simulink model "Comprobacion_Final"  (R2024a)
settings: Solver=ode45  StartTime=0.0  StopTime=10  MaxStep=0.001  RelTol=1e-3
(part 2 of 2)

== matlab function Comprobacion_Final/Cinematica ==
  data: x output; y output; Zin output; x input; dx input; ddx input; theta output; dlth output; ddlth2 output; phi output; dlph output; ddlph2 output; dT output; y input; dy input; ddy input; dz input; ddz input; Zin input; dZin input; ddZin input; ddT output; dpsi output; ddpsi output
function [x, y, Zin, theta, dlth, ddlth2, phi, dlph, ddlph2, dT, ddT, dpsi, ddpsi] = fcn(x, dx, ddx, y, dy, ddy, dz, ddz, Zin, dZin, ddZin)
%% Constantes
p = 79.375;
b = 50.8;
l2 = 93.196;
l1 = 44.45;

%% ============ Geometria de la plataforma (Ax,Ay,Zin -> Oi) ============
Ax = x;
Ay = y;
f1 = (-sin(Ax)*sin(Ay))/(cos(Ax)+cos(Ay));
Az = atan(f1);

alfa1 = deg2rad(0);
alfa2 = deg2rad(120);
alfa3 = deg2rad(240);

Oz = Zin;

R = [ cos(Ay)*cos(Az)                            -cos(Ay)*sin(Az)                          sin(Ay)
      cos(Ax)*sin(Az)+cos(Az)*sin(Ax)*sin(Ay)    cos(Ax)*cos(Az)-sin(Ax)*sin(Ay)*sin(Az)  -cos(Ay)*sin(Ax)
      sin(Ax)*sin(Az)-cos(Ax)*cos(Az)*sin(Ay)    cos(Az)*sin(Ax)+cos(Ax)*sin(Ay)*sin(Az)   cos(Ax)*cos(Ay)];

Rz1 = [cos(alfa1) -sin(alfa1) 0; sin(alfa1) cos(alfa1) 0; 0 0 1];
Rz2 = [cos(alfa2) -sin(alfa2) 0; sin(alfa2) cos(alfa2) 0; 0 0 1];
Rz3 = [cos(alfa3) -sin(alfa3) 0; sin(alfa3) cos(alfa3) 0; 0 0 1];

P = [p; 0; 0];
ux = R(1,1); uy = R(1,2); vy = R(2,2);
Ox = (p*(ux-vy))/2;
Oy = -uy*p;
T  = [Ox; Oy; Oz];
psi = [Ax;Ay;Az];

O1 = T + (R*Rz1*P);
O2 = T + (R*Rz2*P);
O3 = T + (R*Rz3*P);
%% derivadas de o
% Derivada temporal de R (verificada simbólicamente con sympy)
dAx=dx; dAy=dy; dAz=dz;
dpsi=[dAx;dAy;dAz];
ddAx=ddx; ddAy=ddy; ddAz=ddz;
ddpsi=[ddAx;ddAy;ddAz];

dR = [ -dAy*sin(Ay)*cos(Az) - dAz*sin(Az)*cos(Ay), dAy*sin(Ay)*sin(Az) - dAz*cos(Ay)*cos(Az), dAy*cos(Ay);
       -dAx*sin(Ax)*sin(Az) + dAx*sin(Ay)*cos(Ax)*cos(Az) + dAy*sin(Ax)*cos(Ay)*cos(Az) - dAz*sin(Ax)*sin(Ay)*sin(Az) + dAz*cos(Ax)*cos(Az),-dAx*sin(Ax)*cos(Az) - dAx*sin(Ay)*sin(Az)*cos(Ax) - dAy*sin(Ax)*sin(Az)*cos(Ay) - dAz*sin(Ax)*sin(Ay)*cos(Az) - dAz*sin(Az)*cos(Ax), -dAx*cos(Ax)*cos(Ay) + dAy*sin(Ax)*sin(Ay);
        dAx*sin(Ax)*sin(Ay)*cos(Az) + dAx*sin(Az)*cos(Ax) - dAy*cos(Ax)*cos(Ay)*cos(Az) + dAz*sin(Ax)*cos(Az) + dAz*sin(Ay)*sin(Az)*cos(Ax), -dAx*sin(Ax)*sin(Ay)*sin(Az) + dAx*cos(Ax)*cos(Az) + dAy*sin(Az)*cos(Ax)*cos(Ay) - dAz*sin(Ax)*sin(Az) + dAz*sin(Ay)*cos(Ax)*cos(Az), -dAx*sin(Ax)*cos(Ay) - dAy*sin(Ay)*cos(Ax) ];

% Derivada temporal de T = [Ox;Oy;Oz]
dux = dR(1,1);   
duy = dR(1,2);   
dvy = dR(2,2);   

dOx = (p*(dux - dvy))/2;
dOy = -duy*p;
dOz = dZin;         

dT = [dOx; dOy; dOz];

dO1 = dT + p*cos(alfa1)*dR(:,1) + p*sin(alfa1)*dR(:,2);
dO2 = dT + p*cos(alfa2)*dR(:,1) + p*sin(alfa2)*dR(:,2);
dO3 = dT + p*cos(alfa3)*dR(:,1) + p*sin(alfa3)*dR(:,2);
%segunda derivada
% Segundas derivadas de ux = R(1,1), uy = R(1,2), vy = R(2,2)
d2ux = 2*dAy*dAz*sin(Ay)*sin(Az) - (dAy^2*cos(Ay) + ddAy*sin(Ay))*cos(Az) - (dAz^2*cos(Az) + ddAz*sin(Az))*cos(Ay);
d2uy = 2*dAy*dAz*sin(Ay)*cos(Az) + (dAy^2*cos(Ay) + ddAy*sin(Ay))*sin(Az) + (dAz^2*sin(Az) - ddAz*cos(Az))*cos(Ay);
d2vy = dAx^2*sin(Ax)*sin(Ay)*sin(Az) - dAx^2*cos(Ax)*cos(Az)- 2*dAx*dAy*sin(Az)*cos(Ax)*cos(Ay)+ 2*dAx*dAz*sin(Ax)*sin(Az)- 2*dAx*dAz*sin(Ay)*cos(Ax)*cos(Az) + dAy^2*sin(Ax)*sin(Ay)*sin(Az)  - 2*dAy*dAz*sin(Ax)*cos(Ay)*cos(Az) + dAz^2*sin(Ax)*sin(Ay)*sin(Az) - dAz^2*cos(Ax)*cos(Az) - ddAx*sin(Ax)*cos(Az) - ddAx*sin(Ay)*sin(Az)*cos(Ax) - ddAy*sin(Ax)*sin(Az)*cos(Ay) - ddAz*sin(Ax)*sin(Ay)*cos(Az) - ddAz*sin(Az)*cos(Ax);
% Segunda derivada de T = [Ox;Oy;Oz]
ddOx = p*(d2ux - d2vy)/2;
ddOy = -d2uy*p;
ddOz = ddZin; 

ddT = [ddOx; ddOy; ddOz];

%% ============ Cinematica inversa de posicion por pierna ============
[th1, phi1] = solveLeg(O1, alfa1, b, l1, l2);
[th2, phi2] = solveLeg(O2, alfa2, b, l1, l2);
[th3, phi3] = solveLeg(O3, alfa3, b, l1, l2);

theta = [th1; th2; th3];
phi   = [phi1; phi2; phi3];

%% ============ Jacobiano de restriccion por pierna (lD, E) ============
lD1 = [-2*cos(alfa1)*(b+l1*cos(th1))+2*O1(1)   0   2*cos(alfa1)^2*(O1(3)+l1*sin(th1))];
E1  =  2*l1*cos(alfa1)*(cos(alfa1)*cos(th1)*O1(3) + (-b*cos(alfa1)+O1(1))*sin(th1));

lD2 = [-2*cos(alfa2)*(b+l1*cos(th2))+2*O2(1)   0   2*cos(alfa2)^2*(O2(3)+l1*sin(th2))];
E2  =  2*l1*cos(alfa2)*(cos(alfa2)*cos(th2)*O2(3) + (-b*cos(alfa2)+O2(1))*sin(th2));

lD3 = [-2*cos(alfa3)*(b+l1*cos(th3))+2*O3(1)   0   2*cos(alfa3)^2*(O3(3)+l1*sin(th3))];
E3  =  2*l1*cos(alfa3)*(cos(alfa3)*cos(th3)*O3(3) + (-b*cos(alfa3)+O3(1))*sin(th3));

Js = [lD1  0  0  0  0  0  0
       0   0  0 lD2 0  0  0
       0   0  0  0  0  0 lD3];

Jth = [E1  0  0
        0  E2 0
        0  0  E3];

dlX = [dZin; dx; dy];

%% ============ Jacobiano de orientacion pierna<-plataforma ============
Jto1 = [1 0 0                    0                                           (-p*sin(Ay)*cos(alfa1+Az))              (-p*cos(Ay)*sin(alfa1+Az))
        0 1 0 p*((cos(Ax)*sin(Ay)*cos(alfa1+Az))-sin(Ax)*sin(alfa1+Az))  (p*sin(Ax)*cos(Ay)*cos(alfa1+Az))  p*(cos(Ax)*cos(alfa1+Az)-(sin(Ax)*sin(Ay)*sin(alfa1+Az)))
        0 0 1 p*((sin(Ax)*sin(Ay)*cos(alfa1+Az))+cos(Ax)*sin(alfa1+Az)) (-p*cos(Ax)*cos(Ay)*cos(alfa1+Az))  p*(sin(Ax)*cos(alfa1+Az)+(cos(Ax)*sin(Ay)*sin(alfa1+Az)))];

Jto2 = [1 0 0                    0                                           (-p*sin(Ay)*cos(alfa2+Az))              (-p*cos(Ay)*sin(alfa2+Az))
        0 1 0 p*((cos(Ax)*sin(Ay)*cos(alfa2+Az))-sin(Ax)*sin(alfa2+Az))  (p*sin(Ax)*cos(Ay)*cos(alfa2+Az))  p*(cos(Ax)*cos(alfa2+Az)-(sin(Ax)*sin(Ay)*sin(alfa2+Az)))
        0 0 1 p*((sin(Ax)*sin(Ay)*cos(alfa2+Az))+cos(Ax)*sin(alfa2+Az)) (-p*cos(Ax)*cos(Ay)*cos(alfa2+Az))  p*(sin(Ax)*cos(alfa2+Az)+(cos(Ax)*sin(Ay)*sin(alfa2+Az)))];

Jto3 = [1 0 0                    0                                           (-p*sin(Ay)*cos(alfa3+Az))              (-p*cos(Ay)*sin(alfa3+Az))
        0 1 0 p*((cos(Ax)*sin(Ay)*cos(alfa3+Az))-sin(Ax)*sin(alfa3+Az))  (p*sin(Ax)*cos(Ay)*cos(alfa3+Az))  p*(cos(Ax)*cos(alfa3+Az)-(sin(Ax)*sin(Ay)*sin(alfa3+Az)))
        0 0 1 p*((sin(Ax)*sin(Ay)*cos(alfa3+Az))+cos(Ax)*sin(alfa3+Az)) (-p*cos(Ax)*cos(Ay)*cos(alfa3+Az))  p*(sin(Ax)*cos(alfa3+Az)+(cos(Ax)*sin(Ay)*sin(alfa3+Az)))];

Jts = [Jto1; Jto2; Jto3];

%% ============ Jacobiano de la tarea independiente ============
Jox = [0 -(p*cos(Ay)*sin(Ay)*(cos(Ax)+cos(Ay)*sin(Ax)*sin(Ay)))/(2*(1+cos(Ax)*cos(Ay))^2) ...
         -(p*cos(Ay)*sin(Ax)*(cos(Ax)+cos(Ay)+sin(Ax)*sin(Ay)))/(2*(1+cos(Ax)*cos(Ay))^2)];
Joy = [0 -(p*cos(Ay)*sin(Ay)*(cos(Ax)+cos(Ay)))/((1+cos(Ax)*cos(Ay))^2) ...
         -(p*sin(Ax)*(sin(Ax)^2*sin(Ay)^2-cos(Ay)^4-cos(Ax)^2*cos(Ay)^2-1/4*cos(Ax)*(5*cos(Ay)+3*cos(Ay)^3)))/((1+cos(Ax)*cos(Ay))^3)];
JAz = [0 -sin(Ay)/(1+cos(Ax)*cos(Ay))  -sin(Ax)/(1+cos(Ax)*cos(Ay))];
I3x3 = eye(3);

Jxit = [Jox; Joy; I3x3; JAz];
Jxith = (-inv(Jth))*Js*Jts*Jxit;

Dlth = Jxith*dlX;
dlth = [Dlth(1); Dlth(2); Dlth(3)];
dth1=Dlth(1); dth2=Dlth(2); dth3=Dlth(3);
%
JSph1 = [0 0 -1/l2*cos(phi1)];
Jth1ph1 = -l1*cos(th1)/l2*cos(phi1);
JSph2 = [0 0 -1/l2*cos(phi2)];
Jth2ph2 = -l1*cos(th2)/l2*cos(phi2);
JSph3 = [0 0 -1/l2*cos(phi3)];
Jth3ph3 = -l1*cos(th3)/l2*cos(phi3);

JSph = [JSph1 0 0   0   0 0   0
          0   0 0 JSph2 0 0   0
          0   0 0   0   0 0 JSph3];
Jthph = [Jth1ph1    0        0
            0    Jth2ph2     0
            0       0    Jth3ph3];

Jxis = Jts*Jxit;
Jxiph = (JSph*Jxis + Jthph*Jxith);

Dlph = Jxiph*dlX;
dlph = [Dlph(1); Dlph(2); Dlph(3)];
dphi1=Dlph(1); dphi2=Dlph(2); dphi3=Dlph(3);
%% ============ Segunda derivada ============
ddlX = [ddZin; ddx; ddy];

%Ddlth = dJxith*dlX + Jxith*ddlX;
%ddlth = [Ddlth(1); Ddlth(2); Ddlth(3)];

%Ddlph = dJxiph*dlX + Jxiph*ddlX;
%ddlph = [Ddlph(1); Ddlph(2); Ddlph(3)];
%% Segunda derivada time deriv
dJXTH=[(cos(alfa1)*(dO1(1)*l1 - dO1(1)*l1*cos(th1)^2 - O1(1)*dO1(3)*sin(th1) + O1(3)*dO1(1)*sin(th1) - O1(3)^2*dth1*cos(alfa1)*sin(th1) + O1(1)*O1(3)*dth1*cos(th1) - O1(3)*dth1*l1*cos(alfa1) + b*dO1(3)*cos(alfa1)*sin(th1) - O1(3)*b*dth1*cos(alfa1)*cos(th1) + dO1(3)*l1*cos(alfa1)*cos(th1)*sin(th1)))/(l1*(O1(1)*sin(th1) + O1(3)*cos(alfa1)*cos(th1) - b*cos(alfa1)*sin(th1))^2), dAx*((cos(Ay)*sin(Ax)*sin(Ay)*((p*cos(alfa1)*(cos(Az + alfa1)*sin(Ax) + sin(Az + alfa1)*cos(Ax)*sin(Ay))*(O1(3) + l1*sin(th1)))/(l1*(O1(1)*sin(th1) + O1(3)*cos(alfa1)*cos(th1) - b*cos(alfa1)*sin(th1))) + (p*sin(Az + alfa1)*cos(Ay)*(2*b*cos(alfa1) - 2*O1(1) + 2*l1*cos(alfa1)*cos(th1)))/(2*l1*cos(alfa1)*(O1(1)*sin(th1) + O1(3)*cos(alfa1)*cos(th1) - b*cos(alfa1)*sin(th1)))))/(cos(Ax)*cos(Ay) + 1)^2 + (p*cos(alfa1)*(sin(Az + alfa1)*sin(Ax) - cos(Az + alfa1)*cos(Ax)*sin(Ay))*(O1(3) + l1*sin(th1)))/(l1*(O1(1)*sin(th1) + O1(3)*cos(alfa1)*cos(th1) - b*cos(alfa1)*sin(th1))) + (p*sin(Ay)*cos(alfa1)*(cos(Az + alfa1)*cos(Ax) - sin(Az + alfa1)*sin(Ax)*sin(Ay))*(O1(3) + l1*sin(th1)))/(l1*(cos(Ax)*cos(Ay) + 1)*(O1(1)*sin(th1) + O1(3)*cos(alfa1)*cos(th1) - b*cos(alfa1)*sin(th1))) + (p*cos(Ay)*sin(Ay)*(sin(Ax) - cos(Ax)*cos(Ay)*sin(Ay))*(2*b*cos(alfa1) - 2*O1(1) + 2*l1*cos(alfa1)*cos(th1)))/(4*l1*cos(alfa1)*(cos(Ax)*cos(Ay) + 1)^2*(O1(1)*sin(th1) + O1(3)*cos(alfa1)*cos(th1) - b*cos(alfa1)*sin(th1))) - (p*cos(Ay)^2*sin(Ax)*sin(Ay)*(cos(Ax) + cos(Ay)*sin(Ax)*sin(Ay))*(2*b*cos(alfa1) - 2*O1(1) + 2*l1*cos(alfa1)*cos(th1)))/(2*l1*cos(alfa1)*(cos(Ax)*cos(Ay) + 1)^3*(O1(1)*sin(th1) + O1(3)*cos(alfa1)*cos(th1) - b*cos(alfa1)*sin(th1)))) - dAz*((sin(Ay)*((p*cos(alfa1)*(sin(Az + alfa1)*sin(Ax) - cos(Az + alfa1)*cos(Ax)*sin(Ay))*(O1(3) + l1*sin(th1)))/(l1*(O1(1)*sin(th1) + O1(3)*cos(alfa1)*cos(th1) - b*cos(alfa1)*sin(th1))) - (p*cos(Az + alfa1)*cos(Ay)*(2*b*cos(alfa1) - 2*O1(1) + 2*l1*cos(alfa1)*cos(th1)))/(2*l1*cos(alfa1)*(O1(1)*sin(th1) + O1(3)*cos(alfa1)*cos(th1) - b*cos(alfa1)*sin(th1)))))/(cos(Ax)*cos(Ay) + 1) + (p*cos(alfa1)*(cos(Az + alfa1)*cos(Ax) - sin(Az + alfa1)*sin(Ax)*sin(Ay))*(O1(3) + l1*sin(th1)))/(l1*(O1(1)*sin(th1) + O1(3)*cos(alfa1)*cos(th1) - b*cos(alfa1)*sin(th1)))) + dAy*((cos(Ay)*((p*cos(alfa1)*(cos(Az + alfa1)*sin(Ax) + sin(Az + alfa1)*cos(Ax)*sin(Ay))*(O1(3) + l1*sin(th1)))/(l1*(O1(1)*sin(th1) + O1(3)*cos(alfa1)*cos(th1) - b*cos(alfa1)*sin(th1))) + (p*sin(Az + alfa1)*cos(Ay)*(2*b*cos(alfa1) - 2*O1(1) + 2*l1*cos(alfa1)*cos(th1)))/(2*l1*cos(alfa1)*(O1(1)*sin(th1) + O1(3)*cos(alfa1)*cos(th1) - b*cos(alfa1)*sin(th1)))))/(cos(Ax)*cos(Ay) + 1) + (cos(Ax)*sin(Ay)^2*((p*cos(alfa1)*(cos(Az + alfa1)*sin(Ax) + sin(Az + alfa1)*cos(Ax)*sin(Ay))*(O1(3) + l1*sin(th1)))/(l1*(O1(1)*sin(th1) + O1(3)*cos(alfa1)*cos(th1) - b*cos(alfa1)*sin(th1))) + (p*sin(Az + alfa1)*cos(Ay)*(2*b*cos(alfa1) - 2*O1(1) + 2*l1*cos(alfa1)*cos(th1)))/(2*l1*cos(alfa1)*(O1(1)*sin(th1) + O1(3)*cos(alfa1)*cos(th1) - b*cos(alfa1)*sin(th1)))))/(cos(Ax)*cos(Ay) + 1)^2 - (p*cos(Az + alfa1)*cos(Ay)*sin(Ax)*cos(alfa1)*(O1(3) + l1*sin(th1)))/(l1*(O1(1)*sin(th1) + O1(3)*cos(alfa1)*cos(th1) - b*cos(alfa1)*sin(th1))) - (p*cos(Ay)^2*(cos(Ax) + cos(Ay)*sin(Ax)*sin(Ay))*(2*b*cos(alfa1) - 2*O1(1) + 2*l1*cos(alfa1)*cos(th1)))/(4*l1*cos(alfa1)*(cos(Ax)*cos(Ay) + 1)^2*(O1(1)*sin(th1) + O1(3)*cos(alfa1)*cos(th1) - b*cos(alfa1)*sin(th1))) + (p*sin(Ay)^2*(cos(Ax) + cos(Ay)*sin(Ax)*sin(Ay))*(2*b*cos(alfa1) - 2*O1(1) + 2*l1*cos(alfa1)*cos(th1)))/(4*l1*cos(alfa1)*(cos(Ax)*cos(Ay) + 1)^2*(O1(1)*sin(th1) + O1(3)*cos(alfa1)*cos(th1) - b*cos(alfa1)*sin(th1))) + (p*sin(Az + alfa1)*sin(Ay)*(O1(1)*sin(Ay) - b*sin(Ay)*cos(alfa1) + O1(3)*cos(Ax)*cos(Ay)*cos(alfa1)^2 - l1*sin(Ay)*cos(alfa1)*cos(th1) + l1*cos(Ax)*cos(Ay)*cos(alfa1)^2*sin(th1)))/(l1*cos(alfa1)*(cos(Ax)*cos(Ay) + 1)*(O1(1)*sin(th1) + O1(3)*cos(alfa1)*cos(th1) - b*cos(alfa1)*sin(th1))) - (p*cos(Ax)*cos(Ay)*sin(Ay)^2*(cos(Ax) + cos(Ay)*sin(Ax)*sin(Ay))*(2*b*cos(alfa1) - 2*O1(1) + 2*l1*cos(alfa1)*cos(th1)))/(2*l1*cos(alfa1)*(cos(Ax)*cos(Ay) + 1)^3*(O1(1)*sin(th1) + O1(3)*cos(alfa1)*cos(th1) - b*cos(alfa1)*sin(th1))) - (p*cos(Ay)*sin(Ax)*sin(Ay)*(2*cos(Ay)^2 - 1)*(2*b*cos(alfa1) - 2*O1(1) + 2*l1*cos(alfa1)*cos(th1)))/(4*l1*cos(alfa1)*(cos(Ax)*cos(Ay) + 1)^2*(O1(1)*sin(th1) + O1(3)*cos(alfa1)*cos(th1) - b*cos(alfa1)*sin(th1)))) + (dO1(3)*p*(b*cos(alfa1) - O1(1) + l1*cos(alfa1)*cos(th1))*(cos(Ay)^2*sin(Ax)*sin(Ay)^2*cos(th1) - 2*sin(Az + alfa1)*cos(Ay)*sin(Ay)*cos(th1) + 2*sin(Az + alfa1)*cos(Ax)*cos(alfa1)*sin(th1) + cos(Ax)*cos(Ay)*sin(Ay)*cos(th1) - 2*sin(Az + alfa1)*cos(Ax)*cos(Ay)^2*sin(Ay)*cos(th1) + 4*sin(Az + alfa1)*cos(Ax)^2*cos(Ay)*cos(alfa1)*sin(th1) - 2*sin(Az + alfa1)*cos(Ax)*sin(Ay)^2*cos(alfa1)*sin(th1) + 2*sin(Az + alfa1)*cos(Ax)^3*cos(Ay)^2*cos(alfa1)*sin(th1) - 2*sin(Az + alfa1)*cos(Ax)^2*cos(Ay)*sin(Ay)^2*cos(alfa1)*sin(th1) + 2*cos(Az + alfa1)*cos(Ax)*cos(Ay)*sin(Ax)*sin(Ay)*cos(alfa1)*sin(th1) + 2*cos(Az + alfa1)*cos(Ax)^2*cos(Ay)^2*sin(Ax)*sin(Ay)*cos(alfa1)*sin(th1)))/(2*l1*(cos(Ax)*cos(Ay) + 1)^2*(O1(1)*sin(th1) + O1(3)*cos(alfa1)*cos(th1) - b*cos(alfa1)*sin(th1))^2) + (dO1(1)*p*(O1(3) + l1*sin(th1))*(cos(Ay)^2*sin(Ax)*sin(Ay)^2*cos(th1) - 2*sin(Az + alfa1)*cos(Ay)*sin(Ay)*cos(th1) + 2*sin(Az + alfa1)*cos(Ax)*cos(alfa1)*sin(th1) + cos(Ax)*cos(Ay)*sin(Ay)*cos(th1) - 2*sin(Az + alfa1)*cos(Ax)*cos(Ay)^2*sin(Ay)*cos(th1) + 4*sin(Az + alfa1)*cos(Ax)^2*cos(Ay)*cos(alfa1)*sin(th1) - 2*sin(Az + alfa1)*cos(Ax)*sin(Ay)^2*cos(alfa1)*sin(th1) + 2*sin(Az + alfa1)*cos(Ax)^3*cos(Ay)^2*cos(alfa1)*sin(th1) - 2*sin(Az + alfa1)*cos(Ax)^2*cos(Ay)*sin(Ay)^2*cos(alfa1)*sin(th1) + 2*cos(Az + alfa1)*cos(Ax)*cos(Ay)*sin(Ax)*sin(Ay)*cos(alfa1)*sin(th1) + 2*cos(Az + alfa1)*cos(Ax)^2*cos(Ay)^2*sin(Ax)*sin(Ay)*cos(alfa1)*sin(th1)))/(2*l1*(cos(Ax)*cos(Ay) + 1)^2*(O1(1)*sin(th1) + O1(3)*cos(alfa1)*cos(th1) - b*cos(alfa1)*sin(th1))^2) - (dth1*p*(l1*cos(alfa1) - O1(1)*cos(th1) + O1(3)*cos(alfa1)*sin(th1) + b*cos(alfa1)*cos(th1))*(2*O1(1)*sin(Az + alfa1)*cos(Ay)*sin(Ay) - O1(1)*cos(Ax)*cos(Ay)*sin(Ay) + O1(1)*sin(Ax)*sin(Ay)^2*(sin(Ay)^2 - 1) + 2*O1(3)*sin(Az + alfa1)*cos(Ax)*cos(alfa1)^2 - 2*O1(3)*sin(Az + alfa1)*cos(Ax)*sin(Ay)^2*cos(alfa1)^2 + 2*O1(3)*sin(Az + alfa1)*cos(Ax)^3*cos(Ay)^2*cos(alfa1)^2 + b*cos(Ay)^2*sin(Ax)*sin(Ay)^2*cos(alfa1) - 2*b*sin(Az + alfa1)*cos(Ay)*sin(Ay)*cos(alfa1) + 2*O1(1)*sin(Az + alfa1)*cos(Ax)*cos(Ay)^2*sin(Ay) + b*cos(Ax)*cos(Ay)*sin(Ay)*cos(alfa1) + 4*O1(3)*sin(Az + alfa1)*cos(Ax)^2*cos(Ay)*cos(alfa1)^2 - 2*O1(3)*sin(Az + alfa1)*cos(Ax)^2*cos(Ay)*sin(Ay)^2*cos(alfa1)^2 - 2*b*sin(Az + alfa1)*cos(Ax)*cos(Ay)^2*sin(Ay)*cos(alfa1) + 2*O1(3)*cos(Az + alfa1)*cos(Ax)^2*cos(Ay)^2*sin(Ax)*sin(Ay)*cos(alfa1)^2 + 2*O1(3)*cos(Az + alfa1)*cos(Ax)*cos(Ay)*sin(Ax)*sin(Ay)*cos(alfa1)^2))/(2*l1*cos(alfa1)*(cos(Ax)*cos(Ay) + 1)^2*(O1(1)*sin(th1) + O1(3)*cos(alfa1)*cos(th1) - b*cos(alfa1)*sin(th1))^2), dAx*((cos(Ax)*((p*cos(alfa1)*(cos(Az + alfa1)*sin(Ax) + sin(Az + alfa1)*cos(Ax)*sin(Ay))*(O1(3) + l1*sin(th1)))/(l1*(O1(1)*sin(th1) + O1(3)*cos(alfa1)*cos(th1) - b*cos(alfa1)*sin(th1))) + (p*sin(Az + alfa1)*cos(Ay)*(2*b*cos(alfa1) - 2*O1(1) + 2*l1*cos(alfa1)*cos(th1)))/(2*l1*cos(alfa1)*(O1(1)*sin(th1) + O1(3)*cos(alfa1)*cos(th1) - b*cos(alfa1)*sin(th1)))))/(cos(Ax)*cos(Ay) + 1) + (cos(Ay)*sin(Ax)^2*((p*cos(alfa1)*(cos(Az + alfa1)*sin(Ax) + sin(Az + alfa1)*cos(Ax)*sin(Ay))*(O1(3) + l1*sin(th1)))/(l1*(O1(1)*sin(th1) + O1(3)*cos(alfa1)*cos(th1) - b*cos(alfa1)*sin(th1))) + (p*sin(Az + alfa1)*cos(Ay)*(2*b*cos(alfa1) - 2*O1(1) + 2*l1*cos(alfa1)*cos(th1)))/(2*l1*cos(alfa1)*(O1(1)*sin(th1) + O1(3)*cos(alfa1)*cos(th1) - b*cos(alfa1)*sin(th1)))))/(cos(Ax)*cos(Ay) + 1)^2 - (p*cos(Az + alfa1)*cos(Ay)*sin(Ax)*cos(alfa1)*(O1(3) + l1*sin(th1)))/(l1*(O1(1)*sin(th1) + O1(3)*cos(alfa1)*cos(th1) - b*cos(alfa1)*sin(th1))) + (p*sin(Ax)*cos(alfa1)*(cos(Az + alfa1)*cos(Ax) - sin(Az + alfa1)*sin(Ax)*sin(Ay))*(O1(3) + l1*sin(th1)))/(l1*(cos(Ax)*cos(Ay) + 1)*(O1(1)*sin(th1) + O1(3)*cos(alfa1)*cos(th1) - b*cos(alfa1)*sin(th1))) + (p*cos(Ay)*sin(Ax)*(sin(Ax) - cos(Ax)*sin(Ay))*(2*b*cos(alfa1) - 2*O1(1) + 2*l1*cos(alfa1)*cos(th1)))/(4*l1*cos(alfa1)*(cos(Ax)*cos(Ay) + 1)^2*(O1(1)*sin(th1) + O1(3)*cos(alfa1)*cos(th1) - b*cos(alfa1)*sin(th1))) - (p*cos(Ay)^2*sin(Ax)^2*(cos(Ax) + cos(Ay) + sin(Ax)*sin(Ay))*(2*b*cos(alfa1) - 2*O1(1) + 2*l1*cos(alfa1)*cos(th1)))/(2*l1*cos(alfa1)*(cos(Ax)*cos(Ay) + 1)^3*(O1(1)*sin(th1) + O1(3)*cos(alfa1)*cos(th1) - b*cos(alfa1)*sin(th1))) - (p*cos(Ax)*cos(Ay)*(cos(Ax) + cos(Ay) + sin(Ax)*sin(Ay))*(2*b*cos(alfa1) - 2*O1(1) + 2*l1*cos(alfa1)*cos(th1)))/(4*l1*cos(alfa1)*(cos(Ax)*cos(Ay) + 1)^2*(O1(1)*sin(th1) + O1(3)*cos(alfa1)*cos(th1) - b*cos(alfa1)*sin(th1)))) - dAz*((sin(Ax)*((p*cos(alfa1)*(sin(Az + alfa1)*sin(Ax) - cos(Az + alfa1)*cos(Ax)*sin(Ay))*(O1(3) + l1*sin(th1)))/(l1*(O1(1)*sin(th1) + O1(3)*cos(alfa1)*cos(th1) - b*cos(alfa1)*sin(th1))) - (p*cos(Az + alfa1)*cos(Ay)*(2*b*cos(alfa1) - 2*O1(1) + 2*l1*cos(alfa1)*cos(th1)))/(2*l1*cos(alfa1)*(O1(1)*sin(th1) + O1(3)*cos(alfa1)*cos(th1) - b*cos(alfa1)*sin(th1)))))/(cos(Ax)*cos(Ay) + 1) - (p*sin(Az + alfa1)*sin(Ay)*(2*b*cos(alfa1) - 2*O1(1) + 2*l1*cos(alfa1)*cos(th1)))/(2*l1*cos(alfa1)*(O1(1)*sin(th1) + O1(3)*cos(alfa1)*cos(th1) - b*cos(alfa1)*sin(th1))) + (p*sin(Az + alfa1)*cos(Ax)*cos(Ay)*cos(alfa1)*(O1(3) + l1*sin(th1)))/(l1*(O1(1)*sin(th1) + O1(3)*cos(alfa1)*cos(th1) - b*cos(alfa1)*sin(th1)))) + dAy*((cos(Ax)*sin(Ax)*sin(Ay)*((p*cos(alfa1)*(cos(Az + alfa1)*sin(Ax) + sin(Az + alfa1)*cos(Ax)*sin(Ay))*(O1(3) + l1*sin(th1)))/(l1*(O1(1)*sin(th1) + O1(3)*cos(alfa1)*cos(th1) - b*cos(alfa1)*sin(th1))) + (p*sin(Az + alfa1)*cos(Ay)*(2*b*cos(alfa1) - 2*O1(1) + 2*l1*cos(alfa1)*cos(th1)))/(2*l1*cos(alfa1)*(O1(1)*sin(th1) + O1(3)*cos(alfa1)*cos(th1) - b*cos(alfa1)*sin(th1)))))/(cos(Ax)*cos(Ay) + 1)^2 - (p*cos(Az + alfa1)*cos(Ay)*(2*b*cos(alfa1) - 2*O1(1) + 2*l1*cos(alfa1)*cos(th1)))/(2*l1*cos(alfa1)*(O1(1)*sin(th1) + O1(3)*cos(alfa1)*cos(th1) - b*cos(alfa1)*sin(th1))) - (p*cos(Az + alfa1)*cos(Ax)*sin(Ay)*cos(alfa1)*(O1(3) + l1*sin(th1)))/(l1*(O1(1)*sin(th1) + O1(3)*cos(alfa1)*cos(th1) - b*cos(alfa1)*sin(th1))) + (p*sin(Az + alfa1)*sin(Ax)*(O1(1)*sin(Ay) - b*sin(Ay)*cos(alfa1) + O1(3)*cos(Ax)*cos(Ay)*cos(alfa1)^2 - l1*sin(Ay)*cos(alfa1)*cos(th1) + l1*cos(Ax)*cos(Ay)*cos(alfa1)^2*sin(th1)))/(l1*cos(alfa1)*(cos(Ax)*cos(Ay) + 1)*(O1(1)*sin(th1) + O1(3)*cos(alfa1)*cos(th1) - b*cos(alfa1)*sin(th1))) + (p*sin(Ax)*sin(Ay)*(cos(Ax) + cos(Ay) + sin(Ax)*sin(Ay))*(2*b*cos(alfa1) - 2*O1(1) + 2*l1*cos(alfa1)*cos(th1)))/(4*l1*cos(alfa1)*(cos(Ax)*cos(Ay) + 1)^2*(O1(1)*sin(th1) + O1(3)*cos(alfa1)*cos(th1) - b*cos(alfa1)*sin(th1))) + (p*cos(Ay)*sin(Ax)*(sin(Ay) - cos(Ay)*sin(Ax))*(2*b*cos(alfa1) - 2*O1(1) + 2*l1*cos(alfa1)*cos(th1)))/(4*l1*cos(alfa1)*(cos(Ax)*cos(Ay) + 1)^2*(O1(1)*sin(th1) + O1(3)*cos(alfa1)*cos(th1) - b*cos(alfa1)*sin(th1))) - (p*cos(Ax)*cos(Ay)*sin(Ax)*sin(Ay)*(cos(Ax) + cos(Ay) + sin(Ax)*sin(Ay))*(2*b*cos(alfa1) - 2*O1(1) + 2*l1*cos(alfa1)*cos(th1)))/(2*l1*cos(alfa1)*(cos(Ax)*cos(Ay) + 1)^3*(O1(1)*sin(th1) + O1(3)*cos(alfa1)*cos(th1) - b*cos(alfa1)*sin(th1)))) - (dO1(3)*p*(b*cos(alfa1) - O1(1) + l1*cos(alfa1)*cos(th1))*(2*sin(Az + alfa1)*cos(Ay)*sin(Ax)*cos(th1) - cos(Ay)^2*sin(Ax)*cos(th1) - 2*cos(Az + alfa1)*sin(Ay)*cos(th1) - cos(Ax)*cos(Ay)*sin(Ax)*cos(th1) + 2*cos(Az + alfa1)*sin(Ax)^2*cos(alfa1)*sin(th1) - cos(Ay)*sin(Ax)^2*sin(Ay)*cos(th1) + 2*sin(Az + alfa1)*cos(Ax)*cos(Ay)^2*sin(Ax)*cos(th1) - 2*cos(Az + alfa1)*cos(Ax)^2*cos(Ay)^2*sin(Ay)*cos(th1) + 4*cos(Az + alfa1)*cos(Ax)^2*cos(Ay)^2*cos(alfa1)*sin(th1) + 2*cos(Az + alfa1)*cos(Ax)^3*cos(Ay)^3*cos(alfa1)*sin(th1) - 4*cos(Az + alfa1)*cos(Ax)*cos(Ay)*sin(Ay)*cos(th1) + 2*cos(Az + alfa1)*cos(Ax)*cos(Ay)*cos(alfa1)*sin(th1) + 2*sin(Az + alfa1)*cos(Ax)*sin(Ax)*sin(Ay)*cos(alfa1)*sin(th1) + 2*cos(Az + alfa1)*cos(Ax)*cos(Ay)*sin(Ax)^2*cos(alfa1)*sin(th1) + 2*sin(Az + alfa1)*cos(Ax)^2*cos(Ay)*sin(Ax)*sin(Ay)*cos(alfa1)*sin(th1)))/(2*l1*(cos(Ax)*cos(Ay) + 1)^2*(O1(1)*sin(th1) + O1(3)*cos(alfa1)*cos(th1) - b*cos(alfa1)*sin(th1))^2) - (dO1(1)*p*(O1(3) + l1*sin(th1))*(2*sin(Az + alfa1)*cos(Ay)*sin(Ax)*cos(th1) - cos(Ay)^2*sin(Ax)*cos(th1) - 2*cos(Az + alfa1)*sin(Ay)*cos(th1) - cos(Ax)*cos(Ay)*sin(Ax)*cos(th1) + 2*cos(Az + alfa1)*sin(Ax)^2*cos(alfa1)*sin(th1) - cos(Ay)*sin(Ax)^2*sin(Ay)*cos(th1) + 2*sin(Az + alfa1)*cos(Ax)*cos(Ay)^2*sin(Ax)*cos(th1) - 2*cos(Az + alfa1)*cos(Ax)^2*cos(Ay)^2*sin(Ay)*cos(th1) + 4*cos(Az + alfa1)*cos(Ax)^2*cos(Ay)^2*cos(alfa1)*sin(th1) + 2*cos(Az + alfa1)*cos(Ax)^3*cos(Ay)^3*cos(alfa1)*sin(th1) - 4*cos(Az + alfa1)*cos(Ax)*cos(Ay)*sin(Ay)*cos(th1) + 2*cos(Az + alfa1)*cos(Ax)*cos(Ay)*cos(alfa1)*sin(th1) + 2*sin(Az + alfa1)*cos(Ax)*sin(Ax)*sin(Ay)*cos(alfa1)*sin(th1) + 2*cos(Az + alfa1)*cos(Ax)*cos(Ay)*sin(Ax)^2*cos(alfa1)*sin(th1) + 2*sin(Az + alfa1)*cos(Ax)^2*cos(Ay)*sin(Ax)*sin(Ay)*cos(alfa1)*sin(th1)))/(2*l1*(cos(Ax)*cos(Ay) + 1)^2*(O1(1)*sin(th1) + O1(3)*cos(alfa1)*cos(th1) - b*cos(alfa1)*sin(th1))^2) + (dth1*p*(l1*cos(alfa1) - O1(1)*cos(th1) + O1(3)*cos(alfa1)*sin(th1) + b*cos(alfa1)*cos(th1))*(O1(1)*cos(Ay)^2*sin(Ax) + 2*O1(1)*cos(Az + alfa1)*sin(Ay) + O1(1)*cos(Ay)*sin(Ax)^2*sin(Ay) - b*cos(Ay)^2*sin(Ax)*cos(alfa1) + 2*O1(3)*cos(Az + alfa1)*sin(Ax)^2*cos(alfa1)^2 - 2*O1(1)*sin(Az + alfa1)*cos(Ay)*sin(Ax) - 2*b*cos(Az + alfa1)*sin(Ay)*cos(alfa1) + O1(1)*cos(Ax)*cos(Ay)*sin(Ax) + 4*O1(1)*cos(Az + alfa1)*cos(Ax)*cos(Ay)*sin(Ay) + 4*O1(3)*cos(Az + alfa1)*cos(Ax)^2*cos(Ay)^2*cos(alfa1)^2 + 2*O1(3)*cos(Az + alfa1)*cos(Ax)^3*cos(Ay)^3*cos(alfa1)^2 + 2*b*sin(Az + alfa1)*cos(Ay)*sin(Ax)*cos(alfa1) - 2*O1(1)*sin(Az + alfa1)*cos(Ax)*cos(Ay)^2*sin(Ax) + 2*O1(3)*cos(Az + alfa1)*cos(Ax)*cos(Ay)*cos(alfa1)^2 - b*cos(Ax)*cos(Ay)*sin(Ax)*cos(alfa1) + 2*O1(1)*cos(Az + alfa1)*cos(Ax)^2*cos(Ay)^2*sin(Ay) - b*cos(Ay)*sin(Ax)^2*sin(Ay)*cos(alfa1) + 2*O1(3)*sin(Az + alfa1)*cos(Ax)*sin(Ax)*sin(Ay)*cos(alfa1)^2 + 2*b*sin(Az + alfa1)*cos(Ax)*cos(Ay)^2*sin(Ax)*cos(alfa1) + 2*O1(3)*cos(Az + alfa1)*cos(Ax)*cos(Ay)*sin(Ax)^2*cos(alfa1)^2 - 2*b*cos(Az + alfa1)*cos(Ax)^2*cos(Ay)^2*sin(Ay)*cos(alfa1) - 4*b*cos(Az + alfa1)*cos(Ax)*cos(Ay)*sin(Ay)*cos(alfa1) + 2*O1(3)*sin(Az + alfa1)*cos(Ax)^2*cos(Ay)*sin(Ax)*sin(Ay)*cos(alfa1)^2))/(2*l1*cos(alfa1)*(cos(Ax)*cos(Ay) + 1)^2*(O1(1)*sin(th1) + O1(3)*cos(alfa1)*cos(th1) - b*cos(alfa1)*sin(th1))^2)
       (cos(alfa2)*(dO2(1)*l1 - dO2(1)*l1*cos(th2)^2 - O2(1)*dO2(3)*sin(th2) + O2(3)*dO2(1)*sin(th2) - O2(3)^2*dth2*cos(alfa2)*sin(th2) + O2(1)*O2(3)*dth2*cos(th2) - O2(3)*dth2*l1*cos(alfa2) + b*dO2(3)*cos(alfa2)*sin(th2) - O2(3)*b*dth2*cos(alfa2)*cos(th2) + dO2(3)*l1*cos(alfa2)*cos(th2)*sin(th2)))/(l1*(O2(1)*sin(th2) + O2(3)*cos(alfa2)*cos(th2) - b*cos(alfa2)*sin(th2))^2), dAx*((cos(Ay)*sin(Ax)*sin(Ay)*((p*cos(alfa2)*(cos(Az + alfa2)*sin(Ax) + sin(Az + alfa2)*cos(Ax)*sin(Ay))*(O2(3) + l1*sin(th2)))/(l1*(O2(1)*sin(th2) + O2(3)*cos(alfa2)*cos(th2) - b*cos(alfa2)*sin(th2))) + (p*sin(Az + alfa2)*cos(Ay)*(2*b*cos(alfa2) - 2*O2(1) + 2*l1*cos(alfa2)*cos(th2)))/(2*l1*cos(alfa2)*(O2(1)*sin(th2) + O2(3)*cos(alfa2)*cos(th2) - b*cos(alfa2)*sin(th2)))))/(cos(Ax)*cos(Ay) + 1)^2 + (p*cos(alfa2)*(sin(Az + alfa2)*sin(Ax) - cos(Az + alfa2)*cos(Ax)*sin(Ay))*(O2(3) + l1*sin(th2)))/(l1*(O2(1)*sin(th2) + O2(3)*cos(alfa2)*cos(th2) - b*cos(alfa2)*sin(th2))) + (p*sin(Ay)*cos(alfa2)*(cos(Az + alfa2)*cos(Ax) - sin(Az + alfa2)*sin(Ax)*sin(Ay))*(O2(3) + l1*sin(th2)))/(l1*(cos(Ax)*cos(Ay) + 1)*(O2(1)*sin(th2) + O2(3)*cos(alfa2)*cos(th2) - b*cos(alfa2)*sin(th2))) + (p*cos(Ay)*sin(Ay)*(sin(Ax) - cos(Ax)*cos(Ay)*sin(Ay))*(2*b*cos(alfa2) - 2*O2(1) + 2*l1*cos(alfa2)*cos(th2)))/(4*l1*cos(alfa2)*(cos(Ax)*cos(Ay) + 1)^2*(O2(1)*sin(th2) + O2(3)*cos(alfa2)*cos(th2) - b*cos(alfa2)*sin(th2))) - (p*cos(Ay)^2*sin(Ax)*sin(Ay)*(cos(Ax) + cos(Ay)*sin(Ax)*sin(Ay))*(2*b*cos(alfa2) - 2*O2(1) + 2*l1*cos(alfa2)*cos(th2)))/(2*l1*cos(alfa2)*(cos(Ax)*cos(Ay) + 1)^3*(O2(1)*sin(th2) + O2(3)*cos(alfa2)*cos(th2) - b*cos(alfa2)*sin(th2)))) - dAz*((sin(Ay)*((p*cos(alfa2)*(sin(Az + alfa2)*sin(Ax) - cos(Az + alfa2)*cos(Ax)*sin(Ay))*(O2(3) + l1*sin(th2)))/(l1*(O2(1)*sin(th2) + O2(3)*cos(alfa2)*cos(th2) - b*cos(alfa2)*sin(th2))) - (p*cos(Az + alfa2)*cos(Ay)*(2*b*cos(alfa2) - 2*O2(1) + 2*l1*cos(alfa2)*cos(th2)))/(2*l1*cos(alfa2)*(O2(1)*sin(th2) + O2(3)*cos(alfa2)*cos(th2) - b*cos(alfa2)*sin(th2)))))/(cos(Ax)*cos(Ay) + 1) + (p*cos(alfa2)*(cos(Az + alfa2)*cos(Ax) - sin(Az + alfa2)*sin(Ax)*sin(Ay))*(O2(3) + l1*sin(th2)))/(l1*(O2(1)*sin(th2) + O2(3)*cos(alfa2)*cos(th2) - b*cos(alfa2)*sin(th2)))) + dAy*((cos(Ay)*((p*cos(alfa2)*(cos(Az + alfa2)*sin(Ax) + sin(Az + alfa2)*cos(Ax)*sin(Ay))*(O2(3) + l1*sin(th2)))/(l1*(O2(1)*sin(th2) + O2(3)*cos(alfa2)*cos(th2) - b*cos(alfa2)*sin(th2))) + (p*sin(Az + alfa2)*cos(Ay)*(2*b*cos(alfa2) - 2*O2(1) + 2*l1*cos(alfa2)*cos(th2)))/(2*l1*cos(alfa2)*(O2(1)*sin(th2) + O2(3)*cos(alfa2)*cos(th2) - b*cos(alfa2)*sin(th2)))))/(cos(Ax)*cos(Ay) + 1) + (cos(Ax)*sin(Ay)^2*((p*cos(alfa2)*(cos(Az + alfa2)*sin(Ax) + sin(Az + alfa2)*cos(Ax)*sin(Ay))*(O2(3) + l1*sin(th2)))/(l1*(O2(1)*sin(th2) + O2(3)*cos(alfa2)*cos(th2) - b*cos(alfa2)*sin(th2))) + (p*sin(Az + alfa2)*cos(Ay)*(2*b*cos(alfa2) - 2*O2(1) + 2*l1*cos(alfa2)*cos(th2)))/(2*l1*cos(alfa2)*(O2(1)*sin(th2) + O2(3)*cos(alfa2)*cos(th2) - b*cos(alfa2)*sin(th2)))))/(cos(Ax)*cos(Ay) + 1)^2 - (p*cos(Az + alfa2)*cos(Ay)*sin(Ax)*cos(alfa2)*(O2(3) + l1*sin(th2)))/(l1*(O2(1)*sin(th2) + O2(3)*cos(alfa2)*cos(th2) - b*cos(alfa2)*sin(th2))) - (p*cos(Ay)^2*(cos(Ax) + cos(Ay)*sin(Ax)*sin(Ay))*(2*b*cos(alfa2) - 2*O2(1) + 2*l1*cos(alfa2)*cos(th2)))/(4*l1*cos(alfa2)*(cos(Ax)*cos(Ay) + 1)^2*(O2(1)*sin(th2) + O2(3)*cos(alfa2)*cos(th2) - b*cos(alfa2)*sin(th2))) + (p*sin(Ay)^2*(cos(Ax) + cos(Ay)*sin(Ax)*sin(Ay))*(2*b*cos(alfa2) - 2*O2(1) + 2*l1*cos(alfa2)*cos(th2)))/(4*l1*cos(alfa2)*(cos(Ax)*cos(Ay) + 1)^2*(O2(1)*sin(th2) + O2(3)*cos(alfa2)*cos(th2) - b*cos(alfa2)*sin(th2))) + (p*sin(Az + alfa2)*sin(Ay)*(O2(1)*sin(Ay) - b*sin(Ay)*cos(alfa2) + O2(3)*cos(Ax)*cos(Ay)*cos(alfa2)^2 - l1*sin(Ay)*cos(alfa2)*cos(th2) + l1*cos(Ax)*cos(Ay)*cos(alfa2)^2*sin(th2)))/(l1*cos(alfa2)*(cos(Ax)*cos(Ay) + 1)*(O2(1)*sin(th2) + O2(3)*cos(alfa2)*cos(th2) - b*cos(alfa2)*sin(th2))) - (p*cos(Ax)*cos(Ay)*sin(Ay)^2*(cos(Ax) + cos(Ay)*sin(Ax)*sin(Ay))*(2*b*cos(alfa2) - 2*O2(1) + 2*l1*cos(alfa2)*cos(th2)))/(2*l1*cos(alfa2)*(cos(Ax)*cos(Ay) + 1)^3*(O2(1)*sin(th2) + O2(3)*cos(alfa2)*cos(th2) - b*cos(alfa2)*sin(th2))) - (p*cos(Ay)*sin(Ax)*sin(Ay)*(2*cos(Ay)^2 - 1)*(2*b*cos(alfa2) - 2*O2(1) + 2*l1*cos(alfa2)*cos(th2)))/(4*l1*cos(alfa2)*(cos(Ax)*cos(Ay) + 1)^2*(O2(1)*sin(th2) + O2(3)*cos(alfa2)*cos(th2) - b*cos(alfa2)*sin(th2)))) + (dO2(3)*p*(b*cos(alfa2) - O2(1) + l1*cos(alfa2)*cos(th2))*(cos(Ay)^2*sin(Ax)*sin(Ay)^2*cos(th2) - 2*sin(Az + alfa2)*cos(Ay)*sin(Ay)*cos(th2) + 2*sin(Az + alfa2)*cos(Ax)*cos(alfa2)*sin(th2) + cos(Ax)*cos(Ay)*sin(Ay)*cos(th2) - 2*sin(Az + alfa2)*cos(Ax)*cos(Ay)^2*sin(Ay)*cos(th2) + 4*sin(Az + alfa2)*cos(Ax)^2*cos(Ay)*cos(alfa2)*sin(th2) - 2*sin(Az + alfa2)*cos(Ax)*sin(Ay)^2*cos(alfa2)*sin(th2) + 2*sin(Az + alfa2)*cos(Ax)^3*cos(Ay)^2*cos(alfa2)*sin(th2) - 2*sin(Az + alfa2)*cos(Ax)^2*cos(Ay)*sin(Ay)^2*cos(alfa2)*sin(th2) + 2*cos(Az + alfa2)*cos(Ax)*cos(Ay)*sin(Ax)*sin(Ay)*cos(alfa2)*sin(th2) + 2*cos(Az + alfa2)*cos(Ax)^2*cos(Ay)^2*sin(Ax)*sin(Ay)*cos(alfa2)*sin(th2)))/(2*l1*(cos(Ax)*cos(Ay) + 1)^2*(O2(1)*sin(th2) + O2(3)*cos(alfa2)*cos(th2) - b*cos(alfa2)*sin(th2))^2) + (dO2(1)*p*(O2(3) + l1*sin(th2))*(cos(Ay)^2*sin(Ax)*sin(Ay)^2*cos(th2) - 2*sin(Az + alfa2)*cos(Ay)*sin(Ay)*cos(th2) + 2*sin(Az + alfa2)*cos(Ax)*cos(alfa2)*sin(th2) + cos(Ax)*cos(Ay)*sin(Ay)*cos(th2) - 2*sin(Az + alfa2)*cos(Ax)*cos(Ay)^2*sin(Ay)*cos(th2) + 4*sin(Az + alfa2)*cos(Ax)^2*cos(Ay)*cos(alfa2)*sin(th2) - 2*sin(Az + alfa2)*cos(Ax)*sin(Ay)^2*cos(alfa2)*sin(th2) + 2*sin(Az + alfa2)*cos(Ax)^3*cos(Ay)^2*cos(alfa2)*sin(th2) - 2*sin(Az + alfa2)*cos(Ax)^2*cos(Ay)*sin(Ay)^2*cos(alfa2)*sin(th2) + 2*cos(Az + alfa2)*cos(Ax)*cos(Ay)*sin(Ax)*sin(Ay)*cos(alfa2)*sin(th2) + 2*cos(Az + alfa2)*cos(Ax)^2*cos(Ay)^2*sin(Ax)*sin(Ay)*cos(alfa2)*sin(th2)))/(2*l1*(cos(Ax)*cos(Ay) + 1)^2*(O2(1)*sin(th2) + O2(3)*cos(alfa2)*cos(th2) - b*cos(alfa2)*sin(th2))^2) - (dth2*p*(l1*cos(alfa2) - O2(1)*cos(th2) + O2(3)*cos(alfa2)*sin(th2) + b*cos(alfa2)*cos(th2))*(2*O2(1)*sin(Az + alfa2)*cos(Ay)*sin(Ay) - O2(1)*cos(Ax)*cos(Ay)*sin(Ay) + O2(1)*sin(Ax)*sin(Ay)^2*(sin(Ay)^2 - 1) + 2*O2(3)*sin(Az + alfa2)*cos(Ax)*cos(alfa2)^2 - 2*O2(3)*sin(Az + alfa2)*cos(Ax)*sin(Ay)^2*cos(alfa2)^2 + 2*O2(3)*sin(Az + alfa2)*cos(Ax)^3*cos(Ay)^2*cos(alfa2)^2 + b*cos(Ay)^2*sin(Ax)*sin(Ay)^2*cos(alfa2) - 2*b*sin(Az + alfa2)*cos(Ay)*sin(Ay)*cos(alfa2) + 2*O2(1)*sin(Az + alfa2)*cos(Ax)*cos(Ay)^2*sin(Ay) + b*cos(Ax)*cos(Ay)*sin(Ay)*cos(alfa2) + 4*O2(3)*sin(Az + alfa2)*cos(Ax)^2*cos(Ay)*cos(alfa2)^2 - 2*O2(3)*sin(Az + alfa2)*cos(Ax)^2*cos(Ay)*sin(Ay)^2*cos(alfa2)^2 - 2*b*sin(Az + alfa2)*cos(Ax)*cos(Ay)^2*sin(Ay)*cos(alfa2) + 2*O2(3)*cos(Az + alfa2)*cos(Ax)^2*cos(Ay)^2*sin(Ax)*sin(Ay)*cos(alfa2)^2 + 2*O2(3)*cos(Az + alfa2)*cos(Ax)*cos(Ay)*sin(Ax)*sin(Ay)*cos(alfa2)^2))/(2*l1*cos(alfa2)*(cos(Ax)*cos(Ay) + 1)^2*(O2(1)*sin(th2) + O2(3)*cos(alfa2)*cos(th2) - b*cos(alfa2)*sin(th2))^2), dAx*((cos(Ax)*((p*cos(alfa2)*(cos(Az + alfa2)*sin(Ax) + sin(Az + alfa2)*cos(Ax)*sin(Ay))*(O2(3) + l1*sin(th2)))/(l1*(O2(1)*sin(th2) + O2(3)*cos(alfa2)*cos(th2) - b*cos(alfa2)*sin(th2))) + (p*sin(Az + alfa2)*cos(Ay)*(2*b*cos(alfa2) - 2*O2(1) + 2*l1*cos(alfa2)*cos(th2)))/(2*l1*cos(alfa2)*(O2(1)*sin(th2) + O2(3)*cos(alfa2)*cos(th2) - b*cos(alfa2)*sin(th2)))))/(cos(Ax)*cos(Ay) + 1) + (cos(Ay)*sin(Ax)^2*((p*cos(alfa2)*(cos(Az + alfa2)*sin(Ax) + sin(Az + alfa2)*cos(Ax)*sin(Ay))*(O2(3) + l1*sin(th2)))/(l1*(O2(1)*sin(th2) + O2(3)*cos(alfa2)*cos(th2) - b*cos(alfa2)*sin(th2))) + (p*sin(Az + alfa2)*cos(Ay)*(2*b*cos(alfa2) - 2*O2(1) + 2*l1*cos(alfa2)*cos(th2)))/(2*l1*cos(alfa2)*(O2(1)*sin(th2) + O2(3)*cos(alfa2)*cos(th2) - b*cos(alfa2)*sin(th2)))))/(cos(Ax)*cos(Ay) + 1)^2 - (p*cos(Az + alfa2)*cos(Ay)*sin(Ax)*cos(alfa2)*(O2(3) + l1*sin(th2)))/(l1*(O2(1)*sin(th2) + O2(3)*cos(alfa2)*cos(th2) - b*cos(alfa2)*sin(th2))) + (p*sin(Ax)*cos(alfa2)*(cos(Az + alfa2)*cos(Ax) - sin(Az + alfa2)*sin(Ax)*sin(Ay))*(O2(3) + l1*sin(th2)))/(l1*(cos(Ax)*cos(Ay) + 1)*(O2(1)*sin(th2) + O2(3)*cos(alfa2)*cos(th2) - b*cos(alfa2)*sin(th2))) + (p*cos(Ay)*sin(Ax)*(sin(Ax) - cos(Ax)*sin(Ay))*(2*b*cos(alfa2) - 2*O2(1) + 2*l1*cos(alfa2)*cos(th2)))/(4*l1*cos(alfa2)*(cos(Ax)*cos(Ay) + 1)^2*(O2(1)*sin(th2) + O2(3)*cos(alfa2)*cos(th2) - b*cos(alfa2)*sin(th2))) - (p*cos(Ay)^2*sin(Ax)^2*(cos(Ax) + cos(Ay) + sin(Ax)*sin(Ay))*(2*b*cos(alfa2) - 2*O2(1) + 2*l1*cos(alfa2)*cos(th2)))/(2*l1*cos(alfa2)*(cos(Ax)*cos(Ay) + 1)^3*(O2(1)*sin(th2) + O2(3)*cos(alfa2)*cos(th2) - b*cos(alfa2)*sin(th2))) - (p*cos(Ax)*cos(Ay)*(cos(Ax) + cos(Ay) + sin(Ax)*sin(Ay))*(2*b*cos(alfa2) - 2*O2(1) + 2*l1*cos(alfa2)*cos(th2)))/(4*l1*cos(alfa2)*(cos(Ax)*cos(Ay) + 1)^2*(O2(1)*sin(th2) + O2(3)*cos(alfa2)*cos(th2) - b*cos(alfa2)*sin(th2)))) - dAz*((sin(Ax)*((p*cos(alfa2)*(sin(Az + alfa2)*sin(Ax) - cos(Az + alfa2)*cos(Ax)*sin(Ay))*(O2(3) + l1*sin(th2)))/(l1*(O2(1)*sin(th2) + O2(3)*cos(alfa2)*cos(th2) - b*cos(alfa2)*sin(th2))) - (p*cos(Az + alfa2)*cos(Ay)*(2*b*cos(alfa2) - 2*O2(1) + 2*l1*cos(alfa2)*cos(th2)))/(2*l1*cos(alfa2)*(O2(1)*sin(th2) + O2(3)*cos(alfa2)*cos(th2) - b*cos(alfa2)*sin(th2)))))/(cos(Ax)*cos(Ay) + 1) - (p*sin(Az + alfa2)*sin(Ay)*(2*b*cos(alfa2) - 2*O2(1) + 2*l1*cos(alfa2)*cos(th2)))/(2*l1*cos(alfa2)*(O2(1)*sin(th2) + O2(3)*cos(alfa2)*cos(th2) - b*cos(alfa2)*sin(th2))) + (p*sin(Az + alfa2)*cos(Ax)*cos(Ay)*cos(alfa2)*(O2(3) + l1*sin(th2)))/(l1*(O2(1)*sin(th2) + O2(3)*cos(alfa2)*cos(th2) - b*cos(alfa2)*sin(th2)))) + dAy*((cos(Ax)*sin(Ax)*sin(Ay)*((p*cos(alfa2)*(cos(Az + alfa2)*sin(Ax) + sin(Az + alfa2)*cos(Ax)*sin(Ay))*(O2(3) + l1*sin(th2)))/(l1*(O2(1)*sin(th2) + O2(3)*cos(alfa2)*cos(th2) - b*cos(alfa2)*sin(th2))) + (p*sin(Az + alfa2)*cos(Ay)*(2*b*cos(alfa2) - 2*O2(1) + 2*l1*cos(alfa2)*cos(th2)))/(2*l1*cos(alfa2)*(O2(1)*sin(th2) + O2(3)*cos(alfa2)*cos(th2) - b*cos(alfa2)*sin(th2)))))/(cos(Ax)*cos(Ay) + 1)^2 - (p*cos(Az + alfa2)*cos(Ay)*(2*b*cos(alfa2) - 2*O2(1) + 2*l1*cos(alfa2)*cos(th2)))/(2*l1*cos(alfa2)*(O2(1)*sin(th2) + O2(3)*cos(alfa2)*cos(th2) - b*cos(alfa2)*sin(th2))) - (p*cos(Az + alfa2)*cos(Ax)*sin(Ay)*cos(alfa2)*(O2(3) + l1*sin(th2)))/(l1*(O2(1)*sin(th2) + O2(3)*cos(alfa2)*cos(th2) - b*cos(alfa2)*sin(th2))) + (p*sin(Az + alfa2)*sin(Ax)*(O2(1)*sin(Ay) - b*sin(Ay)*cos(alfa2) + O2(3)*cos(Ax)*cos(Ay)*cos(alfa2)^2 - l1*sin(Ay)*cos(alfa2)*cos(th2) + l1*cos(Ax)*cos(Ay)*cos(alfa2)^2*sin(th2)))/(l1*cos(alfa2)*(cos(Ax)*cos(Ay) + 1)*(O2(1)*sin(th2) + O2(3)*cos(alfa2)*cos(th2) - b*cos(alfa2)*sin(th2))) + (p*sin(Ax)*sin(Ay)*(cos(Ax) + cos(Ay) + sin(Ax)*sin(Ay))*(2*b*cos(alfa2) - 2*O2(1) + 2*l1*cos(alfa2)*cos(th2)))/(4*l1*cos(alfa2)*(cos(Ax)*cos(Ay) + 1)^2*(O2(1)*sin(th2) + O2(3)*cos(alfa2)*cos(th2) - b*cos(alfa2)*sin(th2))) + (p*cos(Ay)*sin(Ax)*(sin(Ay) - cos(Ay)*sin(Ax))*(2*b*cos(alfa2) - 2*O2(1) + 2*l1*cos(alfa2)*cos(th2)))/(4*l1*cos(alfa2)*(cos(Ax)*cos(Ay) + 1)^2*(O2(1)*sin(th2) + O2(3)*cos(alfa2)*cos(th2) - b*cos(alfa2)*sin(th2))) - (p*cos(Ax)*cos(Ay)*sin(Ax)*sin(Ay)*(cos(Ax) + cos(Ay) + sin(Ax)*sin(Ay))*(2*b*cos(alfa2) - 2*O2(1) + 2*l1*cos(alfa2)*cos(th2)))/(2*l1*cos(alfa2)*(cos(Ax)*cos(Ay) + 1)^3*(O2(1)*sin(th2) + O2(3)*cos(alfa2)*cos(th2) - b*cos(alfa2)*sin(th2)))) - (dO2(3)*p*(b*cos(alfa2) - O2(1) + l1*cos(alfa2)*cos(th2))*(2*sin(Az + alfa2)*cos(Ay)*sin(Ax)*cos(th2) - cos(Ay)^2*sin(Ax)*cos(th2) - 2*cos(Az + alfa2)*sin(Ay)*cos(th2) - cos(Ax)*cos(Ay)*sin(Ax)*cos(th2) + 2*cos(Az + alfa2)*sin(Ax)^2*cos(alfa2)*sin(th2) - cos(Ay)*sin(Ax)^2*sin(Ay)*cos(th2) + 2*sin(Az + alfa2)*cos(Ax)*cos(Ay)^2*sin(Ax)*cos(th2) - 2*cos(Az + alfa2)*cos(Ax)^2*cos(Ay)^2*sin(Ay)*cos(th2) + 4*cos(Az + alfa2)*cos(Ax)^2*cos(Ay)^2*cos(alfa2)*sin(th2) + 2*cos(Az + alfa2)*cos(Ax)^3*cos(Ay)^3*cos(alfa2)*sin(th2) - 4*cos(Az + alfa2)*cos(Ax)*cos(Ay)*sin(Ay)*cos(th2) + 2*cos(Az + alfa2)*cos(Ax)*cos(Ay)*cos(alfa2)*sin(th2) + 2*sin(Az + alfa2)*cos(Ax)*sin(Ax)*sin(Ay)*cos(alfa2)*sin(th2) + 2*cos(Az + alfa2)*cos(Ax)*cos(Ay)*sin(Ax)^2*cos(alfa2)*sin(th2) + 2*sin(Az + alfa2)*cos(Ax)^2*cos(Ay)*sin(Ax)*sin(Ay)*cos(alfa2)*sin(th2)))/(2*l1*(cos(Ax)*cos(Ay) + 1)^2*(O2(1)*sin(th2) + O2(3)*cos(alfa2)*cos(th2) - b*cos(alfa2)*sin(th2))^2) - (dO2(1)*p*(O2(3) + l1*sin(th2))*(2*sin(Az + alfa2)*cos(Ay)*sin(Ax)*cos(th2) - cos(Ay)^2*sin(Ax)*cos(th2) - 2*cos(Az + alfa2)*sin(Ay)*cos(th2) - cos(Ax)*cos(Ay)*sin(Ax)*cos(th2) + 2*cos(Az + alfa2)*sin(Ax)^2*cos(alfa2)*sin(th2) - cos(Ay)*sin(Ax)^2*sin(Ay)*cos(th2) + 2*sin(Az + alfa2)*cos(Ax)*cos(Ay)^2*sin(Ax)*cos(th2) - 2*cos(Az + alfa2)*cos(Ax)^2*cos(Ay)^2*sin(Ay)*cos(th2) + 4*cos(Az + alfa2)*cos(Ax)^2*cos(Ay)^2*cos(alfa2)*sin(th2) + 2*cos(Az + alfa2)*cos(Ax)^3*cos(Ay)^3*cos(alfa2)*sin(th2) - 4*cos(Az + alfa2)*cos(Ax)*cos(Ay)*sin(Ay)*cos(th2) + 2*cos(Az + alfa2)*cos(Ax)*cos(Ay)*cos(alfa2)*sin(th2) + 2*sin(Az + alfa2)*cos(Ax)*sin(Ax)*sin(Ay)*cos(alfa2)*sin(th2) + 2*cos(Az + alfa2)*cos(Ax)*cos(Ay)*sin(Ax)^2*cos(alfa2)*sin(th2) + 2*sin(Az + alfa2)*cos(Ax)^2*cos(Ay)*sin(Ax)*sin(Ay)*cos(alfa2)*sin(th2)))/(2*l1*(cos(Ax)*cos(Ay) + 1)^2*(O2(1)*sin(th2) + O2(3)*cos(alfa2)*cos(th2) - b*cos(alfa2)*sin(th2))^2) + (dth2*p*(l1*cos(alfa2) - O2(1)*cos(th2) + O2(3)*cos(alfa2)*sin(th2) + b*cos(alfa2)*cos(th2))*(O2(1)*cos(Ay)^2*sin(Ax) + 2*O2(1)*cos(Az + alfa2)*sin(Ay) + O2(1)*cos(Ay)*sin(Ax)^2*sin(Ay) - b*cos(Ay)^2*sin(Ax)*cos(alfa2) + 2*O2(3)*cos(Az + alfa2)*sin(Ax)^2*cos(alfa2)^2 - 2*O2(1)*sin(Az + alfa2)*cos(Ay)*sin(Ax) - 2*b*cos(Az + alfa2)*sin(Ay)*cos(alfa2) + O2(1)*cos(Ax)*cos(Ay)*sin(Ax) + 4*O2(1)*cos(Az + alfa2)*cos(Ax)*cos(Ay)*sin(Ay) + 4*O2(3)*cos(Az + alfa2)*cos(Ax)^2*cos(Ay)^2*cos(alfa2)^2 + 2*O2(3)*cos(Az + alfa2)*cos(Ax)^3*cos(Ay)^3*cos(alfa2)^2 + 2*b*sin(Az + alfa2)*cos(Ay)*sin(Ax)*cos(alfa2) - 2*O2(1)*sin(Az + alfa2)*cos(Ax)*cos(Ay)^2*sin(Ax) + 2*O2(3)*cos(Az + alfa2)*cos(Ax)*cos(Ay)*cos(alfa2)^2 - b*cos(Ax)*cos(Ay)*sin(Ax)*cos(alfa2) + 2*O2(1)*cos(Az + alfa2)*cos(Ax)^2*cos(Ay)^2*sin(Ay) - b*cos(Ay)*sin(Ax)^2*sin(Ay)*cos(alfa2) + 2*O2(3)*sin(Az + alfa2)*cos(Ax)*sin(Ax)*sin(Ay)*cos(alfa2)^2 + 2*b*sin(Az + alfa2)*cos(Ax)*cos(Ay)^2*sin(Ax)*cos(alfa2) + 2*O2(3)*cos(Az + alfa2)*cos(Ax)*cos(Ay)*sin(Ax)^2*cos(alfa2)^2 - 2*b*cos(Az + alfa2)*cos(Ax)^2*cos(Ay)^2*sin(Ay)*cos(alfa2) - 4*b*cos(Az + alfa2)*cos(Ax)*cos(Ay)*sin(Ay)*cos(alfa2) + 2*O2(3)*sin(Az + alfa2)*cos(Ax)^2*cos(Ay)*sin(Ax)*sin(Ay)*cos(alfa2)^2))/(2*l1*cos(alfa2)*(cos(Ax)*cos(Ay) + 1)^2*(O2(1)*sin(th2) + O2(3)*cos(alfa2)*cos(th2) - b*cos(alfa2)*sin(th2))^2)
       (cos(alfa3)*(dO3(1)*l1 - dO3(1)*l1*cos(th3)^2 - O3(1)*dO3(3)*sin(th3) + O3(3)*dO3(1)*sin(th3) - O3(3)^2*dth3*cos(alfa3)*sin(th3) + O3(1)*O3(3)*dth3*cos(th3) - O3(3)*dth3*l1*cos(alfa3) + b*dO3(3)*cos(alfa3)*sin(th3) - O3(3)*b*dth3*cos(alfa3)*cos(th3) + dO3(3)*l1*cos(alfa3)*cos(th3)*sin(th3)))/(l1*(O3(1)*sin(th3) + O3(3)*cos(alfa3)*cos(th3) - b*cos(alfa3)*sin(th3))^2), dAx*((cos(Ay)*sin(Ax)*sin(Ay)*((p*cos(alfa3)*(cos(Az + alfa3)*sin(Ax) + sin(Az + alfa3)*cos(Ax)*sin(Ay))*(O3(3) + l1*sin(th3)))/(l1*(O3(1)*sin(th3) + O3(3)*cos(alfa3)*cos(th3) - b*cos(alfa3)*sin(th3))) + (p*sin(Az + alfa3)*cos(Ay)*(2*b*cos(alfa3) - 2*O3(1) + 2*l1*cos(alfa3)*cos(th3)))/(2*l1*cos(alfa3)*(O3(1)*sin(th3) + O3(3)*cos(alfa3)*cos(th3) - b*cos(alfa3)*sin(th3)))))/(cos(Ax)*cos(Ay) + 1)^2 + (p*cos(alfa3)*(sin(Az + alfa3)*sin(Ax) - cos(Az + alfa3)*cos(Ax)*sin(Ay))*(O3(3) + l1*sin(th3)))/(l1*(O3(1)*sin(th3) + O3(3)*cos(alfa3)*cos(th3) - b*cos(alfa3)*sin(th3))) + (p*sin(Ay)*cos(alfa3)*(cos(Az + alfa3)*cos(Ax) - sin(Az + alfa3)*sin(Ax)*sin(Ay))*(O3(3) + l1*sin(th3)))/(l1*(cos(Ax)*cos(Ay) + 1)*(O3(1)*sin(th3) + O3(3)*cos(alfa3)*cos(th3) - b*cos(alfa3)*sin(th3))) + (p*cos(Ay)*sin(Ay)*(sin(Ax) - cos(Ax)*cos(Ay)*sin(Ay))*(2*b*cos(alfa3) - 2*O3(1) + 2*l1*cos(alfa3)*cos(th3)))/(4*l1*cos(alfa3)*(cos(Ax)*cos(Ay) + 1)^2*(O3(1)*sin(th3) + O3(3)*cos(alfa3)*cos(th3) - b*cos(alfa3)*sin(th3))) - (p*cos(Ay)^2*sin(Ax)*sin(Ay)*(cos(Ax) + cos(Ay)*sin(Ax)*sin(Ay))*(2*b*cos(alfa3) - 2*O3(1) + 2*l1*cos(alfa3)*cos(th3)))/(2*l1*cos(alfa3)*(cos(Ax)*cos(Ay) + 1)^3*(O3(1)*sin(th3) + O3(3)*cos(alfa3)*cos(th3) - b*cos(alfa3)*sin(th3)))) - dAz*((sin(Ay)*((p*cos(alfa3)*(sin(Az + alfa3)*sin(Ax) - cos(Az + alfa3)*cos(Ax)*sin(Ay))*(O3(3) + l1*sin(th3)))/(l1*(O3(1)*sin(th3) + O3(3)*cos(alfa3)*cos(th3) - b*cos(alfa3)*sin(th3))) - (p*cos(Az + alfa3)*cos(Ay)*(2*b*cos(alfa3) - 2*O3(1) + 2*l1*cos(alfa3)*cos(th3)))/(2*l1*cos(alfa3)*(O3(1)*sin(th3) + O3(3)*cos(alfa3)*cos(th3) - b*cos(alfa3)*sin(th3)))))/(cos(Ax)*cos(Ay) + 1) + (p*cos(alfa3)*(cos(Az + alfa3)*cos(Ax) - sin(Az + alfa3)*sin(Ax)*sin(Ay))*(O3(3) + l1*sin(th3)))/(l1*(O3(1)*sin(th3) + O3(3)*cos(alfa3)*cos(th3) - b*cos(alfa3)*sin(th3)))) + dAy*((cos(Ay)*((p*cos(alfa3)*(cos(Az + alfa3)*sin(Ax) + sin(Az + alfa3)*cos(Ax)*sin(Ay))*(O3(3) + l1*sin(th3)))/(l1*(O3(1)*sin(th3) + O3(3)*cos(alfa3)*cos(th3) - b*cos(alfa3)*sin(th3))) + (p*sin(Az + alfa3)*cos(Ay)*(2*b*cos(alfa3) - 2*O3(1) + 2*l1*cos(alfa3)*cos(th3)))/(2*l1*cos(alfa3)*(O3(1)*sin(th3) + O3(3)*cos(alfa3)*cos(th3) - b*cos(alfa3)*sin(th3)))))/(cos(Ax)*cos(Ay) + 1) + (cos(Ax)*sin(Ay)^2*((p*cos(alfa3)*(cos(Az + alfa3)*sin(Ax) + sin(Az + alfa3)*cos(Ax)*sin(Ay))*(O3(3) + l1*sin(th3)))/(l1*(O3(1)*sin(th3) + O3(3)*cos(alfa3)*cos(th3) - b*cos(alfa3)*sin(th3))) + (p*sin(Az + alfa3)*cos(Ay)*(2*b*cos(alfa3) - 2*O3(1) + 2*l1*cos(alfa3)*cos(th3)))/(2*l1*cos(alfa3)*(O3(1)*sin(th3) + O3(3)*cos(alfa3)*cos(th3) - b*cos(alfa3)*sin(th3)))))/(cos(Ax)*cos(Ay) + 1)^2 - (p*cos(Az + alfa3)*cos(Ay)*sin(Ax)*cos(alfa3)*(O3(3) + l1*sin(th3)))/(l1*(O3(1)*sin(th3) + O3(3)*cos(alfa3)*cos(th3) - b*cos(alfa3)*sin(th3))) - (p*cos(Ay)^2*(cos(Ax) + cos(Ay)*sin(Ax)*sin(Ay))*(2*b*cos(alfa3) - 2*O3(1) + 2*l1*cos(alfa3)*cos(th3)))/(4*l1*cos(alfa3)*(cos(Ax)*cos(Ay) + 1)^2*(O3(1)*sin(th3) + O3(3)*cos(alfa3)*cos(th3) - b*cos(alfa3)*sin(th3))) + (p*sin(Ay)^2*(cos(Ax) + cos(Ay)*sin(Ax)*sin(Ay))*(2*b*cos(alfa3) - 2*O3(1) + 2*l1*cos(alfa3)*cos(th3)))/(4*l1*cos(alfa3)*(cos(Ax)*cos(Ay) + 1)^2*(O3(1)*sin(th3) + O3(3)*cos(alfa3)*cos(th3) - b*cos(alfa3)*sin(th3))) + (p*sin(Az + alfa3)*sin(Ay)*(O3(1)*sin(Ay) - b*sin(Ay)*cos(alfa3) + O3(3)*cos(Ax)*cos(Ay)*cos(alfa3)^2 - l1*sin(Ay)*cos(alfa3)*cos(th3) + l1*cos(Ax)*cos(Ay)*cos(alfa3)^2*sin(th3)))/(l1*cos(alfa3)*(cos(Ax)*cos(Ay) + 1)*(O3(1)*sin(th3) + O3(3)*cos(alfa3)*cos(th3) - b*cos(alfa3)*sin(th3))) - (p*cos(Ax)*cos(Ay)*sin(Ay)^2*(cos(Ax) + cos(Ay)*sin(Ax)*sin(Ay))*(2*b*cos(alfa3) - 2*O3(1) + 2*l1*cos(alfa3)*cos(th3)))/(2*l1*cos(alfa3)*(cos(Ax)*cos(Ay) + 1)^3*(O3(1)*sin(th3) + O3(3)*cos(alfa3)*cos(th3) - b*cos(alfa3)*sin(th3))) - (p*cos(Ay)*sin(Ax)*sin(Ay)*(2*cos(Ay)^2 - 1)*(2*b*cos(alfa3) - 2*O3(1) + 2*l1*cos(alfa3)*cos(th3)))/(4*l1*cos(alfa3)*(cos(Ax)*cos(Ay) + 1)^2*(O3(1)*sin(th3) + O3(3)*cos(alfa3)*cos(th3) - b*cos(alfa3)*sin(th3)))) + (dO3(3)*p*(b*cos(alfa3) - O3(1) + l1*cos(alfa3)*cos(th3))*(cos(Ay)^2*sin(Ax)*sin(Ay)^2*cos(th3) - 2*sin(Az + alfa3)*cos(Ay)*sin(Ay)*cos(th3) + 2*sin(Az + alfa3)*cos(Ax)*cos(alfa3)*sin(th3) + cos(Ax)*cos(Ay)*sin(Ay)*cos(th3) - 2*sin(Az + alfa3)*cos(Ax)*cos(Ay)^2*sin(Ay)*cos(th3) + 4*sin(Az + alfa3)*cos(Ax)^2*cos(Ay)*cos(alfa3)*sin(th3) - 2*sin(Az + alfa3)*cos(Ax)*sin(Ay)^2*cos(alfa3)*sin(th3) + 2*sin(Az + alfa3)*cos(Ax)^3*cos(Ay)^2*cos(alfa3)*sin(th3) - 2*sin(Az + alfa3)*cos(Ax)^2*cos(Ay)*sin(Ay)^2*cos(alfa3)*sin(th3) + 2*cos(Az + alfa3)*cos(Ax)*cos(Ay)*sin(Ax)*sin(Ay)*cos(alfa3)*sin(th3) + 2*cos(Az + alfa3)*cos(Ax)^2*cos(Ay)^2*sin(Ax)*sin(Ay)*cos(alfa3)*sin(th3)))/(2*l1*(cos(Ax)*cos(Ay) + 1)^2*(O3(1)*sin(th3) + O3(3)*cos(alfa3)*cos(th3) - b*cos(alfa3)*sin(th3))^2) + (dO3(1)*p*(O3(3) + l1*sin(th3))*(cos(Ay)^2*sin(Ax)*sin(Ay)^2*cos(th3) - 2*sin(Az + alfa3)*cos(Ay)*sin(Ay)*cos(th3) + 2*sin(Az + alfa3)*cos(Ax)*cos(alfa3)*sin(th3) + cos(Ax)*cos(Ay)*sin(Ay)*cos(th3) - 2*sin(Az + alfa3)*cos(Ax)*cos(Ay)^2*sin(Ay)*cos(th3) + 4*sin(Az + alfa3)*cos(Ax)^2*cos(Ay)*cos(alfa3)*sin(th3) - 2*sin(Az + alfa3)*cos(Ax)*sin(Ay)^2*cos(alfa3)*sin(th3) + 2*sin(Az + alfa3)*cos(Ax)^3*cos(Ay)^2*cos(alfa3)*sin(th3) - 2*sin(Az + alfa3)*cos(Ax)^2*cos(Ay)*sin(Ay)^2*cos(alfa3)*sin(th3) + 2*cos(Az + alfa3)*cos(Ax)*cos(Ay)*sin(Ax)*sin(Ay)*cos(alfa3)*sin(th3) + 2*cos(Az + alfa3)*cos(Ax)^2*cos(Ay)^2*sin(Ax)*sin(Ay)*cos(alfa3)*sin(th3)))/(2*l1*(cos(Ax)*cos(Ay) + 1)^2*(O3(1)*sin(th3) + O3(3)*cos(alfa3)*cos(th3) - b*cos(alfa3)*sin(th3))^2) - (dth3*p*(l1*cos(alfa3) - O3(1)*cos(th3) + O3(3)*cos(alfa3)*sin(th3) + b*cos(alfa3)*cos(th3))*(2*O3(1)*sin(Az + alfa3)*cos(Ay)*sin(Ay) - O3(1)*cos(Ax)*cos(Ay)*sin(Ay) + O3(1)*sin(Ax)*sin(Ay)^2*(sin(Ay)^2 - 1) + 2*O3(3)*sin(Az + alfa3)*cos(Ax)*cos(alfa3)^2 - 2*O3(3)*sin(Az + alfa3)*cos(Ax)*sin(Ay)^2*cos(alfa3)^2 + 2*O3(3)*sin(Az + alfa3)*cos(Ax)^3*cos(Ay)^2*cos(alfa3)^2 + b*cos(Ay)^2*sin(Ax)*sin(Ay)^2*cos(alfa3) - 2*b*sin(Az + alfa3)*cos(Ay)*sin(Ay)*cos(alfa3) + 2*O3(1)*sin(Az + alfa3)*cos(Ax)*cos(Ay)^2*sin(Ay) + b*cos(Ax)*cos(Ay)*sin(Ay)*cos(alfa3) + 4*O3(3)*sin(Az + alfa3)*cos(Ax)^2*cos(Ay)*cos(alfa3)^2 - 2*O3(3)*sin(Az + alfa3)*cos(Ax)^2*cos(Ay)*sin(Ay)^2*cos(alfa3)^2 - 2*b*sin(Az + alfa3)*cos(Ax)*cos(Ay)^2*sin(Ay)*cos(alfa3) + 2*O3(3)*cos(Az + alfa3)*cos(Ax)^2*cos(Ay)^2*sin(Ax)*sin(Ay)*cos(alfa3)^2 + 2*O3(3)*cos(Az + alfa3)*cos(Ax)*cos(Ay)*sin(Ax)*sin(Ay)*cos(alfa3)^2))/(2*l1*cos(alfa3)*(cos(Ax)*cos(Ay) + 1)^2*(O3(1)*sin(th3) + O3(3)*cos(alfa3)*cos(th3) - b*cos(alfa3)*sin(th3))^2), dAx*((cos(Ax)*((p*cos(alfa3)*(cos(Az + alfa3)*sin(Ax) + sin(Az + alfa3)*cos(Ax)*sin(Ay))*(O3(3) + l1*sin(th3)))/(l1*(O3(1)*sin(th3) + O3(3)*cos(alfa3)*cos(th3) - b*cos(alfa3)*sin(th3))) + (p*sin(Az + alfa3)*cos(Ay)*(2*b*cos(alfa3) - 2*O3(1) + 2*l1*cos(alfa3)*cos(th3)))/(2*l1*cos(alfa3)*(O3(1)*sin(th3) + O3(3)*cos(alfa3)*cos(th3) - b*cos(alfa3)*sin(th3)))))/(cos(Ax)*cos(Ay) + 1) + (cos(Ay)*sin(Ax)^2*((p*cos(alfa3)*(cos(Az + alfa3)*sin(Ax) + sin(Az + alfa3)*cos(Ax)*sin(Ay))*(O3(3) + l1*sin(th3)))/(l1*(O3(1)*sin(th3) + O3(3)*cos(alfa3)*cos(th3) - b*cos(alfa3)*sin(th3))) + (p*sin(Az + alfa3)*cos(Ay)*(2*b*cos(alfa3) - 2*O3(1) + 2*l1*cos(alfa3)*cos(th3)))/(2*l1*cos(alfa3)*(O3(1)*sin(th3) + O3(3)*cos(alfa3)*cos(th3) - b*cos(alfa3)*sin(th3)))))/(cos(Ax)*cos(Ay) + 1)^2 - (p*cos(Az + alfa3)*cos(Ay)*sin(Ax)*cos(alfa3)*(O3(3) + l1*sin(th3)))/(l1*(O3(1)*sin(th3) + O3(3)*cos(alfa3)*cos(th3) - b*cos(alfa3)*sin(th3))) + (p*sin(Ax)*cos(alfa3)*(cos(Az + alfa3)*cos(Ax) - sin(Az + alfa3)*sin(Ax)*sin(Ay))*(O3(3) + l1*sin(th3)))/(l1*(cos(Ax)*cos(Ay) + 1)*(O3(1)*sin(th3) + O3(3)*cos(alfa3)*cos(th3) - b*cos(alfa3)*sin(th3))) + (p*cos(Ay)*sin(Ax)*(sin(Ax) - cos(Ax)*sin(Ay))*(2*b*cos(alfa3) - 2*O3(1) + 2*l1*cos(alfa3)*cos(th3)))/(4*l1*cos(alfa3)*(cos(Ax)*cos(Ay) + 1)^2*(O3(1)*sin(th3) + O3(3)*cos(alfa3)*cos(th3) - b*cos(alfa3)*sin(th3))) - (p*cos(Ay)^2*sin(Ax)^2*(cos(Ax) + cos(Ay) + sin(Ax)*sin(Ay))*(2*b*cos(alfa3) - 2*O3(1) + 2*l1*cos(alfa3)*cos(th3)))/(2*l1*cos(alfa3)*(cos(Ax)*cos(Ay) + 1)^3*(O3(1)*sin(th3) + O3(3)*cos(alfa3)*cos(th3) - b*cos(alfa3)*sin(th3))) - (p*cos(Ax)*cos(Ay)*(cos(Ax) + cos(Ay) + sin(Ax)*sin(Ay))*(2*b*cos(alfa3) - 2*O3(1) + 2*l1*cos(alfa3)*cos(th3)))/(4*l1*cos(alfa3)*(cos(Ax)*cos(Ay) + 1)^2*(O3(1)*sin(th3) + O3(3)*cos(alfa3)*cos(th3) - b*cos(alfa3)*sin(th3)))) - dAz*((sin(Ax)*((p*cos(alfa3)*(sin(Az + alfa3)*sin(Ax) - cos(Az + alfa3)*cos(Ax)*sin(Ay))*(O3(3) + l1*sin(th3)))/(l1*(O3(1)*sin(th3) + O3(3)*cos(alfa3)*cos(th3) - b*cos(alfa3)*sin(th3))) - (p*cos(Az + alfa3)*cos(Ay)*(2*b*cos(alfa3) - 2*O3(1) + 2*l1*cos(alfa3)*cos(th3)))/(2*l1*cos(alfa3)*(O3(1)*sin(th3) + O3(3)*cos(alfa3)*cos(th3) - b*cos(alfa3)*sin(th3)))))/(cos(Ax)*cos(Ay) + 1) - (p*sin(Az + alfa3)*sin(Ay)*(2*b*cos(alfa3) - 2*O3(1) + 2*l1*cos(alfa3)*cos(th3)))/(2*l1*cos(alfa3)*(O3(1)*sin(th3) + O3(3)*cos(alfa3)*cos(th3) - b*cos(alfa3)*sin(th3))) + (p*sin(Az + alfa3)*cos(Ax)*cos(Ay)*cos(alfa3)*(O3(3) + l1*sin(th3)))/(l1*(O3(1)*sin(th3) + O3(3)*cos(alfa3)*cos(th3) - b*cos(alfa3)*sin(th3)))) + dAy*((cos(Ax)*sin(Ax)*sin(Ay)*((p*cos(alfa3)*(cos(Az + alfa3)*sin(Ax) + sin(Az + alfa3)*cos(Ax)*sin(Ay))*(O3(3) + l1*sin(th3)))/(l1*(O3(1)*sin(th3) + O3(3)*cos(alfa3)*cos(th3) - b*cos(alfa3)*sin(th3))) + (p*sin(Az + alfa3)*cos(Ay)*(2*b*cos(alfa3) - 2*O3(1) + 2*l1*cos(alfa3)*cos(th3)))/(2*l1*cos(alfa3)*(O3(1)*sin(th3) + O3(3)*cos(alfa3)*cos(th3) - b*cos(alfa3)*sin(th3)))))/(cos(Ax)*cos(Ay) + 1)^2 - (p*cos(Az + alfa3)*cos(Ay)*(2*b*cos(alfa3) - 2*O3(1) + 2*l1*cos(alfa3)*cos(th3)))/(2*l1*cos(alfa3)*(O3(1)*sin(th3) + O3(3)*cos(alfa3)*cos(th3) - b*cos(alfa3)*sin(th3))) - (p*cos(Az + alfa3)*cos(Ax)*sin(Ay)*cos(alfa3)*(O3(3) + l1*sin(th3)))/(l1*(O3(1)*sin(th3) + O3(3)*cos(alfa3)*cos(th3) - b*cos(alfa3)*sin(th3))) + (p*sin(Az + alfa3)*sin(Ax)*(O3(1)*sin(Ay) - b*sin(Ay)*cos(alfa3) + O3(3)*cos(Ax)*cos(Ay)*cos(alfa3)^2 - l1*sin(Ay)*cos(alfa3)*cos(th3) + l1*cos(Ax)*cos(Ay)*cos(alfa3)^2*sin(th3)))/(l1*cos(alfa3)*(cos(Ax)*cos(Ay) + 1)*(O3(1)*sin(th3) + O3(3)*cos(alfa3)*cos(th3) - b*cos(alfa3)*sin(th3))) + (p*sin(Ax)*sin(Ay)*(cos(Ax) + cos(Ay) + sin(Ax)*sin(Ay))*(2*b*cos(alfa3) - 2*O3(1) + 2*l1*cos(alfa3)*cos(th3)))/(4*l1*cos(alfa3)*(cos(Ax)*cos(Ay) + 1)^2*(O3(1)*sin(th3) + O3(3)*cos(alfa3)*cos(th3) - b*cos(alfa3)*sin(th3))) + (p*cos(Ay)*sin(Ax)*(sin(Ay) - cos(Ay)*sin(Ax))*(2*b*cos(alfa3) - 2*O3(1) + 2*l1*cos(alfa3)*cos(th3)))/(4*l1*cos(alfa3)*(cos(Ax)*cos(Ay) + 1)^2*(O3(1)*sin(th3) + O3(3)*cos(alfa3)*cos(th3) - b*cos(alfa3)*sin(th3))) - (p*cos(Ax)*cos(Ay)*sin(Ax)*sin(Ay)*(cos(Ax) + cos(Ay) + sin(Ax)*sin(Ay))*(2*b*cos(alfa3) - 2*O3(1) + 2*l1*cos(alfa3)*cos(th3)))/(2*l1*cos(alfa3)*(cos(Ax)*cos(Ay) + 1)^3*(O3(1)*sin(th3) + O3(3)*cos(alfa3)*cos(th3) - b*cos(alfa3)*sin(th3)))) - (dO3(3)*p*(b*cos(alfa3) - O3(1) + l1*cos(alfa3)*cos(th3))*(2*sin(Az + alfa3)*cos(Ay)*sin(Ax)*cos(th3) - cos(Ay)^2*sin(Ax)*cos(th3) - 2*cos(Az + alfa3)*sin(Ay)*cos(th3) - cos(Ax)*cos(Ay)*sin(Ax)*cos(th3) + 2*cos(Az + alfa3)*sin(Ax)^2*cos(alfa3)*sin(th3) - cos(Ay)*sin(Ax)^2*sin(Ay)*cos(th3) + 2*sin(Az + alfa3)*cos(Ax)*cos(Ay)^2*sin(Ax)*cos(th3) - 2*cos(Az + alfa3)*cos(Ax)^2*cos(Ay)^2*sin(Ay)*cos(th3) + 4*cos(Az + alfa3)*cos(Ax)^2*cos(Ay)^2*cos(alfa3)*sin(th3) + 2*cos(Az + alfa3)*cos(Ax)^3*cos(Ay)^3*cos(alfa3)*sin(th3) - 4*cos(Az + alfa3)*cos(Ax)*cos(Ay)*sin(Ay)*cos(th3) + 2*cos(Az + alfa3)*cos(Ax)*cos(Ay)*cos(alfa3)*sin(th3) + 2*sin(Az + alfa3)*cos(Ax)*sin(Ax)*sin(Ay)*cos(alfa3)*sin(th3) + 2*cos(Az + alfa3)*cos(Ax)*cos(Ay)*sin(Ax)^2*cos(alfa3)*sin(th3) + 2*sin(Az + alfa3)*cos(Ax)^2*cos(Ay)*sin(Ax)*sin(Ay)*cos(alfa3)*sin(th3)))/(2*l1*(cos(Ax)*cos(Ay) + 1)^2*(O3(1)*sin(th3) + O3(3)*cos(alfa3)*cos(th3) - b*cos(alfa3)*sin(th3))^2) - (dO3(1)*p*(O3(3) + l1*sin(th3))*(2*sin(Az + alfa3)*cos(Ay)*sin(Ax)*cos(th3) - cos(Ay)^2*sin(Ax)*cos(th3) - 2*cos(Az + alfa3)*sin(Ay)*cos(th3) - cos(Ax)*cos(Ay)*sin(Ax)*cos(th3) + 2*cos(Az + alfa3)*sin(Ax)^2*cos(alfa3)*sin(th3) - cos(Ay)*sin(Ax)^2*sin(Ay)*cos(th3) + 2*sin(Az + alfa3)*cos(Ax)*cos(Ay)^2*sin(Ax)*cos(th3) - 2*cos(Az + alfa3)*cos(Ax)^2*cos(Ay)^2*sin(Ay)*cos(th3) + 4*cos(Az + alfa3)*cos(Ax)^2*cos(Ay)^2*cos(alfa3)*sin(th3) + 2*cos(Az + alfa3)*cos(Ax)^3*cos(Ay)^3*cos(alfa3)*sin(th3) - 4*cos(Az + alfa3)*cos(Ax)*cos(Ay)*sin(Ay)*cos(th3) + 2*cos(Az + alfa3)*cos(Ax)*cos(Ay)*cos(alfa3)*sin(th3) + 2*sin(Az + alfa3)*cos(Ax)*sin(Ax)*sin(Ay)*cos(alfa3)*sin(th3) + 2*cos(Az + alfa3)*cos(Ax)*cos(Ay)*sin(Ax)^2*cos(alfa3)*sin(th3) + 2*sin(Az + alfa3)*cos(Ax)^2*cos(Ay)*sin(Ax)*sin(Ay)*cos(alfa3)*sin(th3)))/(2*l1*(cos(Ax)*cos(Ay) + 1)^2*(O3(1)*sin(th3) + O3(3)*cos(alfa3)*cos(th3) - b*cos(alfa3)*sin(th3))^2) + (dth3*p*(l1*cos(alfa3) - O3(1)*cos(th3) + O3(3)*cos(alfa3)*sin(th3) + b*cos(alfa3)*cos(th3))*(O3(1)*cos(Ay)^2*sin(Ax) + 2*O3(1)*cos(Az + alfa3)*sin(Ay) + O3(1)*cos(Ay)*sin(Ax)^2*sin(Ay) - b*cos(Ay)^2*sin(Ax)*cos(alfa3) + 2*O3(3)*cos(Az + alfa3)*sin(Ax)^2*cos(alfa3)^2 - 2*O3(1)*sin(Az + alfa3)*cos(Ay)*sin(Ax) - 2*b*cos(Az + alfa3)*sin(Ay)*cos(alfa3) + O3(1)*cos(Ax)*cos(Ay)*sin(Ax) + 4*O3(1)*cos(Az + alfa3)*cos(Ax)*cos(Ay)*sin(Ay) + 4*O3(3)*cos(Az + alfa3)*cos(Ax)^2*cos(Ay)^2*cos(alfa3)^2 + 2*O3(3)*cos(Az + alfa3)*cos(Ax)^3*cos(Ay)^3*cos(alfa3)^2 + 2*b*sin(Az + alfa3)*cos(Ay)*sin(Ax)*cos(alfa3) - 2*O3(1)*sin(Az + alfa3)*cos(Ax)*cos(Ay)^2*sin(Ax) + 2*O3(3)*cos(Az + alfa3)*cos(Ax)*cos(Ay)*cos(alfa3)^2 - b*cos(Ax)*cos(Ay)*sin(Ax)*cos(alfa3) + 2*O3(1)*cos(Az + alfa3)*cos(Ax)^2*cos(Ay)^2*sin(Ay) - b*cos(Ay)*sin(Ax)^2*sin(Ay)*cos(alfa3) + 2*O3(3)*sin(Az + alfa3)*cos(Ax)*sin(Ax)*sin(Ay)*cos(alfa3)^2 + 2*b*sin(Az + alfa3)*cos(Ax)*cos(Ay)^2*sin(Ax)*cos(alfa3) + 2*O3(3)*cos(Az + alfa3)*cos(Ax)*cos(Ay)*sin(Ax)^2*cos(alfa3)^2 - 2*b*cos(Az + alfa3)*cos(Ax)^2*cos(Ay)^2*sin(Ay)*cos(alfa3) - 4*b*cos(Az + alfa3)*cos(Ax)*cos(Ay)*sin(Ay)*cos(alfa3) + 2*O3(3)*sin(Az + alfa3)*cos(Ax)^2*cos(Ay)*sin(Ax)*sin(Ay)*cos(alfa3)^2))/(2*l1*cos(alfa3)*(cos(Ax)*cos(Ay) + 1)^2*(O3(1)*sin(th3) + O3(3)*cos(alfa3)*cos(th3) - b*cos(alfa3)*sin(th3))^2)];

dJXPH=[-(O1(1)*O1(3)*dth1*cos(alfa1)*cos(phi1)*cos(th1)^2 - b^2*dphi1*cos(alfa1)^2*sin(phi1)*sin(th1)^2 - O1(1)^2*dphi1*sin(phi1)*sin(th1)^2 + O1(1)*O1(3)*dth1*cos(alfa1)*cos(phi1)*sin(th1)^2 + dO1(3)*l1*cos(alfa1)^2*cos(phi1)*cos(th1)^2*sin(th1) + O1(1)*dth1*l1*cos(alfa1)*cos(phi1)*sin(th1)^3 + 2*O1(1)*b*dphi1*cos(alfa1)*sin(phi1)*sin(th1)^2 - O1(1)*dO1(3)*cos(alfa1)*cos(phi1)*cos(th1)*sin(th1) + O1(3)*dO1(1)*cos(alfa1)*cos(phi1)*cos(th1)*sin(th1) - O1(3)*b*dth1*cos(alfa1)^2*cos(phi1)*cos(th1)^2 - O1(3)*dth1*l1*cos(alfa1)^2*cos(phi1)*cos(th1)^3 - O1(3)*b*dth1*cos(alfa1)^2*cos(phi1)*sin(th1)^2 - b*dth1*l1*cos(alfa1)^2*cos(phi1)*sin(th1)^3 + b*dO1(3)*cos(alfa1)^2*cos(phi1)*cos(th1)*sin(th1) + dO1(1)*l1*cos(alfa1)*cos(phi1)*cos(th1)*sin(th1)^2 + O1(3)*b*dphi1*cos(alfa1)^2*cos(th1)*sin(phi1)*sin(th1) + O1(1)*dphi1*l1*cos(alfa1)*cos(th1)*sin(phi1)*sin(th1)^2 + O1(3)*dphi1*l1*cos(alfa1)^2*cos(th1)^2*sin(phi1)*sin(th1) - b*dphi1*l1*cos(alfa1)^2*cos(th1)*sin(phi1)*sin(th1)^2 - O1(1)*O1(3)*dphi1*cos(alfa1)*cos(th1)*sin(phi1)*sin(th1))/(l2*(O1(1)*sin(th1) + O1(3)*cos(alfa1)*cos(th1) - b*cos(alfa1)*sin(th1))^2), dth1*((p*cos(phi1)*(b*cos(alfa1) - O1(1) + l1*cos(alfa1)*cos(th1))*(2*sin(Az + alfa1)*cos(Ax)*cos(alfa1)*cos(th1) - cos(Ay)^2*sin(Ax)*sin(Ay)^2*sin(th1) + 2*sin(Az + alfa1)*cos(Ay)*sin(Ay)*sin(th1) - cos(Ax)*cos(Ay)*sin(Ay)*sin(th1) + 4*sin(Az + alfa1)*cos(Ax)^2*cos(Ay)*cos(alfa1)*cos(th1) + 2*sin(Az + alfa1)*cos(Ax)*cos(Ay)^2*sin(Ay)*sin(th1) - 2*sin(Az + alfa1)*cos(Ax)*sin(Ay)^2*cos(alfa1)*cos(th1) + 2*sin(Az + alfa1)*cos(Ax)^3*cos(Ay)^2*cos(alfa1)*cos(th1) - 2*sin(Az + alfa1)*cos(Ax)^2*cos(Ay)*sin(Ay)^2*cos(alfa1)*cos(th1) + 2*cos(Az + alfa1)*cos(Ax)*cos(Ay)*sin(Ax)*sin(Ay)*cos(alfa1)*cos(th1) + 2*cos(Az + alfa1)*cos(Ax)^2*cos(Ay)^2*sin(Ax)*sin(Ay)*cos(alfa1)*cos(th1)))/(2*l2*cos(alfa1)*(cos(Ax)*cos(Ay) + 1)^2*(O1(1)*sin(th1) + O1(3)*cos(alfa1)*cos(th1) - b*cos(alfa1)*sin(th1))) - (l1*p*cos(phi1)*sin(th1)*(cos(Ay)^2*sin(Ax)*sin(Ay)^2*cos(th1) - 2*sin(Az + alfa1)*cos(Ay)*sin(Ay)*cos(th1) + 2*sin(Az + alfa1)*cos(Ax)*cos(alfa1)*sin(th1) + cos(Ax)*cos(Ay)*sin(Ay)*cos(th1) - 2*sin(Az + alfa1)*cos(Ax)*cos(Ay)^2*sin(Ay)*cos(th1) + 4*sin(Az + alfa1)*cos(Ax)^2*cos(Ay)*cos(alfa1)*sin(th1) - 2*sin(Az + alfa1)*cos(Ax)*sin(Ay)^2*cos(alfa1)*sin(th1) + 2*sin(Az + alfa1)*cos(Ax)^3*cos(Ay)^2*cos(alfa1)*sin(th1) - 2*sin(Az + alfa1)*cos(Ax)^2*cos(Ay)*sin(Ay)^2*cos(alfa1)*sin(th1) + 2*cos(Az + alfa1)*cos(Ax)*cos(Ay)*sin(Ax)*sin(Ay)*cos(alfa1)*sin(th1) + 2*cos(Az + alfa1)*cos(Ax)^2*cos(Ay)^2*sin(Ax)*sin(Ay)*cos(alfa1)*sin(th1)))/(2*l2*(cos(Ax)*cos(Ay) + 1)^2*(O1(1)*sin(th1) + O1(3)*cos(alfa1)*cos(th1) - b*cos(alfa1)*sin(th1))) + (p*cos(phi1)*(O1(3)*cos(alfa1)*sin(th1) - O1(1)*cos(th1) + b*cos(alfa1)*cos(th1))*(b*cos(alfa1) - O1(1) + l1*cos(alfa1)*cos(th1))*(cos(Ay)^2*sin(Ax)*sin(Ay)^2*cos(th1) - 2*sin(Az + alfa1)*cos(Ay)*sin(Ay)*cos(th1) + 2*sin(Az + alfa1)*cos(Ax)*cos(alfa1)*sin(th1) + cos(Ax)*cos(Ay)*sin(Ay)*cos(th1) - 2*sin(Az + alfa1)*cos(Ax)*cos(Ay)^2*sin(Ay)*cos(th1) + 4*sin(Az + alfa1)*cos(Ax)^2*cos(Ay)*cos(alfa1)*sin(th1) - 2*sin(Az + alfa1)*cos(Ax)*sin(Ay)^2*cos(alfa1)*sin(th1) + 2*sin(Az + alfa1)*cos(Ax)^3*cos(Ay)^2*cos(alfa1)*sin(th1) - 2*sin(Az + alfa1)*cos(Ax)^2*cos(Ay)*sin(Ay)^2*cos(alfa1)*sin(th1) + 2*cos(Az + alfa1)*cos(Ax)*cos(Ay)*sin(Ax)*sin(Ay)*cos(alfa1)*sin(th1) + 2*cos(Az + alfa1)*cos(Ax)^2*cos(Ay)^2*sin(Ax)*sin(Ay)*cos(alfa1)*sin(th1)))/(2*l2*cos(alfa1)*(cos(Ax)*cos(Ay) + 1)^2*(O1(1)*sin(th1) + O1(3)*cos(alfa1)*cos(th1) - b*cos(alfa1)*sin(th1))^2)) - (dO1(3)*p*cos(phi1)*cos(th1)*(b*cos(alfa1) - O1(1) + l1*cos(alfa1)*cos(th1))*(cos(Ay)^2*sin(Ax)*sin(Ay)^2*cos(th1) - 2*sin(Az + alfa1)*cos(Ay)*sin(Ay)*cos(th1) + 2*sin(Az + alfa1)*cos(Ax)*cos(alfa1)*sin(th1) + cos(Ax)*cos(Ay)*sin(Ay)*cos(th1) - 2*sin(Az + alfa1)*cos(Ax)*cos(Ay)^2*sin(Ay)*cos(th1) + 4*sin(Az + alfa1)*cos(Ax)^2*cos(Ay)*cos(alfa1)*sin(th1) - 2*sin(Az + alfa1)*cos(Ax)*sin(Ay)^2*cos(alfa1)*sin(th1) + 2*sin(Az + alfa1)*cos(Ax)^3*cos(Ay)^2*cos(alfa1)*sin(th1) - 2*sin(Az + alfa1)*cos(Ax)^2*cos(Ay)*sin(Ay)^2*cos(alfa1)*sin(th1) + 2*cos(Az + alfa1)*cos(Ax)*cos(Ay)*sin(Ax)*sin(Ay)*cos(alfa1)*sin(th1) + 2*cos(Az + alfa1)*cos(Ax)^2*cos(Ay)^2*sin(Ax)*sin(Ay)*cos(alfa1)*sin(th1)))/(2*l2*(cos(Ax)*cos(Ay) + 1)^2*(O1(1)*sin(th1) + O1(3)*cos(alfa1)*cos(th1) - b*cos(alfa1)*sin(th1))^2) - (dAz*p*cos(phi1)*(b*cos(alfa1) - O1(1) + l1*cos(alfa1)*cos(th1))*(cos(Az + alfa1)*cos(Ay)*sin(Ay)*cos(th1) - cos(Az + alfa1)*cos(Ax)*cos(alfa1)*sin(th1) - cos(Az + alfa1)*cos(Ax)^2*cos(Ay)*cos(alfa1)*sin(th1) + cos(Az + alfa1)*cos(Ax)*sin(Ay)^2*cos(alfa1)*sin(th1) + sin(Az + alfa1)*cos(Ax)*cos(Ay)*sin(Ax)*sin(Ay)*cos(alfa1)*sin(th1)))/(l2*cos(alfa1)*(cos(Ax)*cos(Ay) + 1)*(O1(1)*sin(th1) + O1(3)*cos(alfa1)*cos(th1) - b*cos(alfa1)*sin(th1))) - (dphi1*p*sin(phi1)*(b*cos(alfa1) - O1(1) + l1*cos(alfa1)*cos(th1))*(cos(Ay)^2*sin(Ax)*sin(Ay)^2*cos(th1) - 2*sin(Az + alfa1)*cos(Ay)*sin(Ay)*cos(th1) + 2*sin(Az + alfa1)*cos(Ax)*cos(alfa1)*sin(th1) + cos(Ax)*cos(Ay)*sin(Ay)*cos(th1) - 2*sin(Az + alfa1)*cos(Ax)*cos(Ay)^2*sin(Ay)*cos(th1) + 4*sin(Az + alfa1)*cos(Ax)^2*cos(Ay)*cos(alfa1)*sin(th1) - 2*sin(Az + alfa1)*cos(Ax)*sin(Ay)^2*cos(alfa1)*sin(th1) + 2*sin(Az + alfa1)*cos(Ax)^3*cos(Ay)^2*cos(alfa1)*sin(th1) - 2*sin(Az + alfa1)*cos(Ax)^2*cos(Ay)*sin(Ay)^2*cos(alfa1)*sin(th1) + 2*cos(Az + alfa1)*cos(Ax)*cos(Ay)*sin(Ax)*sin(Ay)*cos(alfa1)*sin(th1) + 2*cos(Az + alfa1)*cos(Ax)^2*cos(Ay)^2*sin(Ax)*sin(Ay)*cos(alfa1)*sin(th1)))/(2*l2*cos(alfa1)*(cos(Ax)*cos(Ay) + 1)^2*(O1(1)*sin(th1) + O1(3)*cos(alfa1)*cos(th1) - b*cos(alfa1)*sin(th1))) - (dO1(1)*p*cos(phi1)*cos(th1)*(O1(3) + l1*sin(th1))*(cos(Ay)^2*sin(Ax)*sin(Ay)^2*cos(th1) - 2*sin(Az + alfa1)*cos(Ay)*sin(Ay)*cos(th1) + 2*sin(Az + alfa1)*cos(Ax)*cos(alfa1)*sin(th1) + cos(Ax)*cos(Ay)*sin(Ay)*cos(th1) - 2*sin(Az + alfa1)*cos(Ax)*cos(Ay)^2*sin(Ay)*cos(th1) + 4*sin(Az + alfa1)*cos(Ax)^2*cos(Ay)*cos(alfa1)*sin(th1) - 2*sin(Az + alfa1)*cos(Ax)*sin(Ay)^2*cos(alfa1)*sin(th1) + 2*sin(Az + alfa1)*cos(Ax)^3*cos(Ay)^2*cos(alfa1)*sin(th1) - 2*sin(Az + alfa1)*cos(Ax)^2*cos(Ay)*sin(Ay)^2*cos(alfa1)*sin(th1) + 2*cos(Az + alfa1)*cos(Ax)*cos(Ay)*sin(Ax)*sin(Ay)*cos(alfa1)*sin(th1) + 2*cos(Az + alfa1)*cos(Ax)^2*cos(Ay)^2*sin(Ax)*sin(Ay)*cos(alfa1)*sin(th1)))/(2*l2*(cos(Ax)*cos(Ay) + 1)^2*(O1(1)*sin(th1) + O1(3)*cos(alfa1)*cos(th1) - b*cos(alfa1)*sin(th1))^2) - (dAy*p*cos(phi1)*(b*cos(alfa1) - O1(1) + l1*cos(alfa1)*cos(th1))*(2*sin(Az + alfa1)*cos(Ay)^2*cos(th1) - cos(Ax)^2*cos(Ay)^3*cos(th1) - 2*sin(Az + alfa1)*sin(Ay)^2*cos(th1) - cos(Ax)*cos(Ay)^2*cos(th1) + cos(Ax)*sin(Ay)^2*cos(th1) + 4*sin(Az + alfa1)*cos(Ax)*cos(Ay)^3*cos(th1) + 2*cos(Ay)*sin(Ax)*sin(Ay)^3*cos(th1) - 2*cos(Ay)^3*sin(Ax)*sin(Ay)*cos(th1) + 2*sin(Az + alfa1)*cos(Ax)^2*cos(Ay)^4*cos(th1) - cos(Ax)^2*cos(Ay)*sin(Ay)^2*cos(th1) - 2*sin(Az + alfa1)*cos(Ax)*cos(Ay)*sin(Ay)^2*cos(th1) - 2*cos(Ax)*cos(Ay)^4*sin(Ax)*sin(Ay)*cos(th1) + 2*sin(Az + alfa1)*cos(Ax)^2*sin(Ay)^3*cos(alfa1)*sin(th1) - 4*cos(Az + alfa1)*cos(Ax)^2*cos(Ay)^3*sin(Ax)*cos(alfa1)*sin(th1) - 2*cos(Az + alfa1)*cos(Ax)^3*cos(Ay)^4*sin(Ax)*cos(alfa1)*sin(th1) + 8*sin(Az + alfa1)*cos(Ax)^2*cos(Ay)^2*sin(Ay)*cos(alfa1)*sin(th1) + 2*sin(Az + alfa1)*cos(Ax)^3*cos(Ay)*sin(Ay)^3*cos(alfa1)*sin(th1) + 4*sin(Az + alfa1)*cos(Ax)^3*cos(Ay)^3*sin(Ay)*cos(alfa1)*sin(th1) + 4*sin(Az + alfa1)*cos(Ax)*cos(Ay)*sin(Ay)*cos(alfa1)*sin(th1) - 2*cos(Az + alfa1)*cos(Ax)*cos(Ay)^2*sin(Ax)*cos(alfa1)*sin(th1) + 2*cos(Az + alfa1)*cos(Ax)*sin(Ax)*sin(Ay)^2*cos(alfa1)*sin(th1) + 2*cos(Az + alfa1)*cos(Ax)^2*cos(Ay)*sin(Ax)*sin(Ay)^2*cos(alfa1)*sin(th1)))/(2*l2*cos(alfa1)*(cos(Ax)*cos(Ay) + 1)^3*(O1(1)*sin(th1) + O1(3)*cos(alfa1)*cos(th1) - b*cos(alfa1)*sin(th1))) - (dAx*p*cos(phi1)*(b*cos(alfa1) - O1(1) + l1*cos(alfa1)*cos(th1))*(2*sin(Az + alfa1)*sin(Ax)*cos(alfa1)*sin(th1) + cos(Ay)*sin(Ax)*sin(Ay)*cos(th1) - cos(Ax)^2*cos(Ay)^3*sin(Ay)^2*cos(th1) - 2*cos(Ay)^3*sin(Ax)^2*sin(Ay)^2*cos(th1) - cos(Ax)*cos(Ay)^2*sin(Ay)^2*cos(th1) + 2*sin(Az + alfa1)*cos(Ay)^2*sin(Ax)*sin(Ay)*cos(th1) - cos(Ax)*cos(Ay)^2*sin(Ax)*sin(Ay)*cos(th1) - 2*sin(Az + alfa1)*sin(Ax)*sin(Ay)^2*cos(alfa1)*sin(th1) - 4*cos(Az + alfa1)*cos(Ax)^3*cos(Ay)^2*sin(Ay)*cos(alfa1)*sin(th1) - 2*cos(Az + alfa1)*cos(Ax)^4*cos(Ay)^3*sin(Ay)*cos(alfa1)*sin(th1) + 6*sin(Az + alfa1)*cos(Ax)^2*cos(Ay)^2*sin(Ax)*cos(alfa1)*sin(th1) + 2*sin(Az + alfa1)*cos(Ax)^3*cos(Ay)^3*sin(Ax)*cos(alfa1)*sin(th1) + 6*sin(Az + alfa1)*cos(Ax)*cos(Ay)*sin(Ax)*cos(alfa1)*sin(th1) + 2*sin(Az + alfa1)*cos(Ax)*cos(Ay)^3*sin(Ax)*sin(Ay)*cos(th1) - 2*cos(Az + alfa1)*cos(Ax)^2*cos(Ay)*sin(Ay)*cos(alfa1)*sin(th1) + 2*cos(Az + alfa1)*cos(Ay)*sin(Ax)^2*sin(Ay)*cos(alfa1)*sin(th1) - 2*sin(Az + alfa1)*cos(Ax)*cos(Ay)*sin(Ax)*sin(Ay)^2*cos(alfa1)*sin(th1) + 2*cos(Az + alfa1)*cos(Ax)*cos(Ay)^2*sin(Ax)^2*sin(Ay)*cos(alfa1)*sin(th1)))/(2*l2*cos(alfa1)*(cos(Ax)*cos(Ay) + 1)^3*(O1(1)*sin(th1) + O1(3)*cos(alfa1)*cos(th1) - b*cos(alfa1)*sin(th1))), (dphi1*p*sin(phi1)*(b*cos(alfa1) - O1(1) + l1*cos(alfa1)*cos(th1))*(2*sin(Az + alfa1)*cos(Ay)*sin(Ax)*cos(th1) - cos(Ay)^2*sin(Ax)*cos(th1) - 2*cos(Az + alfa1)*sin(Ay)*cos(th1) - cos(Ax)*cos(Ay)*sin(Ax)*cos(th1) + 2*cos(Az + alfa1)*sin(Ax)^2*cos(alfa1)*sin(th1) - cos(Ay)*sin(Ax)^2*sin(Ay)*cos(th1) + 2*sin(Az + alfa1)*cos(Ax)*cos(Ay)^2*sin(Ax)*cos(th1) - 2*cos(Az + alfa1)*cos(Ax)^2*cos(Ay)^2*sin(Ay)*cos(th1) + 4*cos(Az + alfa1)*cos(Ax)^2*cos(Ay)^2*cos(alfa1)*sin(th1) + 2*cos(Az + alfa1)*cos(Ax)^3*cos(Ay)^3*cos(alfa1)*sin(th1) - 4*cos(Az + alfa1)*cos(Ax)*cos(Ay)*sin(Ay)*cos(th1) + 2*cos(Az + alfa1)*cos(Ax)*cos(Ay)*cos(alfa1)*sin(th1) + 2*sin(Az + alfa1)*cos(Ax)*sin(Ax)*sin(Ay)*cos(alfa1)*sin(th1) + 2*cos(Az + alfa1)*cos(Ax)*cos(Ay)*sin(Ax)^2*cos(alfa1)*sin(th1) + 2*sin(Az + alfa1)*cos(Ax)^2*cos(Ay)*sin(Ax)*sin(Ay)*cos(alfa1)*sin(th1)))/(2*l2*cos(alfa1)*(cos(Ax)*cos(Ay) + 1)^2*(O1(1)*sin(th1) + O1(3)*cos(alfa1)*cos(th1) - b*cos(alfa1)*sin(th1))) - dth1*((p*cos(phi1)*(b*cos(alfa1) - O1(1) + l1*cos(alfa1)*cos(th1))*(cos(Ay)^2*sin(Ax)*sin(th1) + 2*cos(Az + alfa1)*sin(Ay)*sin(th1) - 2*sin(Az + alfa1)*cos(Ay)*sin(Ax)*sin(th1) + cos(Ax)*cos(Ay)*sin(Ax)*sin(th1) + 2*cos(Az + alfa1)*sin(Ax)^2*cos(alfa1)*cos(th1) + cos(Ay)*sin(Ax)^2*sin(Ay)*sin(th1) - 2*sin(Az + alfa1)*cos(Ax)*cos(Ay)^2*sin(Ax)*sin(th1) + 4*cos(Az + alfa1)*cos(Ax)^2*cos(Ay)^2*cos(alfa1)*cos(th1) + 2*cos(Az + alfa1)*cos(Ax)^3*cos(Ay)^3*cos(alfa1)*cos(th1) + 2*cos(Az + alfa1)*cos(Ax)^2*cos(Ay)^2*sin(Ay)*sin(th1) + 2*cos(Az + alfa1)*cos(Ax)*cos(Ay)*cos(alfa1)*cos(th1) + 4*cos(Az + alfa1)*cos(Ax)*cos(Ay)*sin(Ay)*sin(th1) + 2*sin(Az + alfa1)*cos(Ax)*sin(Ax)*sin(Ay)*cos(alfa1)*cos(th1) + 2*cos(Az + alfa1)*cos(Ax)*cos(Ay)*sin(Ax)^2*cos(alfa1)*cos(th1) + 2*sin(Az + alfa1)*cos(Ax)^2*cos(Ay)*sin(Ax)*sin(Ay)*cos(alfa1)*cos(th1)))/(2*l2*cos(alfa1)*(cos(Ax)*cos(Ay) + 1)^2*(O1(1)*sin(th1) + O1(3)*cos(alfa1)*cos(th1) - b*cos(alfa1)*sin(th1))) - (l1*p*cos(phi1)*sin(th1)*(2*sin(Az + alfa1)*cos(Ay)*sin(Ax)*cos(th1) - cos(Ay)^2*sin(Ax)*cos(th1) - 2*cos(Az + alfa1)*sin(Ay)*cos(th1) - cos(Ax)*cos(Ay)*sin(Ax)*cos(th1) + 2*cos(Az + alfa1)*sin(Ax)^2*cos(alfa1)*sin(th1) - cos(Ay)*sin(Ax)^2*sin(Ay)*cos(th1) + 2*sin(Az + alfa1)*cos(Ax)*cos(Ay)^2*sin(Ax)*cos(th1) - 2*cos(Az + alfa1)*cos(Ax)^2*cos(Ay)^2*sin(Ay)*cos(th1) + 4*cos(Az + alfa1)*cos(Ax)^2*cos(Ay)^2*cos(alfa1)*sin(th1) + 2*cos(Az + alfa1)*cos(Ax)^3*cos(Ay)^3*cos(alfa1)*sin(th1) - 4*cos(Az + alfa1)*cos(Ax)*cos(Ay)*sin(Ay)*cos(th1) + 2*cos(Az + alfa1)*cos(Ax)*cos(Ay)*cos(alfa1)*sin(th1) + 2*sin(Az + alfa1)*cos(Ax)*sin(Ax)*sin(Ay)*cos(alfa1)*sin(th1) + 2*cos(Az + alfa1)*cos(Ax)*cos(Ay)*sin(Ax)^2*cos(alfa1)*sin(th1) + 2*sin(Az + alfa1)*cos(Ax)^2*cos(Ay)*sin(Ax)*sin(Ay)*cos(alfa1)*sin(th1)))/(2*l2*(cos(Ax)*cos(Ay) + 1)^2*(O1(1)*sin(th1) + O1(3)*cos(alfa1)*cos(th1) - b*cos(alfa1)*sin(th1))) + (p*cos(phi1)*(O1(3)*cos(alfa1)*sin(th1) - O1(1)*cos(th1) + b*cos(alfa1)*cos(th1))*(b*cos(alfa1) - O1(1) + l1*cos(alfa1)*cos(th1))*(2*sin(Az + alfa1)*cos(Ay)*sin(Ax)*cos(th1) - cos(Ay)^2*sin(Ax)*cos(th1) - 2*cos(Az + alfa1)*sin(Ay)*cos(th1) - cos(Ax)*cos(Ay)*sin(Ax)*cos(th1) + 2*cos(Az + alfa1)*sin(Ax)^2*cos(alfa1)*sin(th1) - cos(Ay)*sin(Ax)^2*sin(Ay)*cos(th1) + 2*sin(Az + alfa1)*cos(Ax)*cos(Ay)^2*sin(Ax)*cos(th1) - 2*cos(Az + alfa1)*cos(Ax)^2*cos(Ay)^2*sin(Ay)*cos(th1) + 4*cos(Az + alfa1)*cos(Ax)^2*cos(Ay)^2*cos(alfa1)*sin(th1) + 2*cos(Az + alfa1)*cos(Ax)^3*cos(Ay)^3*cos(alfa1)*sin(th1) - 4*cos(Az + alfa1)*cos(Ax)*cos(Ay)*sin(Ay)*cos(th1) + 2*cos(Az + alfa1)*cos(Ax)*cos(Ay)*cos(alfa1)*sin(th1) + 2*sin(Az + alfa1)*cos(Ax)*sin(Ax)*sin(Ay)*cos(alfa1)*sin(th1) + 2*cos(Az + alfa1)*cos(Ax)*cos(Ay)*sin(Ax)^2*cos(alfa1)*sin(th1) + 2*sin(Az + alfa1)*cos(Ax)^2*cos(Ay)*sin(Ax)*sin(Ay)*cos(alfa1)*sin(th1)))/(2*l2*cos(alfa1)*(cos(Ax)*cos(Ay) + 1)^2*(O1(1)*sin(th1) + O1(3)*cos(alfa1)*cos(th1) - b*cos(alfa1)*sin(th1))^2)) + (dO1(1)*p*cos(phi1)*cos(th1)*(O1(3) + l1*sin(th1))*(2*sin(Az + alfa1)*cos(Ay)*sin(Ax)*cos(th1) - cos(Ay)^2*sin(Ax)*cos(th1) - 2*cos(Az + alfa1)*sin(Ay)*cos(th1) - cos(Ax)*cos(Ay)*sin(Ax)*cos(th1) + 2*cos(Az + alfa1)*sin(Ax)^2*cos(alfa1)*sin(th1) - cos(Ay)*sin(Ax)^2*sin(Ay)*cos(th1) + 2*sin(Az + alfa1)*cos(Ax)*cos(Ay)^2*sin(Ax)*cos(th1) - 2*cos(Az + alfa1)*cos(Ax)^2*cos(Ay)^2*sin(Ay)*cos(th1) + 4*cos(Az + alfa1)*cos(Ax)^2*cos(Ay)^2*cos(alfa1)*sin(th1) + 2*cos(Az + alfa1)*cos(Ax)^3*cos(Ay)^3*cos(alfa1)*sin(th1) - 4*cos(Az + alfa1)*cos(Ax)*cos(Ay)*sin(Ay)*cos(th1) + 2*cos(Az + alfa1)*cos(Ax)*cos(Ay)*cos(alfa1)*sin(th1) + 2*sin(Az + alfa1)*cos(Ax)*sin(Ax)*sin(Ay)*cos(alfa1)*sin(th1) + 2*cos(Az + alfa1)*cos(Ax)*cos(Ay)*sin(Ax)^2*cos(alfa1)*sin(th1) + 2*sin(Az + alfa1)*cos(Ax)^2*cos(Ay)*sin(Ax)*sin(Ay)*cos(alfa1)*sin(th1)))/(2*l2*(cos(Ax)*cos(Ay) + 1)^2*(O1(1)*sin(th1) + O1(3)*cos(alfa1)*cos(th1) - b*cos(alfa1)*sin(th1))^2) - (dAz*p*cos(phi1)*(b*cos(alfa1) - O1(1) + l1*cos(alfa1)*cos(th1))*(sin(Az + alfa1)*sin(Ay)*cos(th1) - sin(Az + alfa1)*sin(Ax)^2*cos(alfa1)*sin(th1) + cos(Az + alfa1)*cos(Ay)*sin(Ax)*cos(th1) - sin(Az + alfa1)*cos(Ax)^2*cos(Ay)^2*cos(alfa1)*sin(th1) + sin(Az + alfa1)*cos(Ax)*cos(Ay)*sin(Ay)*cos(th1) - sin(Az + alfa1)*cos(Ax)*cos(Ay)*cos(alfa1)*sin(th1) + cos(Az + alfa1)*cos(Ax)*sin(Ax)*sin(Ay)*cos(alfa1)*sin(th1)))/(l2*cos(alfa1)*(cos(Ax)*cos(Ay) + 1)*(O1(1)*sin(th1) + O1(3)*cos(alfa1)*cos(th1) - b*cos(alfa1)*sin(th1))) + (dAy*p*cos(phi1)*(b*cos(alfa1) - O1(1) + l1*cos(alfa1)*cos(th1))*(2*cos(Az + alfa1)*cos(Ay)*cos(th1) + cos(Ay)^2*sin(Ax)^2*cos(th1) - sin(Ax)^2*sin(Ay)^2*cos(th1) + 2*sin(Az + alfa1)*sin(Ax)*sin(Ay)*cos(th1) - cos(Ax)*sin(Ax)*sin(Ay)*cos(th1) - 2*cos(Ay)*sin(Ax)*sin(Ay)*cos(th1) + 6*cos(Az + alfa1)*cos(Ax)*cos(Ay)^2*cos(th1) + 6*cos(Az + alfa1)*cos(Ax)^2*cos(Ay)^3*cos(th1) + 2*cos(Az + alfa1)*cos(Ax)^3*cos(Ay)^4*cos(th1) + cos(Ax)*cos(Ay)^3*sin(Ax)^2*cos(th1) + cos(Ax)^2*cos(Ay)*sin(Ax)*sin(Ay)*cos(th1) + cos(Ax)*cos(Ay)*sin(Ax)^2*sin(Ay)^2*cos(th1) + 2*cos(Az + alfa1)*cos(Ax)*sin(Ay)*cos(alfa1)*sin(th1) + 6*cos(Az + alfa1)*cos(Ax)^3*cos(Ay)^2*sin(Ay)*cos(alfa1)*sin(th1) + 2*cos(Az + alfa1)*cos(Ax)^4*cos(Ay)^3*sin(Ay)*cos(alfa1)*sin(th1) - 4*sin(Az + alfa1)*cos(Ax)^2*cos(Ay)^2*sin(Ax)*cos(alfa1)*sin(th1) - 2*sin(Az + alfa1)*cos(Ax)^3*cos(Ay)^3*sin(Ax)*cos(alfa1)*sin(th1) - 2*sin(Az + alfa1)*cos(Ax)^2*sin(Ax)*sin(Ay)^2*cos(alfa1)*sin(th1) + 2*sin(Az + alfa1)*cos(Ax)*cos(Ay)*sin(Ax)*sin(Ay)*cos(th1) - 2*sin(Az + alfa1)*cos(Ax)*cos(Ay)*sin(Ax)*cos(alfa1)*sin(th1) + 6*cos(Az + alfa1)*cos(Ax)^2*cos(Ay)*sin(Ay)*cos(alfa1)*sin(th1) - 2*cos(Az + alfa1)*cos(Ax)*sin(Ax)^2*sin(Ay)*cos(alfa1)*sin(th1) - 2*cos(Az + alfa1)*cos(Ax)^2*cos(Ay)*sin(Ax)^2*sin(Ay)*cos(alfa1)*sin(th1) - 2*sin(Az + alfa1)*cos(Ax)^3*cos(Ay)*sin(Ax)*sin(Ay)^2*cos(alfa1)*sin(th1)))/(2*l2*cos(alfa1)*(cos(Ax)*cos(Ay) + 1)^3*(O1(1)*sin(th1) + O1(3)*cos(alfa1)*cos(th1) - b*cos(alfa1)*sin(th1))) + (dAx*p*cos(phi1)*(b*cos(alfa1) - O1(1) + l1*cos(alfa1)*cos(th1))*(cos(Ax)^2*cos(Ay)^3*cos(th1) + cos(Ax)^3*cos(Ay)^2*cos(th1) + 2*cos(Ay)^3*sin(Ax)^2*cos(th1) + cos(Ax)*cos(Ay)^2*cos(th1) + cos(Ax)^2*cos(Ay)*cos(th1) - cos(Ay)*sin(Ax)^2*cos(th1) + 2*cos(Ay)^2*sin(Ax)^3*sin(Ay)*cos(th1) - 4*sin(Az + alfa1)*cos(Ax)^2*cos(Ay)^2*cos(th1) - 2*sin(Az + alfa1)*cos(Ax)^3*cos(Ay)^3*cos(th1) - 2*sin(Az + alfa1)*cos(Ay)^2*sin(Ax)^2*cos(th1) + cos(Ax)*cos(Ay)^2*sin(Ax)^2*cos(th1) - 2*sin(Az + alfa1)*cos(Ax)*cos(Ay)*cos(th1) - 2*cos(Az + alfa1)*cos(Ay)*sin(Ax)^3*cos(alfa1)*sin(th1) - 2*sin(Az + alfa1)*cos(Ax)^2*sin(Ay)*cos(alfa1)*sin(th1) + 2*sin(Az + alfa1)*sin(Ax)^2*sin(Ay)*cos(alfa1)*sin(th1) - 2*sin(Az + alfa1)*cos(Ax)*cos(Ay)^3*sin(Ax)^2*cos(th1) + 2*cos(Ax)^2*cos(Ay)^2*sin(Ax)*sin(Ay)*cos(th1) - 4*cos(Az + alfa1)*cos(Ax)*sin(Ax)*cos(alfa1)*sin(th1) + 2*cos(Az + alfa1)*cos(Ay)*sin(Ax)*cos(alfa1)*sin(th1) + 2*cos(Ax)*cos(Ay)*sin(Ax)*sin(Ay)*cos(th1) - 2*cos(Az + alfa1)*cos(Ax)*cos(Ay)^2*sin(Ax)^3*cos(alfa1)*sin(th1) + 6*cos(Az + alfa1)*cos(Ax)^2*cos(Ay)^3*sin(Ax)*cos(alfa1)*sin(th1) - 4*cos(Az + alfa1)*cos(Ax)^3*cos(Ay)^2*sin(Ax)*cos(alfa1)*sin(th1) + 2*cos(Az + alfa1)*cos(Ax)^3*cos(Ay)^4*sin(Ax)*cos(alfa1)*sin(th1) - 2*sin(Az + alfa1)*cos(Ax)^4*cos(Ay)^2*sin(Ay)*cos(alfa1)*sin(th1) + 6*cos(Az + alfa1)*cos(Ax)*cos(Ay)^2*sin(Ax)*cos(alfa1)*sin(th1) - 8*cos(Az + alfa1)*cos(Ax)^2*cos(Ay)*sin(Ax)*cos(alfa1)*sin(th1) - 4*sin(Az + alfa1)*cos(Ax)^3*cos(Ay)*sin(Ay)*cos(alfa1)*sin(th1) + 2*sin(Az + alfa1)*cos(Ax)*cos(Ay)*sin(Ax)^2*sin(Ay)*cos(alfa1)*sin(th1)))/(2*l2*cos(alfa1)*(cos(Ax)*cos(Ay) + 1)^3*(O1(1)*sin(th1) + O1(3)*cos(alfa1)*cos(th1) - b*cos(alfa1)*sin(th1))) + (dO1(3)*p*cos(phi1)*cos(th1)*(b*cos(alfa1) - O1(1) + l1*cos(alfa1)*cos(th1))*(2*sin(Az + alfa1)*cos(Ay)*sin(Ax)*cos(th1) - cos(Ay)^2*sin(Ax)*cos(th1) - 2*cos(Az + alfa1)*sin(Ay)*cos(th1) - cos(Ax)*cos(Ay)*sin(Ax)*cos(th1) + 2*cos(Az + alfa1)*sin(Ax)^2*cos(alfa1)*sin(th1) - cos(Ay)*sin(Ax)^2*sin(Ay)*cos(th1) + 2*sin(Az + alfa1)*cos(Ax)*cos(Ay)^2*sin(Ax)*cos(th1) - 2*cos(Az + alfa1)*cos(Ax)^2*cos(Ay)^2*sin(Ay)*cos(th1) + 4*cos(Az + alfa1)*cos(Ax)^2*cos(Ay)^2*cos(alfa1)*sin(th1) + 2*cos(Az + alfa1)*cos(Ax)^3*cos(Ay)^3*cos(alfa1)*sin(th1) - 4*cos(Az + alfa1)*cos(Ax)*cos(Ay)*sin(Ay)*cos(th1) + 2*cos(Az + alfa1)*cos(Ax)*cos(Ay)*cos(alfa1)*sin(th1) + 2*sin(Az + alfa1)*cos(Ax)*sin(Ax)*sin(Ay)*cos(alfa1)*sin(th1) + 2*cos(Az + alfa1)*cos(Ax)*cos(Ay)*sin(Ax)^2*cos(alfa1)*sin(th1) + 2*sin(Az + alfa1)*cos(Ax)^2*cos(Ay)*sin(Ax)*sin(Ay)*cos(alfa1)*sin(th1)))/(2*l2*(cos(Ax)*cos(Ay) + 1)^2*(O1(1)*sin(th1) + O1(3)*cos(alfa1)*cos(th1) - b*cos(alfa1)*sin(th1))^2)
       -(O2(1)*O2(3)*dth2*cos(alfa2)*cos(phi2)*cos(th2)^2 - b^2*dphi2*cos(alfa2)^2*sin(phi2)*sin(th2)^2 - O2(1)^2*dphi2*sin(phi2)*sin(th2)^2 + O2(1)*O2(3)*dth2*cos(alfa2)*cos(phi2)*sin(th2)^2 + dO2(3)*l1*cos(alfa2)^2*cos(phi2)*cos(th2)^2*sin(th2) + O2(1)*dth2*l1*cos(alfa2)*cos(phi2)*sin(th2)^3 + 2*O2(1)*b*dphi2*cos(alfa2)*sin(phi2)*sin(th2)^2 - O2(1)*dO2(3)*cos(alfa2)*cos(phi2)*cos(th2)*sin(th2) + O2(3)*dO2(1)*cos(alfa2)*cos(phi2)*cos(th2)*sin(th2) - O2(3)*b*dth2*cos(alfa2)^2*cos(phi2)*cos(th2)^2 - O2(3)*dth2*l1*cos(alfa2)^2*cos(phi2)*cos(th2)^3 - O2(3)*b*dth2*cos(alfa2)^2*cos(phi2)*sin(th2)^2 - b*dth2*l1*cos(alfa2)^2*cos(phi2)*sin(th2)^3 + b*dO2(3)*cos(alfa2)^2*cos(phi2)*cos(th2)*sin(th2) + dO2(1)*l1*cos(alfa2)*cos(phi2)*cos(th2)*sin(th2)^2 + O2(3)*b*dphi2*cos(alfa2)^2*cos(th2)*sin(phi2)*sin(th2) + O2(1)*dphi2*l1*cos(alfa2)*cos(th2)*sin(phi2)*sin(th2)^2 + O2(3)*dphi2*l1*cos(alfa2)^2*cos(th2)^2*sin(phi2)*sin(th2) - b*dphi2*l1*cos(alfa2)^2*cos(th2)*sin(phi2)*sin(th2)^2 - O2(1)*O2(3)*dphi2*cos(alfa2)*cos(th2)*sin(phi2)*sin(th2))/(l2*(O2(1)*sin(th2) + O2(3)*cos(alfa2)*cos(th2) - b*cos(alfa2)*sin(th2))^2), dth2*((p*cos(phi2)*(b*cos(alfa2) - O2(1) + l1*cos(alfa2)*cos(th2))*(2*sin(Az + alfa2)*cos(Ax)*cos(alfa2)*cos(th2) - cos(Ay)^2*sin(Ax)*sin(Ay)^2*sin(th2) + 2*sin(Az + alfa2)*cos(Ay)*sin(Ay)*sin(th2) - cos(Ax)*cos(Ay)*sin(Ay)*sin(th2) + 4*sin(Az + alfa2)*cos(Ax)^2*cos(Ay)*cos(alfa2)*cos(th2) + 2*sin(Az + alfa2)*cos(Ax)*cos(Ay)^2*sin(Ay)*sin(th2) - 2*sin(Az + alfa2)*cos(Ax)*sin(Ay)^2*cos(alfa2)*cos(th2) + 2*sin(Az + alfa2)*cos(Ax)^3*cos(Ay)^2*cos(alfa2)*cos(th2) - 2*sin(Az + alfa2)*cos(Ax)^2*cos(Ay)*sin(Ay)^2*cos(alfa2)*cos(th2) + 2*cos(Az + alfa2)*cos(Ax)*cos(Ay)*sin(Ax)*sin(Ay)*cos(alfa2)*cos(th2) + 2*cos(Az + alfa2)*cos(Ax)^2*cos(Ay)^2*sin(Ax)*sin(Ay)*cos(alfa2)*cos(th2)))/(2*l2*cos(alfa2)*(cos(Ax)*cos(Ay) + 1)^2*(O2(1)*sin(th2) + O2(3)*cos(alfa2)*cos(th2) - b*cos(alfa2)*sin(th2))) - (l1*p*cos(phi2)*sin(th2)*(cos(Ay)^2*sin(Ax)*sin(Ay)^2*cos(th2) - 2*sin(Az + alfa2)*cos(Ay)*sin(Ay)*cos(th2) + 2*sin(Az + alfa2)*cos(Ax)*cos(alfa2)*sin(th2) + cos(Ax)*cos(Ay)*sin(Ay)*cos(th2) - 2*sin(Az + alfa2)*cos(Ax)*cos(Ay)^2*sin(Ay)*cos(th2) + 4*sin(Az + alfa2)*cos(Ax)^2*cos(Ay)*cos(alfa2)*sin(th2) - 2*sin(Az + alfa2)*cos(Ax)*sin(Ay)^2*cos(alfa2)*sin(th2) + 2*sin(Az + alfa2)*cos(Ax)^3*cos(Ay)^2*cos(alfa2)*sin(th2) - 2*sin(Az + alfa2)*cos(Ax)^2*cos(Ay)*sin(Ay)^2*cos(alfa2)*sin(th2) + 2*cos(Az + alfa2)*cos(Ax)*cos(Ay)*sin(Ax)*sin(Ay)*cos(alfa2)*sin(th2) + 2*cos(Az + alfa2)*cos(Ax)^2*cos(Ay)^2*sin(Ax)*sin(Ay)*cos(alfa2)*sin(th2)))/(2*l2*(cos(Ax)*cos(Ay) + 1)^2*(O2(1)*sin(th2) + O2(3)*cos(alfa2)*cos(th2) - b*cos(alfa2)*sin(th2))) + (p*cos(phi2)*(O2(3)*cos(alfa2)*sin(th2) - O2(1)*cos(th2) + b*cos(alfa2)*cos(th2))*(b*cos(alfa2) - O2(1) + l1*cos(alfa2)*cos(th2))*(cos(Ay)^2*sin(Ax)*sin(Ay)^2*cos(th2) - 2*sin(Az + alfa2)*cos(Ay)*sin(Ay)*cos(th2) + 2*sin(Az + alfa2)*cos(Ax)*cos(alfa2)*sin(th2) + cos(Ax)*cos(Ay)*sin(Ay)*cos(th2) - 2*sin(Az + alfa2)*cos(Ax)*cos(Ay)^2*sin(Ay)*cos(th2) + 4*sin(Az + alfa2)*cos(Ax)^2*cos(Ay)*cos(alfa2)*sin(th2) - 2*sin(Az + alfa2)*cos(Ax)*sin(Ay)^2*cos(alfa2)*sin(th2) + 2*sin(Az + alfa2)*cos(Ax)^3*cos(Ay)^2*cos(alfa2)*sin(th2) - 2*sin(Az + alfa2)*cos(Ax)^2*cos(Ay)*sin(Ay)^2*cos(alfa2)*sin(th2) + 2*cos(Az + alfa2)*cos(Ax)*cos(Ay)*sin(Ax)*sin(Ay)*cos(alfa2)*sin(th2) + 2*cos(Az + alfa2)*cos(Ax)^2*cos(Ay)^2*sin(Ax)*sin(Ay)*cos(alfa2)*sin(th2)))/(2*l2*cos(alfa2)*(cos(Ax)*cos(Ay) + 1)^2*(O2(1)*sin(th2) + O2(3)*cos(alfa2)*cos(th2) - b*cos(alfa2)*sin(th2))^2)) - (dO2(3)*p*cos(phi2)*cos(th2)*(b*cos(alfa2) - O2(1) + l1*cos(alfa2)*cos(th2))*(cos(Ay)^2*sin(Ax)*sin(Ay)^2*cos(th2) - 2*sin(Az + alfa2)*cos(Ay)*sin(Ay)*cos(th2) + 2*sin(Az + alfa2)*cos(Ax)*cos(alfa2)*sin(th2) + cos(Ax)*cos(Ay)*sin(Ay)*cos(th2) - 2*sin(Az + alfa2)*cos(Ax)*cos(Ay)^2*sin(Ay)*cos(th2) + 4*sin(Az + alfa2)*cos(Ax)^2*cos(Ay)*cos(alfa2)*sin(th2) - 2*sin(Az + alfa2)*cos(Ax)*sin(Ay)^2*cos(alfa2)*sin(th2) + 2*sin(Az + alfa2)*cos(Ax)^3*cos(Ay)^2*cos(alfa2)*sin(th2) - 2*sin(Az + alfa2)*cos(Ax)^2*cos(Ay)*sin(Ay)^2*cos(alfa2)*sin(th2) + 2*cos(Az + alfa2)*cos(Ax)*cos(Ay)*sin(Ax)*sin(Ay)*cos(alfa2)*sin(th2) + 2*cos(Az + alfa2)*cos(Ax)^2*cos(Ay)^2*sin(Ax)*sin(Ay)*cos(alfa2)*sin(th2)))/(2*l2*(cos(Ax)*cos(Ay) + 1)^2*(O2(1)*sin(th2) + O2(3)*cos(alfa2)*cos(th2) - b*cos(alfa2)*sin(th2))^2) - (dAz*p*cos(phi2)*(b*cos(alfa2) - O2(1) + l1*cos(alfa2)*cos(th2))*(cos(Az + alfa2)*cos(Ay)*sin(Ay)*cos(th2) - cos(Az + alfa2)*cos(Ax)*cos(alfa2)*sin(th2) - cos(Az + alfa2)*cos(Ax)^2*cos(Ay)*cos(alfa2)*sin(th2) + cos(Az + alfa2)*cos(Ax)*sin(Ay)^2*cos(alfa2)*sin(th2) + sin(Az + alfa2)*cos(Ax)*cos(Ay)*sin(Ax)*sin(Ay)*cos(alfa2)*sin(th2)))/(l2*cos(alfa2)*(cos(Ax)*cos(Ay) + 1)*(O2(1)*sin(th2) + O2(3)*cos(alfa2)*cos(th2) - b*cos(alfa2)*sin(th2))) - (dphi2*p*sin(phi2)*(b*cos(alfa2) - O2(1) + l1*cos(alfa2)*cos(th2))*(cos(Ay)^2*sin(Ax)*sin(Ay)^2*cos(th2) - 2*sin(Az + alfa2)*cos(Ay)*sin(Ay)*cos(th2) + 2*sin(Az + alfa2)*cos(Ax)*cos(alfa2)*sin(th2) + cos(Ax)*cos(Ay)*sin(Ay)*cos(th2) - 2*sin(Az + alfa2)*cos(Ax)*cos(Ay)^2*sin(Ay)*cos(th2) + 4*sin(Az + alfa2)*cos(Ax)^2*cos(Ay)*cos(alfa2)*sin(th2) - 2*sin(Az + alfa2)*cos(Ax)*sin(Ay)^2*cos(alfa2)*sin(th2) + 2*sin(Az + alfa2)*cos(Ax)^3*cos(Ay)^2*cos(alfa2)*sin(th2) - 2*sin(Az + alfa2)*cos(Ax)^2*cos(Ay)*sin(Ay)^2*cos(alfa2)*sin(th2) + 2*cos(Az + alfa2)*cos(Ax)*cos(Ay)*sin(Ax)*sin(Ay)*cos(alfa2)*sin(th2) + 2*cos(Az + alfa2)*cos(Ax)^2*cos(Ay)^2*sin(Ax)*sin(Ay)*cos(alfa2)*sin(th2)))/(2*l2*cos(alfa2)*(cos(Ax)*cos(Ay) + 1)^2*(O2(1)*sin(th2) + O2(3)*cos(alfa2)*cos(th2) - b*cos(alfa2)*sin(th2))) - (dO2(1)*p*cos(phi2)*cos(th2)*(O2(3) + l1*sin(th2))*(cos(Ay)^2*sin(Ax)*sin(Ay)^2*cos(th2) - 2*sin(Az + alfa2)*cos(Ay)*sin(Ay)*cos(th2) + 2*sin(Az + alfa2)*cos(Ax)*cos(alfa2)*sin(th2) + cos(Ax)*cos(Ay)*sin(Ay)*cos(th2) - 2*sin(Az + alfa2)*cos(Ax)*cos(Ay)^2*sin(Ay)*cos(th2) + 4*sin(Az + alfa2)*cos(Ax)^2*cos(Ay)*cos(alfa2)*sin(th2) - 2*sin(Az + alfa2)*cos(Ax)*sin(Ay)^2*cos(alfa2)*sin(th2) + 2*sin(Az + alfa2)*cos(Ax)^3*cos(Ay)^2*cos(alfa2)*sin(th2) - 2*sin(Az + alfa2)*cos(Ax)^2*cos(Ay)*sin(Ay)^2*cos(alfa2)*sin(th2) + 2*cos(Az + alfa2)*cos(Ax)*cos(Ay)*sin(Ax)*sin(Ay)*cos(alfa2)*sin(th2) + 2*cos(Az + alfa2)*cos(Ax)^2*cos(Ay)^2*sin(Ax)*sin(Ay)*cos(alfa2)*sin(th2)))/(2*l2*(cos(Ax)*cos(Ay) + 1)^2*(O2(1)*sin(th2) + O2(3)*cos(alfa2)*cos(th2) - b*cos(alfa2)*sin(th2))^2) - (dAy*p*cos(phi2)*(b*cos(alfa2) - O2(1) + l1*cos(alfa2)*cos(th2))*(2*sin(Az + alfa2)*cos(Ay)^2*cos(th2) - cos(Ax)^2*cos(Ay)^3*cos(th2) - 2*sin(Az + alfa2)*sin(Ay)^2*cos(th2) - cos(Ax)*cos(Ay)^2*cos(th2) + cos(Ax)*sin(Ay)^2*cos(th2) + 4*sin(Az + alfa2)*cos(Ax)*cos(Ay)^3*cos(th2) + 2*cos(Ay)*sin(Ax)*sin(Ay)^3*cos(th2) - 2*cos(Ay)^3*sin(Ax)*sin(Ay)*cos(th2) + 2*sin(Az + alfa2)*cos(Ax)^2*cos(Ay)^4*cos(th2) - cos(Ax)^2*cos(Ay)*sin(Ay)^2*cos(th2) - 2*sin(Az + alfa2)*cos(Ax)*cos(Ay)*sin(Ay)^2*cos(th2) - 2*cos(Ax)*cos(Ay)^4*sin(Ax)*sin(Ay)*cos(th2) + 2*sin(Az + alfa2)*cos(Ax)^2*sin(Ay)^3*cos(alfa2)*sin(th2) - 4*cos(Az + alfa2)*cos(Ax)^2*cos(Ay)^3*sin(Ax)*cos(alfa2)*sin(th2) - 2*cos(Az + alfa2)*cos(Ax)^3*cos(Ay)^4*sin(Ax)*cos(alfa2)*sin(th2) + 8*sin(Az + alfa2)*cos(Ax)^2*cos(Ay)^2*sin(Ay)*cos(alfa2)*sin(th2) + 2*sin(Az + alfa2)*cos(Ax)^3*cos(Ay)*sin(Ay)^3*cos(alfa2)*sin(th2) + 4*sin(Az + alfa2)*cos(Ax)^3*cos(Ay)^3*sin(Ay)*cos(alfa2)*sin(th2) + 4*sin(Az + alfa2)*cos(Ax)*cos(Ay)*sin(Ay)*cos(alfa2)*sin(th2) - 2*cos(Az + alfa2)*cos(Ax)*cos(Ay)^2*sin(Ax)*cos(alfa2)*sin(th2) + 2*cos(Az + alfa2)*cos(Ax)*sin(Ax)*sin(Ay)^2*cos(alfa2)*sin(th2) + 2*cos(Az + alfa2)*cos(Ax)^2*cos(Ay)*sin(Ax)*sin(Ay)^2*cos(alfa2)*sin(th2)))/(2*l2*cos(alfa2)*(cos(Ax)*cos(Ay) + 1)^3*(O2(1)*sin(th2) + O2(3)*cos(alfa2)*cos(th2) - b*cos(alfa2)*sin(th2))) - (dAx*p*cos(phi2)*(b*cos(alfa2) - O2(1) + l1*cos(alfa2)*cos(th2))*(2*sin(Az + alfa2)*sin(Ax)*cos(alfa2)*sin(th2) + cos(Ay)*sin(Ax)*sin(Ay)*cos(th2) - cos(Ax)^2*cos(Ay)^3*sin(Ay)^2*cos(th2) - 2*cos(Ay)^3*sin(Ax)^2*sin(Ay)^2*cos(th2) - cos(Ax)*cos(Ay)^2*sin(Ay)^2*cos(th2) + 2*sin(Az + alfa2)*cos(Ay)^2*sin(Ax)*sin(Ay)*cos(th2) - cos(Ax)*cos(Ay)^2*sin(Ax)*sin(Ay)*cos(th2) - 2*sin(Az + alfa2)*sin(Ax)*sin(Ay)^2*cos(alfa2)*sin(th2) - 4*cos(Az + alfa2)*cos(Ax)^3*cos(Ay)^2*sin(Ay)*cos(alfa2)*sin(th2) - 2*cos(Az + alfa2)*cos(Ax)^4*cos(Ay)^3*sin(Ay)*cos(alfa2)*sin(th2) + 6*sin(Az + alfa2)*cos(Ax)^2*cos(Ay)^2*sin(Ax)*cos(alfa2)*sin(th2) + 2*sin(Az + alfa2)*cos(Ax)^3*cos(Ay)^3*sin(Ax)*cos(alfa2)*sin(th2) + 6*sin(Az + alfa2)*cos(Ax)*cos(Ay)*sin(Ax)*cos(alfa2)*sin(th2) + 2*sin(Az + alfa2)*cos(Ax)*cos(Ay)^3*sin(Ax)*sin(Ay)*cos(th2) - 2*cos(Az + alfa2)*cos(Ax)^2*cos(Ay)*sin(Ay)*cos(alfa2)*sin(th2) + 2*cos(Az + alfa2)*cos(Ay)*sin(Ax)^2*sin(Ay)*cos(alfa2)*sin(th2) - 2*sin(Az + alfa2)*cos(Ax)*cos(Ay)*sin(Ax)*sin(Ay)^2*cos(alfa2)*sin(th2) + 2*cos(Az + alfa2)*cos(Ax)*cos(Ay)^2*sin(Ax)^2*sin(Ay)*cos(alfa2)*sin(th2)))/(2*l2*cos(alfa2)*(cos(Ax)*cos(Ay) + 1)^3*(O2(1)*sin(th2) + O2(3)*cos(alfa2)*cos(th2) - b*cos(alfa2)*sin(th2))), (dphi2*p*sin(phi2)*(b*cos(alfa2) - O2(1) + l1*cos(alfa2)*cos(th2))*(2*sin(Az + alfa2)*cos(Ay)*sin(Ax)*cos(th2) - cos(Ay)^2*sin(Ax)*cos(th2) - 2*cos(Az + alfa2)*sin(Ay)*cos(th2) - cos(Ax)*cos(Ay)*sin(Ax)*cos(th2) + 2*cos(Az + alfa2)*sin(Ax)^2*cos(alfa2)*sin(th2) - cos(Ay)*sin(Ax)^2*sin(Ay)*cos(th2) + 2*sin(Az + alfa2)*cos(Ax)*cos(Ay)^2*sin(Ax)*cos(th2) - 2*cos(Az + alfa2)*cos(Ax)^2*cos(Ay)^2*sin(Ay)*cos(th2) + 4*cos(Az + alfa2)*cos(Ax)^2*cos(Ay)^2*cos(alfa2)*sin(th2) + 2*cos(Az + alfa2)*cos(Ax)^3*cos(Ay)^3*cos(alfa2)*sin(th2) - 4*cos(Az + alfa2)*cos(Ax)*cos(Ay)*sin(Ay)*cos(th2) + 2*cos(Az + alfa2)*cos(Ax)*cos(Ay)*cos(alfa2)*sin(th2) + 2*sin(Az + alfa2)*cos(Ax)*sin(Ax)*sin(Ay)*cos(alfa2)*sin(th2) + 2*cos(Az + alfa2)*cos(Ax)*cos(Ay)*sin(Ax)^2*cos(alfa2)*sin(th2) + 2*sin(Az + alfa2)*cos(Ax)^2*cos(Ay)*sin(Ax)*sin(Ay)*cos(alfa2)*sin(th2)))/(2*l2*cos(alfa2)*(cos(Ax)*cos(Ay) + 1)^2*(O2(1)*sin(th2) + O2(3)*cos(alfa2)*cos(th2) - b*cos(alfa2)*sin(th2))) - dth2*((p*cos(phi2)*(b*cos(alfa2) - O2(1) + l1*cos(alfa2)*cos(th2))*(cos(Ay)^2*sin(Ax)*sin(th2) + 2*cos(Az + alfa2)*sin(Ay)*sin(th2) - 2*sin(Az + alfa2)*cos(Ay)*sin(Ax)*sin(th2) + cos(Ax)*cos(Ay)*sin(Ax)*sin(th2) + 2*cos(Az + alfa2)*sin(Ax)^2*cos(alfa2)*cos(th2) + cos(Ay)*sin(Ax)^2*sin(Ay)*sin(th2) - 2*sin(Az + alfa2)*cos(Ax)*cos(Ay)^2*sin(Ax)*sin(th2) + 4*cos(Az + alfa2)*cos(Ax)^2*cos(Ay)^2*cos(alfa2)*cos(th2) + 2*cos(Az + alfa2)*cos(Ax)^3*cos(Ay)^3*cos(alfa2)*cos(th2) + 2*cos(Az + alfa2)*cos(Ax)^2*cos(Ay)^2*sin(Ay)*sin(th2) + 2*cos(Az + alfa2)*cos(Ax)*cos(Ay)*cos(alfa2)*cos(th2) + 4*cos(Az + alfa2)*cos(Ax)*cos(Ay)*sin(Ay)*sin(th2) + 2*sin(Az + alfa2)*cos(Ax)*sin(Ax)*sin(Ay)*cos(alfa2)*cos(th2) + 2*cos(Az + alfa2)*cos(Ax)*cos(Ay)*sin(Ax)^2*cos(alfa2)*cos(th2) + 2*sin(Az + alfa2)*cos(Ax)^2*cos(Ay)*sin(Ax)*sin(Ay)*cos(alfa2)*cos(th2)))/(2*l2*cos(alfa2)*(cos(Ax)*cos(Ay) + 1)^2*(O2(1)*sin(th2) + O2(3)*cos(alfa2)*cos(th2) - b*cos(alfa2)*sin(th2))) - (l1*p*cos(phi2)*sin(th2)*(2*sin(Az + alfa2)*cos(Ay)*sin(Ax)*cos(th2) - cos(Ay)^2*sin(Ax)*cos(th2) - 2*cos(Az + alfa2)*sin(Ay)*cos(th2) - cos(Ax)*cos(Ay)*sin(Ax)*cos(th2) + 2*cos(Az + alfa2)*sin(Ax)^2*cos(alfa2)*sin(th2) - cos(Ay)*sin(Ax)^2*sin(Ay)*cos(th2) + 2*sin(Az + alfa2)*cos(Ax)*cos(Ay)^2*sin(Ax)*cos(th2) - 2*cos(Az + alfa2)*cos(Ax)^2*cos(Ay)^2*sin(Ay)*cos(th2) + 4*cos(Az + alfa2)*cos(Ax)^2*cos(Ay)^2*cos(alfa2)*sin(th2) + 2*cos(Az + alfa2)*cos(Ax)^3*cos(Ay)^3*cos(alfa2)*sin(th2) - 4*cos(Az + alfa2)*cos(Ax)*cos(Ay)*sin(Ay)*cos(th2) + 2*cos(Az + alfa2)*cos(Ax)*cos(Ay)*cos(alfa2)*sin(th2) + 2*sin(Az + alfa2)*cos(Ax)*sin(Ax)*sin(Ay)*cos(alfa2)*sin(th2) + 2*cos(Az + alfa2)*cos(Ax)*cos(Ay)*sin(Ax)^2*cos(alfa2)*sin(th2) + 2*sin(Az + alfa2)*cos(Ax)^2*cos(Ay)*sin(Ax)*sin(Ay)*cos(alfa2)*sin(th2)))/(2*l2*(cos(Ax)*cos(Ay) + 1)^2*(O2(1)*sin(th2) + O2(3)*cos(alfa2)*cos(th2) - b*cos(alfa2)*sin(th2))) + (p*cos(phi2)*(O2(3)*cos(alfa2)*sin(th2) - O2(1)*cos(th2) + b*cos(alfa2)*cos(th2))*(b*cos(alfa2) - O2(1) + l1*cos(alfa2)*cos(th2))*(2*sin(Az + alfa2)*cos(Ay)*sin(Ax)*cos(th2) - cos(Ay)^2*sin(Ax)*cos(th2) - 2*cos(Az + alfa2)*sin(Ay)*cos(th2) - cos(Ax)*cos(Ay)*sin(Ax)*cos(th2) + 2*cos(Az + alfa2)*sin(Ax)^2*cos(alfa2)*sin(th2) - cos(Ay)*sin(Ax)^2*sin(Ay)*cos(th2) + 2*sin(Az + alfa2)*cos(Ax)*cos(Ay)^2*sin(Ax)*cos(th2) - 2*cos(Az + alfa2)*cos(Ax)^2*cos(Ay)^2*sin(Ay)*cos(th2) + 4*cos(Az + alfa2)*cos(Ax)^2*cos(Ay)^2*cos(alfa2)*sin(th2) + 2*cos(Az + alfa2)*cos(Ax)^3*cos(Ay)^3*cos(alfa2)*sin(th2) - 4*cos(Az + alfa2)*cos(Ax)*cos(Ay)*sin(Ay)*cos(th2) + 2*cos(Az + alfa2)*cos(Ax)*cos(Ay)*cos(alfa2)*sin(th2) + 2*sin(Az + alfa2)*cos(Ax)*sin(Ax)*sin(Ay)*cos(alfa2)*sin(th2) + 2*cos(Az + alfa2)*cos(Ax)*cos(Ay)*sin(Ax)^2*cos(alfa2)*sin(th2) + 2*sin(Az + alfa2)*cos(Ax)^2*cos(Ay)*sin(Ax)*sin(Ay)*cos(alfa2)*sin(th2)))/(2*l2*cos(alfa2)*(cos(Ax)*cos(Ay) + 1)^2*(O2(1)*sin(th2) + O2(3)*cos(alfa2)*cos(th2) - b*cos(alfa2)*sin(th2))^2)) + (dO2(1)*p*cos(phi2)*cos(th2)*(O2(3) + l1*sin(th2))*(2*sin(Az + alfa2)*cos(Ay)*sin(Ax)*cos(th2) - cos(Ay)^2*sin(Ax)*cos(th2) - 2*cos(Az + alfa2)*sin(Ay)*cos(th2) - cos(Ax)*cos(Ay)*sin(Ax)*cos(th2) + 2*cos(Az + alfa2)*sin(Ax)^2*cos(alfa2)*sin(th2) - cos(Ay)*sin(Ax)^2*sin(Ay)*cos(th2) + 2*sin(Az + alfa2)*cos(Ax)*cos(Ay)^2*sin(Ax)*cos(th2) - 2*cos(Az + alfa2)*cos(Ax)^2*cos(Ay)^2*sin(Ay)*cos(th2) + 4*cos(Az + alfa2)*cos(Ax)^2*cos(Ay)^2*cos(alfa2)*sin(th2) + 2*cos(Az + alfa2)*cos(Ax)^3*cos(Ay)^3*cos(alfa2)*sin(th2) - 4*cos(Az + alfa2)*cos(Ax)*cos(Ay)*sin(Ay)*cos(th2) + 2*cos(Az + alfa2)*cos(Ax)*cos(Ay)*cos(alfa2)*sin(th2) + 2*sin(Az + alfa2)*cos(Ax)*sin(Ax)*sin(Ay)*cos(alfa2)*sin(th2) + 2*cos(Az + alfa2)*cos(Ax)*cos(Ay)*sin(Ax)^2*cos(alfa2)*sin(th2) + 2*sin(Az + alfa2)*cos(Ax)^2*cos(Ay)*sin(Ax)*sin(Ay)*cos(alfa2)*sin(th2)))/(2*l2*(cos(Ax)*cos(Ay) + 1)^2*(O2(1)*sin(th2) + O2(3)*cos(alfa2)*cos(th2) - b*cos(alfa2)*sin(th2))^2) - (dAz*p*cos(phi2)*(b*cos(alfa2) - O2(1) + l1*cos(alfa2)*cos(th2))*(sin(Az + alfa2)*sin(Ay)*cos(th2) - sin(Az + alfa2)*sin(Ax)^2*cos(alfa2)*sin(th2) + cos(Az + alfa2)*cos(Ay)*sin(Ax)*cos(th2) - sin(Az + alfa2)*cos(Ax)^2*cos(Ay)^2*cos(alfa2)*sin(th2) + sin(Az + alfa2)*cos(Ax)*cos(Ay)*sin(Ay)*cos(th2) - sin(Az + alfa2)*cos(Ax)*cos(Ay)*cos(alfa2)*sin(th2) + cos(Az + alfa2)*cos(Ax)*sin(Ax)*sin(Ay)*cos(alfa2)*sin(th2)))/(l2*cos(alfa2)*(cos(Ax)*cos(Ay) + 1)*(O2(1)*sin(th2) + O2(3)*cos(alfa2)*cos(th2) - b*cos(alfa2)*sin(th2))) + (dAy*p*cos(phi2)*(b*cos(alfa2) - O2(1) + l1*cos(alfa2)*cos(th2))*(2*cos(Az + alfa2)*cos(Ay)*cos(th2) + cos(Ay)^2*sin(Ax)^2*cos(th2) - sin(Ax)^2*sin(Ay)^2*cos(th2) + 2*sin(Az + alfa2)*sin(Ax)*sin(Ay)*cos(th2) - cos(Ax)*sin(Ax)*sin(Ay)*cos(th2) - 2*cos(Ay)*sin(Ax)*sin(Ay)*cos(th2) + 6*cos(Az + alfa2)*cos(Ax)*cos(Ay)^2*cos(th2) + 6*cos(Az + alfa2)*cos(Ax)^2*cos(Ay)^3*cos(th2) + 2*cos(Az + alfa2)*cos(Ax)^3*cos(Ay)^4*cos(th2) + cos(Ax)*cos(Ay)^3*sin(Ax)^2*cos(th2) + cos(Ax)^2*cos(Ay)*sin(Ax)*sin(Ay)*cos(th2) + cos(Ax)*cos(Ay)*sin(Ax)^2*sin(Ay)^2*cos(th2) + 2*cos(Az + alfa2)*cos(Ax)*sin(Ay)*cos(alfa2)*sin(th2) + 6*cos(Az + alfa2)*cos(Ax)^3*cos(Ay)^2*sin(Ay)*cos(alfa2)*sin(th2) + 2*cos(Az + alfa2)*cos(Ax)^4*cos(Ay)^3*sin(Ay)*cos(alfa2)*sin(th2) - 4*sin(Az + alfa2)*cos(Ax)^2*cos(Ay)^2*sin(Ax)*cos(alfa2)*sin(th2) - 2*sin(Az + alfa2)*cos(Ax)^3*cos(Ay)^3*sin(Ax)*cos(alfa2)*sin(th2) - 2*sin(Az + alfa2)*cos(Ax)^2*sin(Ax)*sin(Ay)^2*cos(alfa2)*sin(th2) + 2*sin(Az + alfa2)*cos(Ax)*cos(Ay)*sin(Ax)*sin(Ay)*cos(th2) - 2*sin(Az + alfa2)*cos(Ax)*cos(Ay)*sin(Ax)*cos(alfa2)*sin(th2) + 6*cos(Az + alfa2)*cos(Ax)^2*cos(Ay)*sin(Ay)*cos(alfa2)*sin(th2) - 2*cos(Az + alfa2)*cos(Ax)*sin(Ax)^2*sin(Ay)*cos(alfa2)*sin(th2) - 2*cos(Az + alfa2)*cos(Ax)^2*cos(Ay)*sin(Ax)^2*sin(Ay)*cos(alfa2)*sin(th2) - 2*sin(Az + alfa2)*cos(Ax)^3*cos(Ay)*sin(Ax)*sin(Ay)^2*cos(alfa2)*sin(th2)))/(2*l2*cos(alfa2)*(cos(Ax)*cos(Ay) + 1)^3*(O2(1)*sin(th2) + O2(3)*cos(alfa2)*cos(th2) - b*cos(alfa2)*sin(th2))) + (dAx*p*cos(phi2)*(b*cos(alfa2) - O2(1) + l1*cos(alfa2)*cos(th2))*(cos(Ax)^2*cos(Ay)^3*cos(th2) + cos(Ax)^3*cos(Ay)^2*cos(th2) + 2*cos(Ay)^3*sin(Ax)^2*cos(th2) + cos(Ax)*cos(Ay)^2*cos(th2) + cos(Ax)^2*cos(Ay)*cos(th2) - cos(Ay)*sin(Ax)^2*cos(th2) + 2*cos(Ay)^2*sin(Ax)^3*sin(Ay)*cos(th2) - 4*sin(Az + alfa2)*cos(Ax)^2*cos(Ay)^2*cos(th2) - 2*sin(Az + alfa2)*cos(Ax)^3*cos(Ay)^3*cos(th2) - 2*sin(Az + alfa2)*cos(Ay)^2*sin(Ax)^2*cos(th2) + cos(Ax)*cos(Ay)^2*sin(Ax)^2*cos(th2) - 2*sin(Az + alfa2)*cos(Ax)*cos(Ay)*cos(th2) - 2*cos(Az + alfa2)*cos(Ay)*sin(Ax)^3*cos(alfa2)*sin(th2) - 2*sin(Az + alfa2)*cos(Ax)^2*sin(Ay)*cos(alfa2)*sin(th2) + 2*sin(Az + alfa2)*sin(Ax)^2*sin(Ay)*cos(alfa2)*sin(th2) - 2*sin(Az + alfa2)*cos(Ax)*cos(Ay)^3*sin(Ax)^2*cos(th2) + 2*cos(Ax)^2*cos(Ay)^2*sin(Ax)*sin(Ay)*cos(th2) - 4*cos(Az + alfa2)*cos(Ax)*sin(Ax)*cos(alfa2)*sin(th2) + 2*cos(Az + alfa2)*cos(Ay)*sin(Ax)*cos(alfa2)*sin(th2) + 2*cos(Ax)*cos(Ay)*sin(Ax)*sin(Ay)*cos(th2) - 2*cos(Az + alfa2)*cos(Ax)*cos(Ay)^2*sin(Ax)^3*cos(alfa2)*sin(th2) + 6*cos(Az + alfa2)*cos(Ax)^2*cos(Ay)^3*sin(Ax)*cos(alfa2)*sin(th2) - 4*cos(Az + alfa2)*cos(Ax)^3*cos(Ay)^2*sin(Ax)*cos(alfa2)*sin(th2) + 2*cos(Az + alfa2)*cos(Ax)^3*cos(Ay)^4*sin(Ax)*cos(alfa2)*sin(th2) - 2*sin(Az + alfa2)*cos(Ax)^4*cos(Ay)^2*sin(Ay)*cos(alfa2)*sin(th2) + 6*cos(Az + alfa2)*cos(Ax)*cos(Ay)^2*sin(Ax)*cos(alfa2)*sin(th2) - 8*cos(Az + alfa2)*cos(Ax)^2*cos(Ay)*sin(Ax)*cos(alfa2)*sin(th2) - 4*sin(Az + alfa2)*cos(Ax)^3*cos(Ay)*sin(Ay)*cos(alfa2)*sin(th2) + 2*sin(Az + alfa2)*cos(Ax)*cos(Ay)*sin(Ax)^2*sin(Ay)*cos(alfa2)*sin(th2)))/(2*l2*cos(alfa2)*(cos(Ax)*cos(Ay) + 1)^3*(O2(1)*sin(th2) + O2(3)*cos(alfa2)*cos(th2) - b*cos(alfa2)*sin(th2))) + (dO2(3)*p*cos(phi2)*cos(th2)*(b*cos(alfa2) - O2(1) + l1*cos(alfa2)*cos(th2))*(2*sin(Az + alfa2)*cos(Ay)*sin(Ax)*cos(th2) - cos(Ay)^2*sin(Ax)*cos(th2) - 2*cos(Az + alfa2)*sin(Ay)*cos(th2) - cos(Ax)*cos(Ay)*sin(Ax)*cos(th2) + 2*cos(Az + alfa2)*sin(Ax)^2*cos(alfa2)*sin(th2) - cos(Ay)*sin(Ax)^2*sin(Ay)*cos(th2) + 2*sin(Az + alfa2)*cos(Ax)*cos(Ay)^2*sin(Ax)*cos(th2) - 2*cos(Az + alfa2)*cos(Ax)^2*cos(Ay)^2*sin(Ay)*cos(th2) + 4*cos(Az + alfa2)*cos(Ax)^2*cos(Ay)^2*cos(alfa2)*sin(th2) + 2*cos(Az + alfa2)*cos(Ax)^3*cos(Ay)^3*cos(alfa2)*sin(th2) - 4*cos(Az + alfa2)*cos(Ax)*cos(Ay)*sin(Ay)*cos(th2) + 2*cos(Az + alfa2)*cos(Ax)*cos(Ay)*cos(alfa2)*sin(th2) + 2*sin(Az + alfa2)*cos(Ax)*sin(Ax)*sin(Ay)*cos(alfa2)*sin(th2) + 2*cos(Az + alfa2)*cos(Ax)*cos(Ay)*sin(Ax)^2*cos(alfa2)*sin(th2) + 2*sin(Az + alfa2)*cos(Ax)^2*cos(Ay)*sin(Ax)*sin(Ay)*cos(alfa2)*sin(th2)))/(2*l2*(cos(Ax)*cos(Ay) + 1)^2*(O2(1)*sin(th2) + O2(3)*cos(alfa2)*cos(th2) - b*cos(alfa2)*sin(th2))^2)
       -(O3(1)*O3(3)*dth3*cos(alfa3)*cos(phi3)*cos(th3)^2 - b^2*dphi3*cos(alfa3)^2*sin(phi3)*sin(th3)^2 - O3(1)^2*dphi3*sin(phi3)*sin(th3)^2 + O3(1)*O3(3)*dth3*cos(alfa3)*cos(phi3)*sin(th3)^2 + dO3(3)*l1*cos(alfa3)^2*cos(phi3)*cos(th3)^2*sin(th3) + O3(1)*dth3*l1*cos(alfa3)*cos(phi3)*sin(th3)^3 + 2*O3(1)*b*dphi3*cos(alfa3)*sin(phi3)*sin(th3)^2 - O3(1)*dO3(3)*cos(alfa3)*cos(phi3)*cos(th3)*sin(th3) + O3(3)*dO3(1)*cos(alfa3)*cos(phi3)*cos(th3)*sin(th3) - O3(3)*b*dth3*cos(alfa3)^2*cos(phi3)*cos(th3)^2 - O3(3)*dth3*l1*cos(alfa3)^2*cos(phi3)*cos(th3)^3 - O3(3)*b*dth3*cos(alfa3)^2*cos(phi3)*sin(th3)^2 - b*dth3*l1*cos(alfa3)^2*cos(phi3)*sin(th3)^3 + b*dO3(3)*cos(alfa3)^2*cos(phi3)*cos(th3)*sin(th3) + dO3(1)*l1*cos(alfa3)*cos(phi3)*cos(th3)*sin(th3)^2 + O3(3)*b*dphi3*cos(alfa3)^2*cos(th3)*sin(phi3)*sin(th3) + O3(1)*dphi3*l1*cos(alfa3)*cos(th3)*sin(phi3)*sin(th3)^2 + O3(3)*dphi3*l1*cos(alfa3)^2*cos(th3)^2*sin(phi3)*sin(th3) - b*dphi3*l1*cos(alfa3)^2*cos(th3)*sin(phi3)*sin(th3)^2 - O3(1)*O3(3)*dphi3*cos(alfa3)*cos(th3)*sin(phi3)*sin(th3))/(l2*(O3(1)*sin(th3) + O3(3)*cos(alfa3)*cos(th3) - b*cos(alfa3)*sin(th3))^2), dth3*((p*cos(phi3)*(b*cos(alfa3) - O3(1) + l1*cos(alfa3)*cos(th3))*(2*sin(Az + alfa3)*cos(Ax)*cos(alfa3)*cos(th3) - cos(Ay)^2*sin(Ax)*sin(Ay)^2*sin(th3) + 2*sin(Az + alfa3)*cos(Ay)*sin(Ay)*sin(th3) - cos(Ax)*cos(Ay)*sin(Ay)*sin(th3) + 4*sin(Az + alfa3)*cos(Ax)^2*cos(Ay)*cos(alfa3)*cos(th3) + 2*sin(Az + alfa3)*cos(Ax)*cos(Ay)^2*sin(Ay)*sin(th3) - 2*sin(Az + alfa3)*cos(Ax)*sin(Ay)^2*cos(alfa3)*cos(th3) + 2*sin(Az + alfa3)*cos(Ax)^3*cos(Ay)^2*cos(alfa3)*cos(th3) - 2*sin(Az + alfa3)*cos(Ax)^2*cos(Ay)*sin(Ay)^2*cos(alfa3)*cos(th3) + 2*cos(Az + alfa3)*cos(Ax)*cos(Ay)*sin(Ax)*sin(Ay)*cos(alfa3)*cos(th3) + 2*cos(Az + alfa3)*cos(Ax)^2*cos(Ay)^2*sin(Ax)*sin(Ay)*cos(alfa3)*cos(th3)))/(2*l2*cos(alfa3)*(cos(Ax)*cos(Ay) + 1)^2*(O3(1)*sin(th3) + O3(3)*cos(alfa3)*cos(th3) - b*cos(alfa3)*sin(th3))) - (l1*p*cos(phi3)*sin(th3)*(cos(Ay)^2*sin(Ax)*sin(Ay)^2*cos(th3) - 2*sin(Az + alfa3)*cos(Ay)*sin(Ay)*cos(th3) + 2*sin(Az + alfa3)*cos(Ax)*cos(alfa3)*sin(th3) + cos(Ax)*cos(Ay)*sin(Ay)*cos(th3) - 2*sin(Az + alfa3)*cos(Ax)*cos(Ay)^2*sin(Ay)*cos(th3) + 4*sin(Az + alfa3)*cos(Ax)^2*cos(Ay)*cos(alfa3)*sin(th3) - 2*sin(Az + alfa3)*cos(Ax)*sin(Ay)^2*cos(alfa3)*sin(th3) + 2*sin(Az + alfa3)*cos(Ax)^3*cos(Ay)^2*cos(alfa3)*sin(th3) - 2*sin(Az + alfa3)*cos(Ax)^2*cos(Ay)*sin(Ay)^2*cos(alfa3)*sin(th3) + 2*cos(Az + alfa3)*cos(Ax)*cos(Ay)*sin(Ax)*sin(Ay)*cos(alfa3)*sin(th3) + 2*cos(Az + alfa3)*cos(Ax)^2*cos(Ay)^2*sin(Ax)*sin(Ay)*cos(alfa3)*sin(th3)))/(2*l2*(cos(Ax)*cos(Ay) + 1)^2*(O3(1)*sin(th3) + O3(3)*cos(alfa3)*cos(th3) - b*cos(alfa3)*sin(th3))) + (p*cos(phi3)*(O3(3)*cos(alfa3)*sin(th3) - O3(1)*cos(th3) + b*cos(alfa3)*cos(th3))*(b*cos(alfa3) - O3(1) + l1*cos(alfa3)*cos(th3))*(cos(Ay)^2*sin(Ax)*sin(Ay)^2*cos(th3) - 2*sin(Az + alfa3)*cos(Ay)*sin(Ay)*cos(th3) + 2*sin(Az + alfa3)*cos(Ax)*cos(alfa3)*sin(th3) + cos(Ax)*cos(Ay)*sin(Ay)*cos(th3) - 2*sin(Az + alfa3)*cos(Ax)*cos(Ay)^2*sin(Ay)*cos(th3) + 4*sin(Az + alfa3)*cos(Ax)^2*cos(Ay)*cos(alfa3)*sin(th3) - 2*sin(Az + alfa3)*cos(Ax)*sin(Ay)^2*cos(alfa3)*sin(th3) + 2*sin(Az + alfa3)*cos(Ax)^3*cos(Ay)^2*cos(alfa3)*sin(th3) - 2*sin(Az + alfa3)*cos(Ax)^2*cos(Ay)*sin(Ay)^2*cos(alfa3)*sin(th3) + 2*cos(Az + alfa3)*cos(Ax)*cos(Ay)*sin(Ax)*sin(Ay)*cos(alfa3)*sin(th3) + 2*cos(Az + alfa3)*cos(Ax)^2*cos(Ay)^2*sin(Ax)*sin(Ay)*cos(alfa3)*sin(th3)))/(2*l2*cos(alfa3)*(cos(Ax)*cos(Ay) + 1)^2*(O3(1)*sin(th3) + O3(3)*cos(alfa3)*cos(th3) - b*cos(alfa3)*sin(th3))^2)) - (dO3(3)*p*cos(phi3)*cos(th3)*(b*cos(alfa3) - O3(1) + l1*cos(alfa3)*cos(th3))*(cos(Ay)^2*sin(Ax)*sin(Ay)^2*cos(th3) - 2*sin(Az + alfa3)*cos(Ay)*sin(Ay)*cos(th3) + 2*sin(Az + alfa3)*cos(Ax)*cos(alfa3)*sin(th3) + cos(Ax)*cos(Ay)*sin(Ay)*cos(th3) - 2*sin(Az + alfa3)*cos(Ax)*cos(Ay)^2*sin(Ay)*cos(th3) + 4*sin(Az + alfa3)*cos(Ax)^2*cos(Ay)*cos(alfa3)*sin(th3) - 2*sin(Az + alfa3)*cos(Ax)*sin(Ay)^2*cos(alfa3)*sin(th3) + 2*sin(Az + alfa3)*cos(Ax)^3*cos(Ay)^2*cos(alfa3)*sin(th3) - 2*sin(Az + alfa3)*cos(Ax)^2*cos(Ay)*sin(Ay)^2*cos(alfa3)*sin(th3) + 2*cos(Az + alfa3)*cos(Ax)*cos(Ay)*sin(Ax)*sin(Ay)*cos(alfa3)*sin(th3) + 2*cos(Az + alfa3)*cos(Ax)^2*cos(Ay)^2*sin(Ax)*sin(Ay)*cos(alfa3)*sin(th3)))/(2*l2*(cos(Ax)*cos(Ay) + 1)^2*(O3(1)*sin(th3) + O3(3)*cos(alfa3)*cos(th3) - b*cos(alfa3)*sin(th3))^2) - (dAz*p*cos(phi3)*(b*cos(alfa3) - O3(1) + l1*cos(alfa3)*cos(th3))*(cos(Az + alfa3)*cos(Ay)*sin(Ay)*cos(th3) - cos(Az + alfa3)*cos(Ax)*cos(alfa3)*sin(th3) - cos(Az + alfa3)*cos(Ax)^2*cos(Ay)*cos(alfa3)*sin(th3) + cos(Az + alfa3)*cos(Ax)*sin(Ay)^2*cos(alfa3)*sin(th3) + sin(Az + alfa3)*cos(Ax)*cos(Ay)*sin(Ax)*sin(Ay)*cos(alfa3)*sin(th3)))/(l2*cos(alfa3)*(cos(Ax)*cos(Ay) + 1)*(O3(1)*sin(th3) + O3(3)*cos(alfa3)*cos(th3) - b*cos(alfa3)*sin(th3))) - (dphi3*p*sin(phi3)*(b*cos(alfa3) - O3(1) + l1*cos(alfa3)*cos(th3))*(cos(Ay)^2*sin(Ax)*sin(Ay)^2*cos(th3) - 2*sin(Az + alfa3)*cos(Ay)*sin(Ay)*cos(th3) + 2*sin(Az + alfa3)*cos(Ax)*cos(alfa3)*sin(th3) + cos(Ax)*cos(Ay)*sin(Ay)*cos(th3) - 2*sin(Az + alfa3)*cos(Ax)*cos(Ay)^2*sin(Ay)*cos(th3) + 4*sin(Az + alfa3)*cos(Ax)^2*cos(Ay)*cos(alfa3)*sin(th3) - 2*sin(Az + alfa3)*cos(Ax)*sin(Ay)^2*cos(alfa3)*sin(th3) + 2*sin(Az + alfa3)*cos(Ax)^3*cos(Ay)^2*cos(alfa3)*sin(th3) - 2*sin(Az + alfa3)*cos(Ax)^2*cos(Ay)*sin(Ay)^2*cos(alfa3)*sin(th3) + 2*cos(Az + alfa3)*cos(Ax)*cos(Ay)*sin(Ax)*sin(Ay)*cos(alfa3)*sin(th3) + 2*cos(Az + alfa3)*cos(Ax)^2*cos(Ay)^2*sin(Ax)*sin(Ay)*cos(alfa3)*sin(th3)))/(2*l2*cos(alfa3)*(cos(Ax)*cos(Ay) + 1)^2*(O3(1)*sin(th3) + O3(3)*cos(alfa3)*cos(th3) - b*cos(alfa3)*sin(th3))) - (dO3(1)*p*cos(phi3)*cos(th3)*(O3(3) + l1*sin(th3))*(cos(Ay)^2*sin(Ax)*sin(Ay)^2*cos(th3) - 2*sin(Az + alfa3)*cos(Ay)*sin(Ay)*cos(th3) + 2*sin(Az + alfa3)*cos(Ax)*cos(alfa3)*sin(th3) + cos(Ax)*cos(Ay)*sin(Ay)*cos(th3) - 2*sin(Az + alfa3)*cos(Ax)*cos(Ay)^2*sin(Ay)*cos(th3) + 4*sin(Az + alfa3)*cos(Ax)^2*cos(Ay)*cos(alfa3)*sin(th3) - 2*sin(Az + alfa3)*cos(Ax)*sin(Ay)^2*cos(alfa3)*sin(th3) + 2*sin(Az + alfa3)*cos(Ax)^3*cos(Ay)^2*cos(alfa3)*sin(th3) - 2*sin(Az + alfa3)*cos(Ax)^2*cos(Ay)*sin(Ay)^2*cos(alfa3)*sin(th3) + 2*cos(Az + alfa3)*cos(Ax)*cos(Ay)*sin(Ax)*sin(Ay)*cos(alfa3)*sin(th3) + 2*cos(Az + alfa3)*cos(Ax)^2*cos(Ay)^2*sin(Ax)*sin(Ay)*cos(alfa3)*sin(th3)))/(2*l2*(cos(Ax)*cos(Ay) + 1)^2*(O3(1)*sin(th3) + O3(3)*cos(alfa3)*cos(th3) - b*cos(alfa3)*sin(th3))^2) - (dAy*p*cos(phi3)*(b*cos(alfa3) - O3(1) + l1*cos(alfa3)*cos(th3))*(2*sin(Az + alfa3)*cos(Ay)^2*cos(th3) - cos(Ax)^2*cos(Ay)^3*cos(th3) - 2*sin(Az + alfa3)*sin(Ay)^2*cos(th3) - cos(Ax)*cos(Ay)^2*cos(th3) + cos(Ax)*sin(Ay)^2*cos(th3) + 4*sin(Az + alfa3)*cos(Ax)*cos(Ay)^3*cos(th3) + 2*cos(Ay)*sin(Ax)*sin(Ay)^3*cos(th3) - 2*cos(Ay)^3*sin(Ax)*sin(Ay)*cos(th3) + 2*sin(Az + alfa3)*cos(Ax)^2*cos(Ay)^4*cos(th3) - cos(Ax)^2*cos(Ay)*sin(Ay)^2*cos(th3) - 2*sin(Az + alfa3)*cos(Ax)*cos(Ay)*sin(Ay)^2*cos(th3) - 2*cos(Ax)*cos(Ay)^4*sin(Ax)*sin(Ay)*cos(th3) + 2*sin(Az + alfa3)*cos(Ax)^2*sin(Ay)^3*cos(alfa3)*sin(th3) - 4*cos(Az + alfa3)*cos(Ax)^2*cos(Ay)^3*sin(Ax)*cos(alfa3)*sin(th3) - 2*cos(Az + alfa3)*cos(Ax)^3*cos(Ay)^4*sin(Ax)*cos(alfa3)*sin(th3) + 8*sin(Az + alfa3)*cos(Ax)^2*cos(Ay)^2*sin(Ay)*cos(alfa3)*sin(th3) + 2*sin(Az + alfa3)*cos(Ax)^3*cos(Ay)*sin(Ay)^3*cos(alfa3)*sin(th3) + 4*sin(Az + alfa3)*cos(Ax)^3*cos(Ay)^3*sin(Ay)*cos(alfa3)*sin(th3) + 4*sin(Az + alfa3)*cos(Ax)*cos(Ay)*sin(Ay)*cos(alfa3)*sin(th3) - 2*cos(Az + alfa3)*cos(Ax)*cos(Ay)^2*sin(Ax)*cos(alfa3)*sin(th3) + 2*cos(Az + alfa3)*cos(Ax)*sin(Ax)*sin(Ay)^2*cos(alfa3)*sin(th3) + 2*cos(Az + alfa3)*cos(Ax)^2*cos(Ay)*sin(Ax)*sin(Ay)^2*cos(alfa3)*sin(th3)))/(2*l2*cos(alfa3)*(cos(Ax)*cos(Ay) + 1)^3*(O3(1)*sin(th3) + O3(3)*cos(alfa3)*cos(th3) - b*cos(alfa3)*sin(th3))) - (dAx*p*cos(phi3)*(b*cos(alfa3) - O3(1) + l1*cos(alfa3)*cos(th3))*(2*sin(Az + alfa3)*sin(Ax)*cos(alfa3)*sin(th3) + cos(Ay)*sin(Ax)*sin(Ay)*cos(th3) - cos(Ax)^2*cos(Ay)^3*sin(Ay)^2*cos(th3) - 2*cos(Ay)^3*sin(Ax)^2*sin(Ay)^2*cos(th3) - cos(Ax)*cos(Ay)^2*sin(Ay)^2*cos(th3) + 2*sin(Az + alfa3)*cos(Ay)^2*sin(Ax)*sin(Ay)*cos(th3) - cos(Ax)*cos(Ay)^2*sin(Ax)*sin(Ay)*cos(th3) - 2*sin(Az + alfa3)*sin(Ax)*sin(Ay)^2*cos(alfa3)*sin(th3) - 4*cos(Az + alfa3)*cos(Ax)^3*cos(Ay)^2*sin(Ay)*cos(alfa3)*sin(th3) - 2*cos(Az + alfa3)*cos(Ax)^4*cos(Ay)^3*sin(Ay)*cos(alfa3)*sin(th3) + 6*sin(Az + alfa3)*cos(Ax)^2*cos(Ay)^2*sin(Ax)*cos(alfa3)*sin(th3) + 2*sin(Az + alfa3)*cos(Ax)^3*cos(Ay)^3*sin(Ax)*cos(alfa3)*sin(th3) + 6*sin(Az + alfa3)*cos(Ax)*cos(Ay)*sin(Ax)*cos(alfa3)*sin(th3) + 2*sin(Az + alfa3)*cos(Ax)*cos(Ay)^3*sin(Ax)*sin(Ay)*cos(th3) - 2*cos(Az + alfa3)*cos(Ax)^2*cos(Ay)*sin(Ay)*cos(alfa3)*sin(th3) + 2*cos(Az + alfa3)*cos(Ay)*sin(Ax)^2*sin(Ay)*cos(alfa3)*sin(th3) - 2*sin(Az + alfa3)*cos(Ax)*cos(Ay)*sin(Ax)*sin(Ay)^2*cos(alfa3)*sin(th3) + 2*cos(Az + alfa3)*cos(Ax)*cos(Ay)^2*sin(Ax)^2*sin(Ay)*cos(alfa3)*sin(th3)))/(2*l2*cos(alfa3)*(cos(Ax)*cos(Ay) + 1)^3*(O3(1)*sin(th3) + O3(3)*cos(alfa3)*cos(th3) - b*cos(alfa3)*sin(th3))), (dphi3*p*sin(phi3)*(b*cos(alfa3) - O3(1) + l1*cos(alfa3)*cos(th3))*(2*sin(Az + alfa3)*cos(Ay)*sin(Ax)*cos(th3) - cos(Ay)^2*sin(Ax)*cos(th3) - 2*cos(Az + alfa3)*sin(Ay)*cos(th3) - cos(Ax)*cos(Ay)*sin(Ax)*cos(th3) + 2*cos(Az + alfa3)*sin(Ax)^2*cos(alfa3)*sin(th3) - cos(Ay)*sin(Ax)^2*sin(Ay)*cos(th3) + 2*sin(Az + alfa3)*cos(Ax)*cos(Ay)^2*sin(Ax)*cos(th3) - 2*cos(Az + alfa3)*cos(Ax)^2*cos(Ay)^2*sin(Ay)*cos(th3) + 4*cos(Az + alfa3)*cos(Ax)^2*cos(Ay)^2*cos(alfa3)*sin(th3) + 2*cos(Az + alfa3)*cos(Ax)^3*cos(Ay)^3*cos(alfa3)*sin(th3) - 4*cos(Az + alfa3)*cos(Ax)*cos(Ay)*sin(Ay)*cos(th3) + 2*cos(Az + alfa3)*cos(Ax)*cos(Ay)*cos(alfa3)*sin(th3) + 2*sin(Az + alfa3)*cos(Ax)*sin(Ax)*sin(Ay)*cos(alfa3)*sin(th3) + 2*cos(Az + alfa3)*cos(Ax)*cos(Ay)*sin(Ax)^2*cos(alfa3)*sin(th3) + 2*sin(Az + alfa3)*cos(Ax)^2*cos(Ay)*sin(Ax)*sin(Ay)*cos(alfa3)*sin(th3)))/(2*l2*cos(alfa3)*(cos(Ax)*cos(Ay) + 1)^2*(O3(1)*sin(th3) + O3(3)*cos(alfa3)*cos(th3) - b*cos(alfa3)*sin(th3))) - dth3*((p*cos(phi3)*(b*cos(alfa3) - O3(1) + l1*cos(alfa3)*cos(th3))*(cos(Ay)^2*sin(Ax)*sin(th3) + 2*cos(Az + alfa3)*sin(Ay)*sin(th3) - 2*sin(Az + alfa3)*cos(Ay)*sin(Ax)*sin(th3) + cos(Ax)*cos(Ay)*sin(Ax)*sin(th3) + 2*cos(Az + alfa3)*sin(Ax)^2*cos(alfa3)*cos(th3) + cos(Ay)*sin(Ax)^2*sin(Ay)*sin(th3) - 2*sin(Az + alfa3)*cos(Ax)*cos(Ay)^2*sin(Ax)*sin(th3) + 4*cos(Az + alfa3)*cos(Ax)^2*cos(Ay)^2*cos(alfa3)*cos(th3) + 2*cos(Az + alfa3)*cos(Ax)^3*cos(Ay)^3*cos(alfa3)*cos(th3) + 2*cos(Az + alfa3)*cos(Ax)^2*cos(Ay)^2*sin(Ay)*sin(th3) + 2*cos(Az + alfa3)*cos(Ax)*cos(Ay)*cos(alfa3)*cos(th3) + 4*cos(Az + alfa3)*cos(Ax)*cos(Ay)*sin(Ay)*sin(th3) + 2*sin(Az + alfa3)*cos(Ax)*sin(Ax)*sin(Ay)*cos(alfa3)*cos(th3) + 2*cos(Az + alfa3)*cos(Ax)*cos(Ay)*sin(Ax)^2*cos(alfa3)*cos(th3) + 2*sin(Az + alfa3)*cos(Ax)^2*cos(Ay)*sin(Ax)*sin(Ay)*cos(alfa3)*cos(th3)))/(2*l2*cos(alfa3)*(cos(Ax)*cos(Ay) + 1)^2*(O3(1)*sin(th3) + O3(3)*cos(alfa3)*cos(th3) - b*cos(alfa3)*sin(th3))) - (l1*p*cos(phi3)*sin(th3)*(2*sin(Az + alfa3)*cos(Ay)*sin(Ax)*cos(th3) - cos(Ay)^2*sin(Ax)*cos(th3) - 2*cos(Az + alfa3)*sin(Ay)*cos(th3) - cos(Ax)*cos(Ay)*sin(Ax)*cos(th3) + 2*cos(Az + alfa3)*sin(Ax)^2*cos(alfa3)*sin(th3) - cos(Ay)*sin(Ax)^2*sin(Ay)*cos(th3) + 2*sin(Az + alfa3)*cos(Ax)*cos(Ay)^2*sin(Ax)*cos(th3) - 2*cos(Az + alfa3)*cos(Ax)^2*cos(Ay)^2*sin(Ay)*cos(th3) + 4*cos(Az + alfa3)*cos(Ax)^2*cos(Ay)^2*cos(alfa3)*sin(th3) + 2*cos(Az + alfa3)*cos(Ax)^3*cos(Ay)^3*cos(alfa3)*sin(th3) - 4*cos(Az + alfa3)*cos(Ax)*cos(Ay)*sin(Ay)*cos(th3) + 2*cos(Az + alfa3)*cos(Ax)*cos(Ay)*cos(alfa3)*sin(th3) + 2*sin(Az + alfa3)*cos(Ax)*sin(Ax)*sin(Ay)*cos(alfa3)*sin(th3) + 2*cos(Az + alfa3)*cos(Ax)*cos(Ay)*sin(Ax)^2*cos(alfa3)*sin(th3) + 2*sin(Az + alfa3)*cos(Ax)^2*cos(Ay)*sin(Ax)*sin(Ay)*cos(alfa3)*sin(th3)))/(2*l2*(cos(Ax)*cos(Ay) + 1)^2*(O3(1)*sin(th3) + O3(3)*cos(alfa3)*cos(th3) - b*cos(alfa3)*sin(th3))) + (p*cos(phi3)*(O3(3)*cos(alfa3)*sin(th3) - O3(1)*cos(th3) + b*cos(alfa3)*cos(th3))*(b*cos(alfa3) - O3(1) + l1*cos(alfa3)*cos(th3))*(2*sin(Az + alfa3)*cos(Ay)*sin(Ax)*cos(th3) - cos(Ay)^2*sin(Ax)*cos(th3) - 2*cos(Az + alfa3)*sin(Ay)*cos(th3) - cos(Ax)*cos(Ay)*sin(Ax)*cos(th3) + 2*cos(Az + alfa3)*sin(Ax)^2*cos(alfa3)*sin(th3) - cos(Ay)*sin(Ax)^2*sin(Ay)*cos(th3) + 2*sin(Az + alfa3)*cos(Ax)*cos(Ay)^2*sin(Ax)*cos(th3) - 2*cos(Az + alfa3)*cos(Ax)^2*cos(Ay)^2*sin(Ay)*cos(th3) + 4*cos(Az + alfa3)*cos(Ax)^2*cos(Ay)^2*cos(alfa3)*sin(th3) + 2*cos(Az + alfa3)*cos(Ax)^3*cos(Ay)^3*cos(alfa3)*sin(th3) - 4*cos(Az + alfa3)*cos(Ax)*cos(Ay)*sin(Ay)*cos(th3) + 2*cos(Az + alfa3)*cos(Ax)*cos(Ay)*cos(alfa3)*sin(th3) + 2*sin(Az + alfa3)*cos(Ax)*sin(Ax)*sin(Ay)*cos(alfa3)*sin(th3) + 2*cos(Az + alfa3)*cos(Ax)*cos(Ay)*sin(Ax)^2*cos(alfa3)*sin(th3) + 2*sin(Az + alfa3)*cos(Ax)^2*cos(Ay)*sin(Ax)*sin(Ay)*cos(alfa3)*sin(th3)))/(2*l2*cos(alfa3)*(cos(Ax)*cos(Ay) + 1)^2*(O3(1)*sin(th3) + O3(3)*cos(alfa3)*cos(th3) - b*cos(alfa3)*sin(th3))^2)) + (dO3(1)*p*cos(phi3)*cos(th3)*(O3(3) + l1*sin(th3))*(2*sin(Az + alfa3)*cos(Ay)*sin(Ax)*cos(th3) - cos(Ay)^2*sin(Ax)*cos(th3) - 2*cos(Az + alfa3)*sin(Ay)*cos(th3) - cos(Ax)*cos(Ay)*sin(Ax)*cos(th3) + 2*cos(Az + alfa3)*sin(Ax)^2*cos(alfa3)*sin(th3) - cos(Ay)*sin(Ax)^2*sin(Ay)*cos(th3) + 2*sin(Az + alfa3)*cos(Ax)*cos(Ay)^2*sin(Ax)*cos(th3) - 2*cos(Az + alfa3)*cos(Ax)^2*cos(Ay)^2*sin(Ay)*cos(th3) + 4*cos(Az + alfa3)*cos(Ax)^2*cos(Ay)^2*cos(alfa3)*sin(th3) + 2*cos(Az + alfa3)*cos(Ax)^3*cos(Ay)^3*cos(alfa3)*sin(th3) - 4*cos(Az + alfa3)*cos(Ax)*cos(Ay)*sin(Ay)*cos(th3) + 2*cos(Az + alfa3)*cos(Ax)*cos(Ay)*cos(alfa3)*sin(th3) + 2*sin(Az + alfa3)*cos(Ax)*sin(Ax)*sin(Ay)*cos(alfa3)*sin(th3) + 2*cos(Az + alfa3)*cos(Ax)*cos(Ay)*sin(Ax)^2*cos(alfa3)*sin(th3) + 2*sin(Az + alfa3)*cos(Ax)^2*cos(Ay)*sin(Ax)*sin(Ay)*cos(alfa3)*sin(th3)))/(2*l2*(cos(Ax)*cos(Ay) + 1)^2*(O3(1)*sin(th3) + O3(3)*cos(alfa3)*cos(th3) - b*cos(alfa3)*sin(th3))^2) - (dAz*p*cos(phi3)*(b*cos(alfa3) - O3(1) + l1*cos(alfa3)*cos(th3))*(sin(Az + alfa3)*sin(Ay)*cos(th3) - sin(Az + alfa3)*sin(Ax)^2*cos(alfa3)*sin(th3) + cos(Az + alfa3)*cos(Ay)*sin(Ax)*cos(th3) - sin(Az + alfa3)*cos(Ax)^2*cos(Ay)^2*cos(alfa3)*sin(th3) + sin(Az + alfa3)*cos(Ax)*cos(Ay)*sin(Ay)*cos(th3) - sin(Az + alfa3)*cos(Ax)*cos(Ay)*cos(alfa3)*sin(th3) + cos(Az + alfa3)*cos(Ax)*sin(Ax)*sin(Ay)*cos(alfa3)*sin(th3)))/(l2*cos(alfa3)*(cos(Ax)*cos(Ay) + 1)*(O3(1)*sin(th3) + O3(3)*cos(alfa3)*cos(th3) - b*cos(alfa3)*sin(th3))) + (dAy*p*cos(phi3)*(b*cos(alfa3) - O3(1) + l1*cos(alfa3)*cos(th3))*(2*cos(Az + alfa3)*cos(Ay)*cos(th3) + cos(Ay)^2*sin(Ax)^2*cos(th3) - sin(Ax)^2*sin(Ay)^2*cos(th3) + 2*sin(Az + alfa3)*sin(Ax)*sin(Ay)*cos(th3) - cos(Ax)*sin(Ax)*sin(Ay)*cos(th3) - 2*cos(Ay)*sin(Ax)*sin(Ay)*cos(th3) + 6*cos(Az + alfa3)*cos(Ax)*cos(Ay)^2*cos(th3) + 6*cos(Az + alfa3)*cos(Ax)^2*cos(Ay)^3*cos(th3) + 2*cos(Az + alfa3)*cos(Ax)^3*cos(Ay)^4*cos(th3) + cos(Ax)*cos(Ay)^3*sin(Ax)^2*cos(th3) + cos(Ax)^2*cos(Ay)*sin(Ax)*sin(Ay)*cos(th3) + cos(Ax)*cos(Ay)*sin(Ax)^2*sin(Ay)^2*cos(th3) + 2*cos(Az + alfa3)*cos(Ax)*sin(Ay)*cos(alfa3)*sin(th3) + 6*cos(Az + alfa3)*cos(Ax)^3*cos(Ay)^2*sin(Ay)*cos(alfa3)*sin(th3) + 2*cos(Az + alfa3)*cos(Ax)^4*cos(Ay)^3*sin(Ay)*cos(alfa3)*sin(th3) - 4*sin(Az + alfa3)*cos(Ax)^2*cos(Ay)^2*sin(Ax)*cos(alfa3)*sin(th3) - 2*sin(Az + alfa3)*cos(Ax)^3*cos(Ay)^3*sin(Ax)*cos(alfa3)*sin(th3) - 2*sin(Az + alfa3)*cos(Ax)^2*sin(Ax)*sin(Ay)^2*cos(alfa3)*sin(th3) + 2*sin(Az + alfa3)*cos(Ax)*cos(Ay)*sin(Ax)*sin(Ay)*cos(th3) - 2*sin(Az + alfa3)*cos(Ax)*cos(Ay)*sin(Ax)*cos(alfa3)*sin(th3) + 6*cos(Az + alfa3)*cos(Ax)^2*cos(Ay)*sin(Ay)*cos(alfa3)*sin(th3) - 2*cos(Az + alfa3)*cos(Ax)*sin(Ax)^2*sin(Ay)*cos(alfa3)*sin(th3) - 2*cos(Az + alfa3)*cos(Ax)^2*cos(Ay)*sin(Ax)^2*sin(Ay)*cos(alfa3)*sin(th3) - 2*sin(Az + alfa3)*cos(Ax)^3*cos(Ay)*sin(Ax)*sin(Ay)^2*cos(alfa3)*sin(th3)))/(2*l2*cos(alfa3)*(cos(Ax)*cos(Ay) + 1)^3*(O3(1)*sin(th3) + O3(3)*cos(alfa3)*cos(th3) - b*cos(alfa3)*sin(th3))) + (dAx*p*cos(phi3)*(b*cos(alfa3) - O3(1) + l1*cos(alfa3)*cos(th3))*(cos(Ax)^2*cos(Ay)^3*cos(th3) + cos(Ax)^3*cos(Ay)^2*cos(th3) + 2*cos(Ay)^3*sin(Ax)^2*cos(th3) + cos(Ax)*cos(Ay)^2*cos(th3) + cos(Ax)^2*cos(Ay)*cos(th3) - cos(Ay)*sin(Ax)^2*cos(th3) + 2*cos(Ay)^2*sin(Ax)^3*sin(Ay)*cos(th3) - 4*sin(Az + alfa3)*cos(Ax)^2*cos(Ay)^2*cos(th3) - 2*sin(Az + alfa3)*cos(Ax)^3*cos(Ay)^3*cos(th3) - 2*sin(Az + alfa3)*cos(Ay)^2*sin(Ax)^2*cos(th3) + cos(Ax)*cos(Ay)^2*sin(Ax)^2*cos(th3) - 2*sin(Az + alfa3)*cos(Ax)*cos(Ay)*cos(th3) - 2*cos(Az + alfa3)*cos(Ay)*sin(Ax)^3*cos(alfa3)*sin(th3) - 2*sin(Az + alfa3)*cos(Ax)^2*sin(Ay)*cos(alfa3)*sin(th3) + 2*sin(Az + alfa3)*sin(Ax)^2*sin(Ay)*cos(alfa3)*sin(th3) - 2*sin(Az + alfa3)*cos(Ax)*cos(Ay)^3*sin(Ax)^2*cos(th3) + 2*cos(Ax)^2*cos(Ay)^2*sin(Ax)*sin(Ay)*cos(th3) - 4*cos(Az + alfa3)*cos(Ax)*sin(Ax)*cos(alfa3)*sin(th3) + 2*cos(Az + alfa3)*cos(Ay)*sin(Ax)*cos(alfa3)*sin(th3) + 2*cos(Ax)*cos(Ay)*sin(Ax)*sin(Ay)*cos(th3) - 2*cos(Az + alfa3)*cos(Ax)*cos(Ay)^2*sin(Ax)^3*cos(alfa3)*sin(th3) + 6*cos(Az + alfa3)*cos(Ax)^2*cos(Ay)^3*sin(Ax)*cos(alfa3)*sin(th3) - 4*cos(Az + alfa3)*cos(Ax)^3*cos(Ay)^2*sin(Ax)*cos(alfa3)*sin(th3) + 2*cos(Az + alfa3)*cos(Ax)^3*cos(Ay)^4*sin(Ax)*cos(alfa3)*sin(th3) - 2*sin(Az + alfa3)*cos(Ax)^4*cos(Ay)^2*sin(Ay)*cos(alfa3)*sin(th3) + 6*cos(Az + alfa3)*cos(Ax)*cos(Ay)^2*sin(Ax)*cos(alfa3)*sin(th3) - 8*cos(Az + alfa3)*cos(Ax)^2*cos(Ay)*sin(Ax)*cos(alfa3)*sin(th3) - 4*sin(Az + alfa3)*cos(Ax)^3*cos(Ay)*sin(Ay)*cos(alfa3)*sin(th3) + 2*sin(Az + alfa3)*cos(Ax)*cos(Ay)*sin(Ax)^2*sin(Ay)*cos(alfa3)*sin(th3)))/(2*l2*cos(alfa3)*(cos(Ax)*cos(Ay) + 1)^3*(O3(1)*sin(th3) + O3(3)*cos(alfa3)*cos(th3) - b*cos(alfa3)*sin(th3))) + (dO3(3)*p*cos(phi3)*cos(th3)*(b*cos(alfa3) - O3(1) + l1*cos(alfa3)*cos(th3))*(2*sin(Az + alfa3)*cos(Ay)*sin(Ax)*cos(th3) - cos(Ay)^2*sin(Ax)*cos(th3) - 2*cos(Az + alfa3)*sin(Ay)*cos(th3) - cos(Ax)*cos(Ay)*sin(Ax)*cos(th3) + 2*cos(Az + alfa3)*sin(Ax)^2*cos(alfa3)*sin(th3) - cos(Ay)*sin(Ax)^2*sin(Ay)*cos(th3) + 2*sin(Az + alfa3)*cos(Ax)*cos(Ay)^2*sin(Ax)*cos(th3) - 2*cos(Az + alfa3)*cos(Ax)^2*cos(Ay)^2*sin(Ay)*cos(th3) + 4*cos(Az + alfa3)*cos(Ax)^2*cos(Ay)^2*cos(alfa3)*sin(th3) + 2*cos(Az + alfa3)*cos(Ax)^3*cos(Ay)^3*cos(alfa3)*sin(th3) - 4*cos(Az + alfa3)*cos(Ax)*cos(Ay)*sin(Ay)*cos(th3) + 2*cos(Az + alfa3)*cos(Ax)*cos(Ay)*cos(alfa3)*sin(th3) + 2*sin(Az + alfa3)*cos(Ax)*sin(Ax)*sin(Ay)*cos(alfa3)*sin(th3) + 2*cos(Az + alfa3)*cos(Ax)*cos(Ay)*sin(Ax)^2*cos(alfa3)*sin(th3) + 2*sin(Az + alfa3)*cos(Ax)^2*cos(Ay)*sin(Ax)*sin(Ay)*cos(alfa3)*sin(th3)))/(2*l2*(cos(Ax)*cos(Ay) + 1)^2*(O3(1)*sin(th3) + O3(3)*cos(alfa3)*cos(th3) - b*cos(alfa3)*sin(th3))^2)];

Ddlth2 = dJXTH*dlX + Jxith*ddlX;
ddlth2 = [Ddlth2(1); Ddlth2(2); Ddlth2(3)];

Ddlph2 = dJXPH*dlX + Jxiph*ddlX;
ddlph2 = [Ddlph2(1); Ddlph2(2); Ddlph2(3)];
end

%% ---- Funcion local: cinematica inversa de posicion de una pierna ----
function [th,phi] = solveLeg(O, alfa, b, l1, l2)
    A = 2*l1*cos(alfa)*(b*cos(alfa) - O(1));
    B = 2*l1*O(3)*cos(alfa)^2;
    C = O(1)^2 - 2*b*O(1)*cos(alfa) + cos(alfa)^2*(b^2 + l1^2 - l2^2 + O(3)^2);

    f_sol1 = (B + sqrt(A^2 + B^2 - C^2)) \ (C - A);
    Ang1 = 2*atan(f_sol1);
    th = (-Ang1) - pi;

    Cphi1 = (O(1) - cos(alfa)*(b + l1*cos(th))) / (l2*cos(alfa));
    Sphi1 = (-O(3) + l1*sin(th)) / l2;
    phi = atan2(Cphi1, Sphi1) + pi/2;
end
